simulink model "solar_pv_protected_c07_circuit"  (R2026b)
(part 7 of 16)

      | 用語2　　　　　　　 ; ADC：Analog-to-Digital Converter（アナログ・デジタル変換器）。測定電圧をデジタル値へ変換する回路。電流や温度も、センサーで電圧へ変換した後に読み取る。
      | 用語3　　　　　　　 ; IC：Integrated Circuit（集積回路）。複数の電子素子と機能を小さな半導体チップに集積した部品。
      | 用語4　　　　　　　 ; CH：Channel（測定チャネル）。CH0〜CH7はADCの入力番号であり、同時測定を意味しない。
      | 用語5　　　　　　　 ; MOSFET：Metal-Oxide-Semiconductor Field-Effect Transistor（金属・酸化膜・半導体構造の電界効果トランジスタ）。ゲートとソースの電圧でドレインとソースの導通を制御する素子。N-MOSはNチャネル型を表す。
      | 用語6　　　　　　　 ; FB：Feedback（帰還）。出力などを検出して内部制御へ戻すための信号・端子。
  ReadLabel_R31_P5 : ConnectionLabel  Description=|  Label=P5
      | この回路での名前　　; P5
      | 種別　　　　　　　　; ConnectionLabel
      | この回路での役割　　; 5V電源モジュールU12の出力を、ゲートドライバ入力LEDの電流制限抵抗とRP2040電源用ダイオードD3へ分配する。
      | この場所の直接接続　; R31（P5からU8のLEDへ流す電流をR32とともに制限する／232 ohm 1% 0.125W）: 1
      | 直接接続の範囲　　　; このラベルから実際の線・分岐・明示的な境界端子だけを追った接続。同名ラベルによる離れた場所への接続はこの欄に含めない。
      | 同一ネットの主接続　; U12（12Vから5Vを作る電源モジュール／TSR 1-2450）: 3(+VOUT)
      |                     ; C48（5V出力局所バルク／22uF 25V X7R）: 1
      |                     ; R31（P5からU8のLEDへ流す電流をR32とともに制限する／232 ohm 1% 0.125W）: 1
      |                     ; R38（P5からU9のLEDへ流す電流をR39とともに制限する／232 ohm 1% 0.125W）: 1
      |                     ; D3（DIODE／40V 1A Schottky VSYS OR）: 2(A)
      | 同一ネット全端子　　; C48: 1
      |                     ; D3: 2(A)
      |                     ; R31: 1
      |                     ; R38: 1
      |                     ; U12: 3(+VOUT)
      | 接続部品数　　　　　; 5部品（部品番号で集計。同一ネット全体）
      | 接続端子数　　　　　; 5端子（423端子の部品対応表で集計。ラベル・境界ポートの重複は含めない）
      | この場所の端子数　　; 1端子／1部品（同名ラベルによる接続を除く）
      | 同階層同名ラベル数　; 3個（このラベル自身を含む）
      | 全階層の接続ラベル　; 3個（実際に同じノードへつながるラベル。名前が違う別名も含む）
      | 接続ルール　　　　　; 同じ階層の同じラベル名を仮想配線として結ぶ。別のSubsystem内とは名前だけでつながらず、明示的なConnection Portと配線をたどる。色は用途の表示であり接続を決めない。
      | 確認の範囲　　　　　; 現在の保存回路の端子・配線から求めた静的接続。抵抗やICの内部を導線として短絡せずに集計した。説明の更新は動作シミュレーション、タイミング、実部品の性能・実機動作を保証するものではない。
      | 記録の基準　　　　　; measurement_label_layout_20261022_r01/after_layout_graph.json。部品対応表は端子名の対応付けにのみ使用。
      | 
      | 【この説明欄の略語・記号】
      | 用語1　　　　　　　 ; X7R：セラミックコンデンサの温度特性記号。英語の頭文字ではなく分類コード。X＝下限−55 ℃、7＝上限+125 ℃、R＝その範囲の容量変化±15%。直流バイアスによる容量変化は別に確認する。
      | 用語2　　　　　　　 ; IC：Integrated Circuit（集積回路）。複数の電子素子と機能を小さな半導体チップに集積した部品。
      | 用語3　　　　　　　 ; LED：Light-Emitting Diode（発光ダイオード）。本回路のゲートドライバ入力では光によって信号を伝え、入力側と出力側を絶縁するために用いる。
      | 用語4　　　　　　　 ; VIN/VOUT：入力電圧・出力電圧を表す端子／ネット名。INは入力、OUTは出力。電源変換器の電力端子なのか、検出用端子なのかは対象部品によって異なるため、端子と接続の説明に従う。
  ReadLabel_R38_P5 : ConnectionLabel  Description=|  Label=P5
      | この回路での名前　　; P5
      | 種別　　　　　　　　; ConnectionLabel
      | この回路での役割　　; 5V電源モジュールU12の出力を、ゲートドライバ入力LEDの電流制限抵抗とRP2040電源用ダイオードD3へ分配する。
      | この場所の直接接続　; R38（P5からU9のLEDへ流す電流をR39とともに制限する／232 ohm 1% 0.125W）: 1
      | 直接接続の範囲　　　; このラベルから実際の線・分岐・明示的な境界端子だけを追った接続。同名ラベルによる離れた場所への接続はこの欄に含めない。
      | 同一ネットの主接続　; U12（12Vから5Vを作る電源モジュール／TSR 1-2450）: 3(+VOUT)
      |                     ; C48（5V出力局所バルク／22uF 25V X7R）: 1
      |                     ; R31（P5からU8のLEDへ流す電流をR32とともに制限する／232 ohm 1% 0.125W）: 1
      |                     ; R38（P5からU9のLEDへ流す電流をR39とともに制限する／232 ohm 1% 0.125W）: 1
      |                     ; D3（DIODE／40V 1A Schottky VSYS OR）: 2(A)
      | 同一ネット全端子　　; C48: 1
      |                     ; D3: 2(A)
      |                     ; R31: 1
      |                     ; R38: 1
      |                     ; U12: 3(+VOUT)
      | 接続部品数　　　　　; 5部品（部品番号で集計。同一ネット全体）
      | 接続端子数　　　　　; 5端子（423端子の部品対応表で集計。ラベル・境界ポートの重複は含めない）
      | この場所の端子数　　; 1端子／1部品（同名ラベルによる接続を除く）
      | 同階層同名ラベル数　; 3個（このラベル自身を含む）
      | 全階層の接続ラベル　; 3個（実際に同じノードへつながるラベル。名前が違う別名も含む）
      | 接続ルール　　　　　; 同じ階層の同じラベル名を仮想配線として結ぶ。別のSubsystem内とは名前だけでつながらず、明示的なConnection Portと配線をたどる。色は用途の表示であり接続を決めない。
      | 確認の範囲　　　　　; 現在の保存回路の端子・配線から求めた静的接続。抵抗やICの内部を導線として短絡せずに集計した。説明の更新は動作シミュレーション、タイミング、実部品の性能・実機動作を保証するものではない。
      | 記録の基準　　　　　; measurement_label_layout_20261022_r01/after_layout_graph.json。部品対応表は端子名の対応付けにのみ使用。
      | 
      | 【この説明欄の略語・記号】
      | 用語1　　　　　　　 ; X7R：セラミックコンデンサの温度特性記号。英語の頭文字ではなく分類コード。X＝下限−55 ℃、7＝上限+125 ℃、R＝その範囲の容量変化±15%。直流バイアスによる容量変化は別に確認する。
      | 用語2　　　　　　　 ; IC：Integrated Circuit（集積回路）。複数の電子素子と機能を小さな半導体チップに集積した部品。
      | 用語3　　　　　　　 ; LED：Light-Emitting Diode（発光ダイオード）。本回路のゲートドライバ入力では光によって信号を伝え、入力側と出力側を絶縁するために用いる。
      | 用語4　　　　　　　 ; VIN/VOUT：入力電圧・出力電圧を表す端子／ネット名。INは入力、OUTは出力。電源変換器の電力端子なのか、検出用端子なのかは対象部品によって異なるため、端子と接続の説明に従う。
  ReadLabel_R45_H12 : ConnectionLabel  Description=|  Label=H12
      | この回路での名前　　; H12
      | 種別　　　　　　　　; ConnectionLabel
      | この回路での役割　　; 絶縁電源U10の二次側出力を、高側ゲートドライバU8と二次側コンデンサへ供給する。電圧の基準はSWであり、共通GND基準の12V電源P12とは別。
      | この場所の直接接続　; R45（H12からH_FBへ接続し、R46とともにU10の出力電圧帰還を構成する／38.3k 1%）: 1
      |                     ; R47（H_RLIMとH12を0 Ωで接続し、U10のRLIM端子の既存設定を実装する／0 ohm）: 2
      | 直接接続の範囲　　　; このラベルから実際の線・分岐・明示的な境界端子だけを追った接続。同名ラベルによる離れた場所への接続はこの欄に含めない。
      | 同一ネットの主接続　; U10（高側ゲート用の浮動電源を作る絶縁DC/DC／UCC14131QDWNRQ1）: 28(VDD), 29(VDD)
      |                     ; U8（高側の光ゲートドライバ／ACPL-P346-560E）: 6(VCC)
      |                     ; C32（光ゲートドライバ局所バイパス／1uF 50V X7R）: 1
      |                     ; C37（絶縁DC/DC二次側バルク／22uF 25V X7R）: 1
      |                     ; C38（絶縁DC/DC二次側HFバイパス／100nF 50V X7R）: 1
      |                     ; R45（H12からH_FBへ接続し、R46とともにU10の出力電圧帰還を構成する／38.3k 1%）: 1
      |                     ; R47（H_RLIMとH12を0 Ωで接続し、U10のRLIM端子の既存設定を実装する／0 ohm）: 2
      | 同一ネット全端子　　; C32: 1
      |                     ; C37: 1
      |                     ; C38: 1
      |                     ; R45: 1
      |                     ; R47: 2
      |                     ; U8: 6(VCC)
      |                     ; U10: 28(VDD), 29(VDD)
      | 接続部品数　　　　　; 7部品（部品番号で集計。同一ネット全体）
      | 接続端子数　　　　　; 8端子（423端子の部品対応表で集計。ラベル・境界ポートの重複は含めない）
      | この場所の端子数　　; 2端子／2部品（同名ラベルによる接続を除く）
      | 同階層同名ラベル数　; 3個（このラベル自身を含む）
      | 全階層の接続ラベル　; 3個（実際に同じノードへつながるラベル。名前が違う別名も含む）
      | 接続ルール　　　　　; 同じ階層の同じラベル名を仮想配線として結ぶ。別のSubsystem内とは名前だけでつながらず、明示的なConnection Portと配線をたどる。色は用途の表示であり接続を決めない。
      | 確認の範囲　　　　　; 現在の保存回路の端子・配線から求めた静的接続。抵抗やICの内部を導線として短絡せずに集計した。説明の更新は動作シミュレーション、タイミング、実部品の性能・実機動作を保証するものではない。
      | 記録の基準　　　　　; measurement_label_layout_20261022_r01/after_layout_graph.json。部品対応表は端子名の対応付けにのみ使用。
      | 
      | 【この説明欄の略語・記号】
      | 用語1　　　　　　　 ; DC：Direct Current（直流）。ここでは直流電源または直流成分。DCバイアスはコンデンサに重なる直流電圧を指す。
      | 用語2　　　　　　　 ; DC/DC：DC-to-DC Converter（直流電圧変換器）。直流入力を別の直流電圧へ変換する電源回路。絶縁の有無は個々の部品説明で確認する。
      | 用語3　　　　　　　 ; HF：High Frequency（高周波）。速い電圧・電流変化に対応する成分。具体的な周波数帯は対象回路ごとに説明する。
      | 用語4　　　　　　　 ; X7R：セラミックコンデンサの温度特性記号。英語の頭文字ではなく分類コード。X＝下限−55 ℃、7＝上限+125 ℃、R＝その範囲の容量変化±15%。直流バイアスによる容量変化は別に確認する。
      | 用語5　　　　　　　 ; IC：Integrated Circuit（集積回路）。複数の電子素子と機能を小さな半導体チップに集積した部品。
      | 用語6　　　　　　　 ; MOSFET：Metal-Oxide-Semiconductor Field-Effect Transistor（金属・酸化膜・半導体構造の電界効果トランジスタ）。ゲートとソースの電圧でドレインとソースの導通を制御する素子。N-MOSはNチャネル型を表す。
      | 用語7　　　　　　　 ; GND：Ground（回路の基準電位・電流帰路）。この図の共通基準。保護接地や大地への接続を意味するとは限らない。
      | 用語8　　　　　　　 ; FB：Feedback（帰還）。出力などを検出して内部制御へ戻すための信号・端子。
      | 用語9　　　　　　　 ; VCC/VDD/VEE/VS：ICの電源端子名。文字の歴史的な由来を現在の接続機能へ当てはめない。現回路のVEEはU8/U10では浮動基準SW、U9ではGND。各電圧・基準は端子と接続を参照する。
      | 用語10　　　　　　　; RLIM：U10の外付け抵抗による制限設定端子。外付けR47で二次側の電圧調整に使う電流を制限する端子。主電力段の充電電流制限とは別の機能。
      | 用語11　　　　　　　; SW：Switching Node（スイッチング点）。主電力段の上下MOSFETとL1がつながる、電圧が高速に切り替わる点。GNDとは別電位。
  ReadLabel_R45_H_FB : ConnectionLabel  Description=|  Label=H_FB
      | この回路での名前　　; H_FB
      | 種別　　　　　　　　; ConnectionLabel
      | この回路での役割　　; 絶縁電源U10の二次側出力を監視する分圧抵抗R45/R46と、U10のFBVEE/FBVDD入力、フィルタC39を結ぶアナログ帰還信号。基準はSW。電力を供給する出力線ではない。
      | この場所の直接接続　; R45（H12からH_FBへ接続し、R46とともにU10の出力電圧帰還を構成する／38.3k 1%）: 2
      | 直接接続の範囲　　　; このラベルから実際の線・分岐・明示的な境界端子だけを追った接続。同名ラベルによる離れた場所への接続はこの欄に含めない。
      | 同一ネットの主接続　; U10（高側ゲート用の浮動電源を作る絶縁DC/DC／UCC14131QDWNRQ1）: 33(FBVEE), 34(FBVDD)
      |                     ; R45（H12からH_FBへ接続し、R46とともにU10の出力電圧帰還を構成する／38.3k 1%）: 2
      |                     ; R46（H_FBからSWへ接続し、R45とともにU10の出力電圧帰還を構成する／10k 1%）: 1
      |                     ; C39（浮動出力フィードバックフィルタ／330pF 50V C0G 5%）: 1
      | 同一ネット全端子　　; C39: 1
      |                     ; R45: 2
      |                     ; R46: 1
      |                     ; U10: 33(FBVEE), 34(FBVDD)
      | 接続部品数　　　　　; 4部品（部品番号で集計。同一ネット全体）
      | 接続端子数　　　　　; 5端子（423端子の部品対応表で集計。ラベル・境界ポートの重複は含めない）
      | この場所の端子数　　; 1端子／1部品（同名ラベルによる接続を除く）
      | 同階層同名ラベル数　; 3個（このラベル自身を含む）
      | 全階層の接続ラベル　; 3個（実際に同じノードへつながるラベル。名前が違う別名も含む）
      | 接続ルール　　　　　; 同じ階層の同じラベル名を仮想配線として結ぶ。別のSubsystem内とは名前だけでつながらず、明示的なConnection Portと配線をたどる。色は用途の表示であり接続を決めない。
      | 確認の範囲　　　　　; 現在の保存回路の端子・配線から求めた静的接続。抵抗やICの内部を導線として短絡せずに集計した。説明の更新は動作シミュレーション、タイミング、実部品の性能・実機動作を保証するものではない。
      | 記録の基準　　　　　; measurement_label_layout_20261022_r01/after_layout_graph.json。部品対応表は端子名の対応付けにのみ使用。
      | 
      | 【この説明欄の略語・記号】
      | 用語1　　　　　　　 ; DC：Direct Current（直流）。ここでは直流電源または直流成分。DCバイアスはコンデンサに重なる直流電圧を指す。
      | 用語2　　　　　　　 ; DC/DC：DC-to-DC Converter（直流電圧変換器）。直流入力を別の直流電圧へ変換する電源回路。絶縁の有無は個々の部品説明で確認する。
      | 用語3　　　　　　　 ; C0G：温度補償系セラミックコンデンサの温度特性記号。英語の頭文字ではなく分類コード。−55〜+125 ℃で容量の温度係数が0±30 ppm/℃の特性を表す。ppmはparts per million（100万分の1）で、30 ppm/℃は1 ℃当たり0.003%に相当する。
      | 用語4　　　　　　　 ; IC：Integrated Circuit（集積回路）。複数の電子素子と機能を小さな半導体チップに集積した部品。
      | 用語5　　　　　　　 ; MOSFET：Metal-Oxide-Semiconductor Field-Effect Transistor（金属・酸化膜・半導体構造の電界効果トランジスタ）。ゲートとソースの電圧でドレインとソースの導通を制御する素子。N-MOSはNチャネル型を表す。
      | 用語6　　　　　　　 ; GND：Ground（回路の基準電位・電流帰路）。この図の共通基準。保護接地や大地への接続を意味するとは限らない。
      | 用語7　　　　　　　 ; FB：Feedback（帰還）。出力などを検出して内部制御へ戻すための信号・端子。
      | 用語8　　　　　　　 ; FBVDD/FBVEE：U10の出力電圧帰還端子。二次側の出力電圧設定に用いる。現接続では両端子がH_FBへ接続される。
      | 用語9　　　　　　　 ; SW：Switching Node（スイッチング点）。主電力段の上下MOSFETとL1がつながる、電圧が高速に切り替わる点。GNDとは別電位。
  ReadLabel_R46_H_FB : ConnectionLabel  Description=|  Label=H_FB
      | この回路での名前　　; H_FB
      | 種別　　　　　　　　; ConnectionLabel
      | この回路での役割　　; 絶縁電源U10の二次側出力を監視する分圧抵抗R45/R46と、U10のFBVEE/FBVDD入力、フィルタC39を結ぶアナログ帰還信号。基準はSW。電力を供給する出力線ではない。
      | この場所の直接接続　; R46（H_FBからSWへ接続し、R45とともにU10の出力電圧帰還を構成する／10k 1%）: 1
      | 直接接続の範囲　　　; このラベルから実際の線・分岐・明示的な境界端子だけを追った接続。同名ラベルによる離れた場所への接続はこの欄に含めない。
      | 同一ネットの主接続　; U10（高側ゲート用の浮動電源を作る絶縁DC/DC／UCC14131QDWNRQ1）: 33(FBVEE), 34(FBVDD)
      |                     ; R45（H12からH_FBへ接続し、R46とともにU10の出力電圧帰還を構成する／38.3k 1%）: 2
      |                     ; R46（H_FBからSWへ接続し、R45とともにU10の出力電圧帰還を構成する／10k 1%）: 1
      |                     ; C39（浮動出力フィードバックフィルタ／330pF 50V C0G 5%）: 1
      | 同一ネット全端子　　; C39: 1
      |                     ; R45: 2
      |                     ; R46: 1
      |                     ; U10: 33(FBVEE), 34(FBVDD)
      | 接続部品数　　　　　; 4部品（部品番号で集計。同一ネット全体）
      | 接続端子数　　　　　; 5端子（423端子の部品対応表で集計。ラベル・境界ポートの重複は含めない）
      | この場所の端子数　　; 1端子／1部品（同名ラベルによる接続を除く）
      | 同階層同名ラベル数　; 3個（このラベル自身を含む）
      | 全階層の接続ラベル　; 3個（実際に同じノードへつながるラベル。名前が違う別名も含む）
      | 接続ルール　　　　　; 同じ階層の同じラベル名を仮想配線として結ぶ。別のSubsystem内とは名前だけでつながらず、明示的なConnection Portと配線をたどる。色は用途の表示であり接続を決めない。
      | 確認の範囲　　　　　; 現在の保存回路の端子・配線から求めた静的接続。抵抗やICの内部を導線として短絡せずに集計した。説明の更新は動作シミュレーション、タイミング、実部品の性能・実機動作を保証するものではない。
      | 記録の基準　　　　　; measurement_label_layout_20261022_r01/after_layout_graph.json。部品対応表は端子名の対応付けにのみ使用。
      | 
      | 【この説明欄の略語・記号】
      | 用語1　　　　　　　 ; DC：Direct Current（直流）。ここでは直流電源または直流成分。DCバイアスはコンデンサに重なる直流電圧を指す。
      | 用語2　　　　　　　 ; DC/DC：DC-to-DC Converter（直流電圧変換器）。直流入力を別の直流電圧へ変換する電源回路。絶縁の有無は個々の部品説明で確認する。
      | 用語3　　　　　　　 ; C0G：温度補償系セラミックコンデンサの温度特性記号。英語の頭文字ではなく分類コード。−55〜+125 ℃で容量の温度係数が0±30 ppm/℃の特性を表す。ppmはparts per million（100万分の1）で、30 ppm/℃は1 ℃当たり0.003%に相当する。
      | 用語4　　　　　　　 ; IC：Integrated Circuit（集積回路）。複数の電子素子と機能を小さな半導体チップに集積した部品。
      | 用語5　　　　　　　 ; MOSFET：Metal-Oxide-Semiconductor Field-Effect Transistor（金属・酸化膜・半導体構造の電界効果トランジスタ）。ゲートとソースの電圧でドレインとソースの導通を制御する素子。N-MOSはNチャネル型を表す。
      | 用語6　　　　　　　 ; GND：Ground（回路の基準電位・電流帰路）。この図の共通基準。保護接地や大地への接続を意味するとは限らない。
      | 用語7　　　　　　　 ; FB：Feedback（帰還）。出力などを検出して内部制御へ戻すための信号・端子。
      | 用語8　　　　　　　 ; FBVDD/FBVEE：U10の出力電圧帰還端子。二次側の出力電圧設定に用いる。現接続では両端子がH_FBへ接続される。
      | 用語9　　　　　　　 ; SW：Switching Node（スイッチング点）。主電力段の上下MOSFETとL1がつながる、電圧が高速に切り替わる点。GNDとは別電位。
  ReadLabel_R49_V3V3 : ConnectionLabel  Description=|  Label=V3V3
      | この回路での名前　　; V3V3
      | 種別　　　　　　　　; ConnectionLabel
      | この回路での役割　　; RP2040基板U7の3.3V出力から、ADC・電流検出IC・温度センサー・基準電圧ICなどへ電源を分配する。信号のプルアップ抵抗にも供給する。
      | この場所の直接接続　; R49（U10のオープンドレインPG信号BIAS_PGをPicoの3V3へ引き上げ、GP9で読める電圧にする／10k 1%）: 2
      | 直接接続の範囲　　　; このラベルから実際の線・分岐・明示的な境界端子だけを追った接続。同名ラベルによる離れた場所への接続はこの欄に含めない。
      | 同一ネットの主接続　; U7（RP2040搭載Pico W／SC0918）: 36(3V3_OUT)
      |                     ; U1（外付けADC／MCP3208-CI/SL）: 16(VDD)
      |                     ; U2（PV入力電流の検出アンプ／INA241A3IDDFR）: 6(VS)
      |                     ; U3（L1直後の出力電流の検出アンプ／INA241A3IDDFR）: 6(VS)
      |                     ; U4（電池温度センサー／TMP235A2DBZR）: 1(VDD)
      |                     ; U5（放熱器温度センサー／TMP235A2DBZR）: 1(VDD)
      |                     ; U6（2.5Vの測定基準電圧源／REF3025EAIDBZR）: 1(IN)
      |                     ; R49（U10のオープンドレインPG信号BIAS_PGをPicoの3V3へ引き上げ、GP9で読める電圧にする／10k 1%）: 2
      |                     ; P_RFLT_PU（LTC4364のオープンドレインFLTをMCUの3.3 V系へ引き上げる／22 kΩ）: 1
      | 同一ネット全端子　　; C17: 1
      |                     ; C18: 1
      |                     ; C22: 1
      |                     ; C24: 1
      |                     ; C26: 1
      |                     ; C28: 1
      |                     ; C30: 1
      |                     ; P_RFLT_PU: 1
      |                     ; R15: 1
      |                     ; R49: 2
      |                     ; U1: 16(VDD)
      |                     ; U2: 6(VS)
      |                     ; U3: 6(VS)
      |                     ; U4: 1(VDD)
      |                     ; U5: 1(VDD)
      |                     ; U6: 1(IN)
      |                     ; U7: 36(3V3_OUT)
      | 接続部品数　　　　　; 17部品（部品番号で集計。同一ネット全体）
      | 接続端子数　　　　　; 17端子（423端子の部品対応表で集計。ラベル・境界ポートの重複は含めない）
      | この場所の端子数　　; 1端子／1部品（同名ラベルによる接続を除く）
      | 同階層同名ラベル数　; 10個（このラベル自身を含む）
      | 全階層の接続ラベル　; 10個（実際に同じノードへつながるラベル。名前が違う別名も含む）
      | 接続ルール　　　　　; 同じ階層の同じラベル名を仮想配線として結ぶ。別のSubsystem内とは名前だけでつながらず、明示的なConnection Portと配線をたどる。色は用途の表示であり接続を決めない。
      | 確認の範囲　　　　　; 現在の保存回路の端子・配線から求めた静的接続。抵抗やICの内部を導線として短絡せずに集計した。説明の更新は動作シミュレーション、タイミング、実部品の性能・実機動作を保証するものではない。
      | 記録の基準　　　　　; measurement_label_layout_20261022_r01/after_layout_graph.json。部品対応表は端子名の対応付けにのみ使用。
      | 
      | 【この説明欄の略語・記号】
      | 用語1　　　　　　　 ; ADC：Analog-to-Digital Converter（アナログ・デジタル変換器）。測定電圧をデジタル値へ変換する回路。電流や温度も、センサーで電圧へ変換した後に読み取る。
      | 用語2　　　　　　　 ; IC：Integrated Circuit（集積回路）。複数の電子素子と機能を小さな半導体チップに集積した部品。
      | 用語3　　　　　　　 ; MCU：Microcontroller Unit（マイクロコントローラ）。プログラムを実行し、測定値の処理や出力制御を担当する小型計算機。
      | 用語4　　　　　　　 ; GPIO：General-Purpose Input/Output（汎用入出力端子）。入力・出力や周辺機能に割り当てられる端子。GPの後の数字はRP2040の端子信号番号で、基板上の物理ピン番号とは別。
      | 用語5　　　　　　　 ; MOSFET：Metal-Oxide-Semiconductor Field-Effect Transistor（金属・酸化膜・半導体構造の電界効果トランジスタ）。ゲートとソースの電圧でドレインとソースの導通を制御する素子。N-MOSはNチャネル型を表す。
      | 用語6　　　　　　　 ; PV：Photovoltaic（太陽光発電）。光を電気へ変える発電方式。PVを含むネット名は太陽電池側の測定・電力経路を表す。
      | 用語7　　　　　　　 ; GND：Ground（回路の基準電位・電流帰路）。この図の共通基準。保護接地や大地への接続を意味するとは限らない。
      | 用語8　　　　　　　 ; PG：Power Good（電源状態通知）。電源出力が規定状態にあるかを知らせる信号。プルアップ条件と実際の通知条件は対象ICの説明で確認する。
      | 用語9　　　　　　　 ; FLT：Fault（故障状態通知）。LTC4364の故障警告出力。全種類の異常や逆流を一律に通知する信号という意味ではない。
      | 用語10　　　　　　　; VCC/VDD/VEE/VS：ICの電源端子名。文字の歴史的な由来を現在の接続機能へ当てはめない。現回路のVEEはU8/U10では浮動基準SW、U9ではGND。各電圧・基準は端子と接続を参照する。
      | 用語11　　　　　　　; SW：Switching Node（スイッチング点）。主電力段の上下MOSFETとL1がつながる、電圧が高速に切り替わる点。GNDとは別電位。
  ReadLabel_U10_BIAS_EN : ConnectionLabel  Description=|  Label=BIAS_EN
      | この回路での名前　　; BIAS_EN
      | 種別　　　　　　　　; ConnectionLabel
      | この回路での役割　　; RP2040基板U7のGP8と、絶縁電源U10のENA入力を結ぶ有効化指令線。R48はこの指令線のプルダウン。電源出力そのものではない。
      | この場所の直接接続　; U10（絶縁ゲート用補助電源）: 4(ENA)
      | 直接接続の範囲　　　; このラベルから実際の線・分岐・明示的な境界端子だけを追った接続。同名ラベルによる離れた場所への接続はこの欄に含めない。
      | 同一ネットの主接続　; U7（RP2040搭載Pico W／SC0918）: 11(GP8)
      |                     ; U10（高側ゲート用の浮動電源を作る絶縁DC/DC／UCC14131QDWNRQ1）: 4(ENA)
      |                     ; R48（BIAS_ENをGNDへ引き下げ、RP2040未駆動時のU10停止側の状態を作る／10k 1%）: 1
      | 同一ネット全端子　　; R48: 1
      |                     ; U7: 11(GP8)
      |                     ; U10: 4(ENA)
      | 接続部品数　　　　　; 3部品（部品番号で集計。同一ネット全体）
      | 接続端子数　　　　　; 3端子（423端子の部品対応表で集計。ラベル・境界ポートの重複は含めない）
      | この場所の端子数　　; 1端子／1部品（同名ラベルによる接続を除く）
      | 同階層同名ラベル数　; 2個（このラベル自身を含む）
      | 全階層の接続ラベル　; 2個（実際に同じノードへつながるラベル）
      | 接続ルール　　　　　; 同じ階層の同じラベル名を仮想配線として結ぶ。別のSubsystem内とは名前だけでつながらず、明示的なConnection Portと配線をたどる。色は用途の表示であり接続を決めない。
      | 確認の範囲　　　　　; 現在の保存回路の端子・配線から求めた静的接続。抵抗やICの内部を導線として短絡せずに集計した。説明の更新は動作シミュレーション、タイミング、実部品の性能・実機動作を保証するものではない。
      | 記録の基準　　　　　; bias_resistor_layout_20261022_r01/final_layout_graph.json。実際の配線・端子・同階層ラベルから確認。
      | 
      | 【この説明欄の略語・記号】
      | 用語1　　　　　　　 ; DC：Direct Current（直流）。ここでは直流電源または直流成分。DCバイアスはコンデンサに重なる直流電圧を指す。
      | 用語2　　　　　　　 ; DC/DC：DC-to-DC Converter（直流電圧変換器）。直流入力を別の直流電圧へ変換する電源回路。絶縁の有無は個々の部品説明で確認する。
      | 用語3　　　　　　　 ; IC：Integrated Circuit（集積回路）。複数の電子素子と機能を小さな半導体チップに集積した部品。
      | 用語4　　　　　　　 ; GPIO：General-Purpose Input/Output（汎用入出力端子）。入力・出力や周辺機能に割り当てられる端子。GPの後の数字はRP2040の端子信号番号で、基板上の物理ピン番号とは別。
      | 用語5　　　　　　　 ; GND：Ground（回路の基準電位・電流帰路）。この図の共通基準。保護接地や大地への接続を意味するとは限らない。
      | 用語6　　　　　　　 ; EN：Enable（動作許可）。対象機能の動作を許可する信号。端子ごとの有効レベルや接続状態に従う。
      | 
      | 【信号と抵抗の役割】
      | 名前の意味　　　　　; BIASは英単語Bias（バイアス）で、この図ではゲート駆動用の補助電源を指す。EN = Enable（動作許可）、PG = Power Good（電源状態通知）。ラベルは部品ではなく、同じ階層の同名ノードとの接続を示す。
      | 動作と論理状態　　　; U7のGP8とU10のENA（4番）は同じノード。Highで絶縁電源の動作を許可し、Lowで停止を指示する。R48はそのノードからGNDへの10 kΩプルダウンで、マイコン端子が駆動されない間のLow側の状態を作る。
      | メーカー根拠　　　　; https://www.ti.com/lit/gpn/ucc14131-q1（UCC14131-Q1データシート、端子表と11.3.3）
  ReadLabel_U10_BIAS_PG : ConnectionLabel  Description=|  Label=BIAS_PG
      | この回路での名前　　; BIAS_PG
      | 種別　　　　　　　　; ConnectionLabel
      | この回路での役割　　; 絶縁電源U10のPG出力から、RP2040基板U7のGP9へ電源の状態を返す。R49を介して3.3Vへプルアップされる。停止指令とは別の状態信号。
      | この場所の直接接続　; U10（絶縁ゲート用補助電源）: 3(PG)
      | 直接接続の範囲　　　; このラベルから実際の線・分岐・明示的な境界端子だけを追った接続。同名ラベルによる離れた場所への接続はこの欄に含めない。
      | 同一ネットの主接続　; U10（高側ゲート用の浮動電源を作る絶縁DC/DC／UCC14131QDWNRQ1）: 3(PG)
      |                     ; U7（RP2040搭載Pico W／SC0918）: 12(GP9)
      |                     ; R49（U10のオープンドレインPG信号BIAS_PGをPicoの3V3へ引き上げ、GP9で読める電圧にする／10k 1%）: 1
      | 同一ネット全端子　　; R49: 1
      |                     ; U7: 12(GP9)
      |                     ; U10: 3(PG)
      | 接続部品数　　　　　; 3部品（部品番号で集計。同一ネット全体）
      | 接続端子数　　　　　; 3端子（423端子の部品対応表で集計。ラベル・境界ポートの重複は含めない）
      | この場所の端子数　　; 1端子／1部品（同名ラベルによる接続を除く）
      | 同階層同名ラベル数　; 2個（このラベル自身を含む）
      | 全階層の接続ラベル　; 2個（実際に同じノードへつながるラベル）
      | 接続ルール　　　　　; 同じ階層の同じラベル名を仮想配線として結ぶ。別のSubsystem内とは名前だけでつながらず、明示的なConnection Portと配線をたどる。色は用途の表示であり接続を決めない。
      | 確認の範囲　　　　　; 現在の保存回路の端子・配線から求めた静的接続。抵抗やICの内部を導線として短絡せずに集計した。説明の更新は動作シミュレーション、タイミング、実部品の性能・実機動作を保証するものではない。
      | 記録の基準　　　　　; bias_resistor_layout_20261022_r01/final_layout_graph.json。実際の配線・端子・同階層ラベルから確認。
      | 
      | 【この説明欄の略語・記号】
      | 用語1　　　　　　　 ; DC：Direct Current（直流）。ここでは直流電源または直流成分。DCバイアスはコンデンサに重なる直流電圧を指す。
      | 用語2　　　　　　　 ; DC/DC：DC-to-DC Converter（直流電圧変換器）。直流入力を別の直流電圧へ変換する電源回路。絶縁の有無は個々の部品説明で確認する。
      | 用語3　　　　　　　 ; IC：Integrated Circuit（集積回路）。複数の電子素子と機能を小さな半導体チップに集積した部品。
      | 用語4　　　　　　　 ; GPIO：General-Purpose Input/Output（汎用入出力端子）。入力・出力や周辺機能に割り当てられる端子。GPの後の数字はRP2040の端子信号番号で、基板上の物理ピン番号とは別。
      | 用語5　　　　　　　 ; PG：Power Good（電源状態通知）。電源出力が規定状態にあるかを知らせる信号。プルアップ条件と実際の通知条件は対象ICの説明で確認する。
      | 
      | 【信号と抵抗の役割】
      | 名前の意味　　　　　; BIASは英単語Bias（バイアス）で、この図ではゲート駆動用の補助電源を指す。EN = Enable（動作許可）、PG = Power Good（電源状態通知）。ラベルは部品ではなく、同じ階層の同名ノードとの接続を示す。
      | 動作と論理状態　　　; U10のPG（3番）からU7のGP9へ状態を返す。U10の正常成立時は内部出力がLowへ引き込み、正常不成立・停止時は出力を解放する。R49は解放時のノードを3.3 Vへ引き上げる10 kΩプルアップ。GP9は入力として読む。Highが正常という意味ではない。
      | メーカー根拠　　　　; https://www.ti.com/lit/gpn/ucc14131-q1（UCC14131-Q1データシート、端子表と11.3.3）
  ReadLabel_U10_H12 : ConnectionLabel  Description=|  Label=H12
      | この回路での名前　　; H12
      | 種別　　　　　　　　; ConnectionLabel
      | この回路での役割　　; 絶縁電源U10の二次側出力を、高側ゲートドライバU8と二次側コンデンサへ供給する。電圧の基準はSWであり、共通GND基準の12V電源P12とは別。
      | この場所の直接接続　; C37（絶縁DC/DC二次側バルク／22uF 25V X7R）: 1
      |                     ; C38（絶縁DC/DC二次側HFバイパス／100nF 50V X7R）: 1
      |                     ; U10（高側ゲート用の浮動電源を作る絶縁DC/DC／UCC14131QDWNRQ1）: 28(VDD), 29(VDD)
      | 直接接続の範囲　　　; このラベルから実際の線・分岐・明示的な境界端子だけを追った接続。同名ラベルによる離れた場所への接続はこの欄に含めない。
      | 同一ネットの主接続　; U10（高側ゲート用の浮動電源を作る絶縁DC/DC／UCC14131QDWNRQ1）: 28(VDD), 29(VDD)
      |                     ; U8（高側の光ゲートドライバ／ACPL-P346-560E）: 6(VCC)
      |                     ; C32（光ゲートドライバ局所バイパス／1uF 50V X7R）: 1
      |                     ; C37（絶縁DC/DC二次側バルク／22uF 25V X7R）: 1
      |                     ; C38（絶縁DC/DC二次側HFバイパス／100nF 50V X7R）: 1
      |                     ; R45（H12からH_FBへ接続し、R46とともにU10の出力電圧帰還を構成する／38.3k 1%）: 1
      |                     ; R47（H_RLIMとH12を0 Ωで接続し、U10のRLIM端子の既存設定を実装する／0 ohm）: 2
      | 同一ネット全端子　　; C32: 1
      |                     ; C37: 1
      |                     ; C38: 1
      |                     ; R45: 1
      |                     ; R47: 2
      |                     ; U8: 6(VCC)
      |                     ; U10: 28(VDD), 29(VDD)
      | 接続部品数　　　　　; 7部品（部品番号で集計。同一ネット全体）
      | 接続端子数　　　　　; 8端子（423端子の部品対応表で集計。ラベル・境界ポートの重複は含めない）
      | この場所の端子数　　; 4端子／3部品（同名ラベルによる接続を除く）
      | 同階層同名ラベル数　; 3個（このラベル自身を含む）
      | 全階層の接続ラベル　; 3個（実際に同じノードへつながるラベル。名前が違う別名も含む）
      | 接続ルール　　　　　; 同じ階層の同じラベル名を仮想配線として結ぶ。別のSubsystem内とは名前だけでつながらず、明示的なConnection Portと配線をたどる。色は用途の表示であり接続を決めない。
      | 確認の範囲　　　　　; 現在の保存回路の端子・配線から求めた静的接続。抵抗やICの内部を導線として短絡せずに集計した。説明の更新は動作シミュレーション、タイミング、実部品の性能・実機動作を保証するものではない。
      | 記録の基準　　　　　; measurement_label_layout_20261022_r01/after_layout_graph.json。部品対応表は端子名の対応付けにのみ使用。
      | 
      | 【この説明欄の略語・記号】
      | 用語1　　　　　　　 ; DC：Direct Current（直流）。ここでは直流電源または直流成分。DCバイアスはコンデンサに重なる直流電圧を指す。
      | 用語2　　　　　　　 ; DC/DC：DC-to-DC Converter（直流電圧変換器）。直流入力を別の直流電圧へ変換する電源回路。絶縁の有無は個々の部品説明で確認する。
      | 用語3　　　　　　　 ; HF：High Frequency（高周波）。速い電圧・電流変化に対応する成分。具体的な周波数帯は対象回路ごとに説明する。
      | 用語4　　　　　　　 ; X7R：セラミックコンデンサの温度特性記号。英語の頭文字ではなく分類コード。X＝下限−55 ℃、7＝上限+125 ℃、R＝その範囲の容量変化±15%。直流バイアスによる容量変化は別に確認する。
      | 用語5　　　　　　　 ; IC：Integrated Circuit（集積回路）。複数の電子素子と機能を小さな半導体チップに集積した部品。
      | 用語6　　　　　　　 ; MOSFET：Metal-Oxide-Semiconductor Field-Effect Transistor（金属・酸化膜・半導体構造の電界効果トランジスタ）。ゲートとソースの電圧でドレインとソースの導通を制御する素子。N-MOSはNチャネル型を表す。
      | 用語7　　　　　　　 ; GND：Ground（回路の基準電位・電流帰路）。この図の共通基準。保護接地や大地への接続を意味するとは限らない。
      | 用語8　　　　　　　 ; FB：Feedback（帰還）。出力などを検出して内部制御へ戻すための信号・端子。
      | 用語9　　　　　　　 ; VCC/VDD/VEE/VS：ICの電源端子名。文字の歴史的な由来を現在の接続機能へ当てはめない。現回路のVEEはU8/U10では浮動基準SW、U9ではGND。各電圧・基準は端子と接続を参照する。
      | 用語10　　　　　　　; RLIM：U10の外付け抵抗による制限設定端子。外付けR47で二次側の電圧調整に使う電流を制限する端子。主電力段の充電電流制限とは別の機能。
      | 用語11　　　　　　　; SW：Switching Node（スイッチング点）。主電力段の上下MOSFETとL1がつながる、電圧が高速に切り替わる点。GNDとは別電位。
  ReadLabel_U10_H_FB1 : ConnectionLabel  Description=|  Label=H_FB
      | この回路での名前　　; H_FB
      | 種別　　　　　　　　; ConnectionLabel
      | この回路での役割　　; 絶縁電源U10の二次側出力を監視する分圧抵抗R45/R46と、U10のFBVEE/FBVDD入力、フィルタC39を結ぶアナログ帰還信号。基準はSW。電力を供給する出力線ではない。
      | この場所の直接接続　; C39（浮動出力フィードバックフィルタ／330pF 50V C0G 5%）: 1
      |                     ; U10（高側ゲート用の浮動電源を作る絶縁DC/DC／UCC14131QDWNRQ1）: 33(FBVEE), 34(FBVDD)
      | 直接接続の範囲　　　; このラベルから実際の線・分岐・明示的な境界端子だけを追った接続。同名ラベルによる離れた場所への接続はこの欄に含めない。
      | 同一ネットの主接続　; U10（高側ゲート用の浮動電源を作る絶縁DC/DC／UCC14131QDWNRQ1）: 33(FBVEE), 34(FBVDD)
      |                     ; R45（H12からH_FBへ接続し、R46とともにU10の出力電圧帰還を構成する／38.3k 1%）: 2
      |                     ; R46（H_FBからSWへ接続し、R45とともにU10の出力電圧帰還を構成する／10k 1%）: 1
      |                     ; C39（浮動出力フィードバックフィルタ／330pF 50V C0G 5%）: 1
      | 同一ネット全端子　　; C39: 1
      |                     ; R45: 2
      |                     ; R46: 1
      |                     ; U10: 33(FBVEE), 34(FBVDD)
      | 接続部品数　　　　　; 4部品（部品番号で集計。同一ネット全体）
      | 接続端子数　　　　　; 5端子（423端子の部品対応表で集計。ラベル・境界ポートの重複は含めない）
      | この場所の端子数　　; 3端子／2部品（同名ラベルによる接続を除く）
      | 同階層同名ラベル数　; 3個（このラベル自身を含む）
      | 全階層の接続ラベル　; 3個（実際に同じノードへつながるラベル。名前が違う別名も含む）
      | 接続ルール　　　　　; 同じ階層の同じラベル名を仮想配線として結ぶ。別のSubsystem内とは名前だけでつながらず、明示的なConnection Portと配線をたどる。色は用途の表示であり接続を決めない。
      | 確認の範囲　　　　　; 現在の保存回路の端子・配線から求めた静的接続。抵抗やICの内部を導線として短絡せずに集計した。説明の更新は動作シミュレーション、タイミング、実部品の性能・実機動作を保証するものではない。
      | 記録の基準　　　　　; measurement_label_layout_20261022_r01/after_layout_graph.json。部品対応表は端子名の対応付けにのみ使用。
      | 
      | 【この説明欄の略語・記号】
      | 用語1　　　　　　　 ; DC：Direct Current（直流）。ここでは直流電源または直流成分。DCバイアスはコンデンサに重なる直流電圧を指す。
      | 用語2　　　　　　　 ; DC/DC：DC-to-DC Converter（直流電圧変換器）。直流入力を別の直流電圧へ変換する電源回路。絶縁の有無は個々の部品説明で確認する。
      | 用語3　　　　　　　 ; C0G：温度補償系セラミックコンデンサの温度特性記号。英語の頭文字ではなく分類コード。−55〜+125 ℃で容量の温度係数が0±30 ppm/℃の特性を表す。ppmはparts per million（100万分の1）で、30 ppm/℃は1 ℃当たり0.003%に相当する。
      | 用語4　　　　　　　 ; IC：Integrated Circuit（集積回路）。複数の電子素子と機能を小さな半導体チップに集積した部品。
      | 用語5　　　　　　　 ; MOSFET：Metal-Oxide-Semiconductor Field-Effect Transistor（金属・酸化膜・半導体構造の電界効果トランジスタ）。ゲートとソースの電圧でドレインとソースの導通を制御する素子。N-MOSはNチャネル型を表す。
      | 用語6　　　　　　　 ; GND：Ground（回路の基準電位・電流帰路）。この図の共通基準。保護接地や大地への接続を意味するとは限らない。
      | 用語7　　　　　　　 ; FB：Feedback（帰還）。出力などを検出して内部制御へ戻すための信号・端子。
      | 用語8　　　　　　　 ; FBVDD/FBVEE：U10の出力電圧帰還端子。二次側の出力電圧設定に用いる。現接続では両端子がH_FBへ接続される。
      | 用語9　　　　　　　 ; SW：Switching Node（スイッチング点）。主電力段の上下MOSFETとL1がつながる、電圧が高速に切り替わる点。GNDとは別電位。
  ReadLabel_U10_P12 : ConnectionLabel  Description=|  Label=P12
      | この回路での名前　　; P12
      | 種別　　　　　　　　; ConnectionLabel
      | この回路での役割　　; 12V電源モジュールU11の出力を、低側ゲートドライバU9、絶縁電源U10の一次側、5V電源モジュールU12へ分配する。
      | この場所の直接接続　; C34（絶縁DC/DC入力バルク／22uF 25V X7R）: 1
      |                     ; C35（絶縁DC/DC入力バルク／22uF 25V X7R）: 1
      |                     ; C36（絶縁DC/DC一次側HFバイパス／100nF 50V X7R）: 1
      |                     ; U10（高側ゲート用の浮動電源を作る絶縁DC/DC／UCC14131QDWNRQ1）: 6(VIN), 7(VIN)
      | 直接接続の範囲　　　; このラベルから実際の線・分岐・明示的な境界端子だけを追った接続。同名ラベルによる離れた場所への接続はこの欄に含めない。
      | 同一ネットの主接続　; U11（バッテリー補助分岐から12Vを作る電源モジュール／TSR 1-48120WI）: 3(+VOUT)
      |                     ; U9（低側の光ゲートドライバ／ACPL-P346-560E）: 6(VCC)
      |                     ; U10（高側ゲート用の浮動電源を作る絶縁DC/DC／UCC14131QDWNRQ1）: 6(VIN), 7(VIN)
      |                     ; U12（12Vから5Vを作る電源モジュール／TSR 1-2450）: 1(+VIN)
      |                     ; C45（12Vレギュレータ出力局所バイパス／22uF 25V X7R）: 1
      |                     ; C46（共通12Vバルク/過渡蓄積／470uF 25V hybrid）: 1
      |                     ; C47（5Vレギュレータ入力局所バイパス／1uF 50V X7R）: 1
      | 同一ネット全端子　　; C33: 1
      |                     ; C34: 1
      |                     ; C35: 1
      |                     ; C36: 1
      |                     ; C45: 1
      |                     ; C46: 1
      |                     ; C47: 1
      |                     ; U9: 6(VCC)
      |                     ; U10: 6(VIN), 7(VIN)
      |                     ; U11: 3(+VOUT)
      |                     ; U12: 1(+VIN)
      | 接続部品数　　　　　; 11部品（部品番号で集計。同一ネット全体）
      | 接続端子数　　　　　; 12端子（423端子の部品対応表で集計。ラベル・境界ポートの重複は含めない）
      | この場所の端子数　　; 5端子／4部品（同名ラベルによる接続を除く）
      | 同階層同名ラベル数　; 4個（このラベル自身を含む）
      | 全階層の接続ラベル　; 4個（実際に同じノードへつながるラベル。名前が違う別名も含む）
      | 接続ルール　　　　　; 同じ階層の同じラベル名を仮想配線として結ぶ。別のSubsystem内とは名前だけでつながらず、明示的なConnection Portと配線をたどる。色は用途の表示であり接続を決めない。
      | 確認の範囲　　　　　; 現在の保存回路の端子・配線から求めた静的接続。抵抗やICの内部を導線として短絡せずに集計した。説明の更新は動作シミュレーション、タイミング、実部品の性能・実機動作を保証するものではない。
      | 記録の基準　　　　　; measurement_label_layout_20261022_r01/after_layout_graph.json。部品対応表は端子名の対応付けにのみ使用。
      | 
      | 【この説明欄の略語・記号】
      | 用語1　　　　　　　 ; DC：Direct Current（直流）。ここでは直流電源または直流成分。DCバイアスはコンデンサに重なる直流電圧を指す。
      | 用語2　　　　　　　 ; DC/DC：DC-to-DC Converter（直流電圧変換器）。直流入力を別の直流電圧へ変換する電源回路。絶縁の有無は個々の部品説明で確認する。
      | 用語3　　　　　　　 ; HF：High Frequency（高周波）。速い電圧・電流変化に対応する成分。具体的な周波数帯は対象回路ごとに説明する。
      | 用語4　　　　　　　 ; X7R：セラミックコンデンサの温度特性記号。英語の頭文字ではなく分類コード。X＝下限−55 ℃、7＝上限+125 ℃、R＝その範囲の容量変化±15%。直流バイアスによる容量変化は別に確認する。
      | 用語5　　　　　　　 ; IC：Integrated Circuit（集積回路）。複数の電子素子と機能を小さな半導体チップに集積した部品。
      | 用語6　　　　　　　 ; MOSFET：Metal-Oxide-Semiconductor Field-Effect Transistor（金属・酸化膜・半導体構造の電界効果トランジスタ）。ゲートとソースの電圧でドレインとソースの導通を制御する素子。N-MOSはNチャネル型を表す。
      | 用語7　　　　　　　 ; GND：Ground（回路の基準電位・電流帰路）。この図の共通基準。保護接地や大地への接続を意味するとは限らない。
      | 用語8　　　　　　　 ; VIN/VOUT：入力電圧・出力電圧を表す端子／ネット名。INは入力、OUTは出力。電源変換器の電力端子なのか、検出用端子なのかは対象部品によって異なるため、端子と接続の説明に従う。
      | 用語9　　　　　　　 ; VCC/VDD/VEE/VS：ICの電源端子名。文字の歴史的な由来を現在の接続機能へ当てはめない。現回路のVEEはU8/U10では浮動基準SW、U9ではGND。各電圧・基準は端子と接続を参照する。
      | 用語10　　　　　　　; SW：Switching Node（スイッチング点）。主電力段の上下MOSFETとL1がつながる、電圧が高速に切り替わる点。GNDとは別電位。
  ReadLabel_U11_BAT_AUX : ConnectionLabel  Description=|  Label=BAT_AUX
      | この回路での名前　　; BAT_AUX
      | 種別　　　　　　　　; ConnectionLabel
      | この回路での役割　　; 補助電源入力ヒューズF1の出力と、12V電源モジュールU11の入力・入力コンデンサC40〜C44を結ぶ。
      | この場所の直接接続　; C40（12V補助電源入力バイパス群／2.2uF 100V X7R）: 1
      |                     ; C41（12V補助電源入力バイパス群／2.2uF 100V X7R）: 1
      |                     ; C42（12V補助電源入力バイパス群／2.2uF 100V X7R）: 1
      |                     ; C43（12V補助電源入力バイパス群／2.2uF 100V X7R）: 1
      |                     ; C44（12V補助電源入力バイパス群／2.2uF 100V X7R）: 1
      |                     ; U11（バッテリー補助分岐から12Vを作る電源モジュール／TSR 1-48120WI）: 1(+VIN)
      | 直接接続の範囲　　　; このラベルから実際の線・分岐・明示的な境界端子だけを追った接続。同名ラベルによる離れた場所への接続はこの欄に含めない。
      | 同一ネットの主接続　; F1（U11を含む補助電源入力の過電流に対処するために入れる／1.6A 300VDC time-lag T SMD）: 2
      |                     ; U11（バッテリー補助分岐から12Vを作る電源モジュール／TSR 1-48120WI）: 1(+VIN)
      |                     ; C40（12V補助電源入力バイパス群／2.2uF 100V X7R）: 1
      |                     ; C41（12V補助電源入力バイパス群／2.2uF 100V X7R）: 1
      |                     ; C42（12V補助電源入力バイパス群／2.2uF 100V X7R）: 1
      |                     ; C43（12V補助電源入力バイパス群／2.2uF 100V X7R）: 1
      |                     ; C44（12V補助電源入力バイパス群／2.2uF 100V X7R）: 1
      | 同一ネット全端子　　; C40: 1
      |                     ; C41: 1
      |                     ; C42: 1
      |                     ; C43: 1
      |                     ; C44: 1
      |                     ; F1: 2
      |                     ; U11: 1(+VIN)
      | 接続部品数　　　　　; 7部品（部品番号で集計。同一ネット全体）
      | 接続端子数　　　　　; 7端子（423端子の部品対応表で集計。ラベル・境界ポートの重複は含めない）
      | この場所の端子数　　; 6端子／6部品（同名ラベルによる接続を除く）
      | 同階層同名ラベル数　; 2個（このラベル自身を含む）
      | 全階層の接続ラベル　; 2個（実際に同じノードへつながるラベル。名前が違う別名も含む）
      | 接続ルール　　　　　; 同じ階層の同じラベル名を仮想配線として結ぶ。別のSubsystem内とは名前だけでつながらず、明示的なConnection Portと配線をたどる。色は用途の表示であり接続を決めない。
      | 確認の範囲　　　　　; 現在の保存回路の端子・配線から求めた静的接続。抵抗やICの内部を導線として短絡せずに集計した。説明の更新は動作シミュレーション、タイミング、実部品の性能・実機動作を保証するものではない。
      | 記録の基準　　　　　; measurement_label_layout_20261022_r01/after_layout_graph.json。部品対応表は端子名の対応付けにのみ使用。
      | 
      | 【この説明欄の略語・記号】
      | 用語1　　　　　　　 ; X7R：セラミックコンデンサの温度特性記号。英語の頭文字ではなく分類コード。X＝下限−55 ℃、7＝上限+125 ℃、R＝その範囲の容量変化±15%。直流バイアスによる容量変化は別に確認する。
      | 用語2　　　　　　　 ; IC：Integrated Circuit（集積回路）。複数の電子素子と機能を小さな半導体チップに集積した部品。
      | 用語3　　　　　　　 ; SMD：Surface-Mount Device（表面実装部品）。基板表面のパッドへはんだ付けする形式の部品。
      | 用語4　　　　　　　 ; VIN/VOUT：入力電圧・出力電圧を表す端子／ネット名。INは入力、OUTは出力。電源変換器の電力端子なのか、検出用端子なのかは対象部品によって異なるため、端子と接続の説明に従う。
  ReadLabel_U11_P12 : ConnectionLabel  Description=|  Label=P12
      | この回路での名前　　; P12
      | 種別　　　　　　　　; ConnectionLabel
      | この回路での役割　　; 12V電源モジュールU11の出力を、低側ゲートドライバU9、絶縁電源U10の一次側、5V電源モジュールU12へ分配する。
      | この場所の直接接続　; C45（12Vレギュレータ出力局所バイパス／22uF 25V X7R）: 1
      |                     ; C46（共通12Vバルク/過渡蓄積／470uF 25V hybrid）: 1
      |                     ; U11（バッテリー補助分岐から12Vを作る電源モジュール／TSR 1-48120WI）: 3(+VOUT)
      | 直接接続の範囲　　　; このラベルから実際の線・分岐・明示的な境界端子だけを追った接続。同名ラベルによる離れた場所への接続はこの欄に含めない。
      | 同一ネットの主接続　; U11（バッテリー補助分岐から12Vを作る電源モジュール／TSR 1-48120WI）: 3(+VOUT)
      |                     ; U9（低側の光ゲートドライバ／ACPL-P346-560E）: 6(VCC)
      |                     ; U10（高側ゲート用の浮動電源を作る絶縁DC/DC／UCC14131QDWNRQ1）: 6(VIN), 7(VIN)
      |                     ; U12（12Vから5Vを作る電源モジュール／TSR 1-2450）: 1(+VIN)
      |                     ; C45（12Vレギュレータ出力局所バイパス／22uF 25V X7R）: 1
      |                     ; C46（共通12Vバルク/過渡蓄積／470uF 25V hybrid）: 1
      |                     ; C47（5Vレギュレータ入力局所バイパス／1uF 50V X7R）: 1
      | 同一ネット全端子　　; C33: 1
      |                     ; C34: 1
      |                     ; C35: 1
      |                     ; C36: 1
      |                     ; C45: 1
      |                     ; C46: 1
      |                     ; C47: 1
      |                     ; U9: 6(VCC)
      |                     ; U10: 6(VIN), 7(VIN)
      |                     ; U11: 3(+VOUT)
      |                     ; U12: 1(+VIN)
      | 接続部品数　　　　　; 11部品（部品番号で集計。同一ネット全体）
      | 接続端子数　　　　　; 12端子（423端子の部品対応表で集計。ラベル・境界ポートの重複は含めない）
      | この場所の端子数　　; 3端子／3部品（同名ラベルによる接続を除く）
      | 同階層同名ラベル数　; 4個（このラベル自身を含む）
      | 全階層の接続ラベル　; 4個（実際に同じノードへつながるラベル。名前が違う別名も含む）
      | 接続ルール　　　　　; 同じ階層の同じラベル名を仮想配線として結ぶ。別のSubsystem内とは名前だけでつながらず、明示的なConnection Portと配線をたどる。色は用途の表示であり接続を決めない。
      | 確認の範囲　　　　　; 現在の保存回路の端子・配線から求めた静的接続。抵抗やICの内部を導線として短絡せずに集計した。説明の更新は動作シミュレーション、タイミング、実部品の性能・実機動作を保証するものではない。
      | 記録の基準　　　　　; measurement_label_layout_20261022_r01/after_layout_graph.json。部品対応表は端子名の対応付けにのみ使用。
      | 
      | 【この説明欄の略語・記号】
      | 用語1　　　　　　　 ; DC：Direct Current（直流）。ここでは直流電源または直流成分。DCバイアスはコンデンサに重なる直流電圧を指す。
      | 用語2　　　　　　　 ; DC/DC：DC-to-DC Converter（直流電圧変換器）。直流入力を別の直流電圧へ変換する電源回路。絶縁の有無は個々の部品説明で確認する。
      | 用語3　　　　　　　 ; X7R：セラミックコンデンサの温度特性記号。英語の頭文字ではなく分類コード。X＝下限−55 ℃、7＝上限+125 ℃、R＝その範囲の容量変化±15%。直流バイアスによる容量変化は別に確認する。
      | 用語4　　　　　　　 ; IC：Integrated Circuit（集積回路）。複数の電子素子と機能を小さな半導体チップに集積した部品。
      | 用語5　　　　　　　 ; MOSFET：Metal-Oxide-Semiconductor Field-Effect Transistor（金属・酸化膜・半導体構造の電界効果トランジスタ）。ゲートとソースの電圧でドレインとソースの導通を制御する素子。N-MOSはNチャネル型を表す。
      | 用語6　　　　　　　 ; GND：Ground（回路の基準電位・電流帰路）。この図の共通基準。保護接地や大地への接続を意味するとは限らない。
      | 用語7　　　　　　　 ; VIN/VOUT：入力電圧・出力電圧を表す端子／ネット名。INは入力、OUTは出力。電源変換器の電力端子なのか、検出用端子なのかは対象部品によって異なるため、端子と接続の説明に従う。
      | 用語8　　　　　　　 ; VCC/VDD/VEE/VS：ICの電源端子名。文字の歴史的な由来を現在の接続機能へ当てはめない。現回路のVEEはU8/U10では浮動基準SW、U9ではGND。各電圧・基準は端子と接続を参照する。
      | 用語9　　　　　　　 ; SW：Switching Node（スイッチング点）。主電力段の上下MOSFETとL1がつながる、電圧が高速に切り替わる点。GNDとは別電位。
  ReadLabel_U12_P12 : ConnectionLabel  Description=|  Label=P12
      | この回路での名前　　; P12
      | 種別　　　　　　　　; ConnectionLabel
      | この回路での役割　　; 12V電源モジュールU11の出力を、低側ゲートドライバU9、絶縁電源U10の一次側、5V電源モジュールU12へ分配する。
      | この場所の直接接続　; C47（5Vレギュレータ入力局所バイパス／1uF 50V X7R）: 1
      |                     ; U12（12Vから5Vを作る電源モジュール／TSR 1-2450）: 1(+VIN)
      | 直接接続の範囲　　　; このラベルから実際の線・分岐・明示的な境界端子だけを追った接続。同名ラベルによる離れた場所への接続はこの欄に含めない。
      | 同一ネットの主接続　; U11（バッテリー補助分岐から12Vを作る電源モジュール／TSR 1-48120WI）: 3(+VOUT)
      |                     ; U9（低側の光ゲートドライバ／ACPL-P346-560E）: 6(VCC)
      |                     ; U10（高側ゲート用の浮動電源を作る絶縁DC/DC／UCC14131QDWNRQ1）: 6(VIN), 7(VIN)
      |                     ; U12（12Vから5Vを作る電源モジュール／TSR 1-2450）: 1(+VIN)
      |                     ; C45（12Vレギュレータ出力局所バイパス／22uF 25V X7R）: 1
      |                     ; C46（共通12Vバルク/過渡蓄積／470uF 25V hybrid）: 1
      |                     ; C47（5Vレギュレータ入力局所バイパス／1uF 50V X7R）: 1
      | 同一ネット全端子　　; C33: 1
      |                     ; C34: 1
      |                     ; C35: 1
      |                     ; C36: 1
      |                     ; C45: 1
      |                     ; C46: 1
      |                     ; C47: 1
      |                     ; U9: 6(VCC)
      |                     ; U10: 6(VIN), 7(VIN)
      |                     ; U11: 3(+VOUT)
      |                     ; U12: 1(+VIN)
      | 接続部品数　　　　　; 11部品（部品番号で集計。同一ネット全体）
      | 接続端子数　　　　　; 12端子（423端子の部品対応表で集計。ラベル・境界ポートの重複は含めない）
      | この場所の端子数　　; 2端子／2部品（同名ラベルによる接続を除く）
      | 同階層同名ラベル数　; 4個（このラベル自身を含む）
      | 全階層の接続ラベル　; 4個（実際に同じノードへつながるラベル。名前が違う別名も含む）
      | 接続ルール　　　　　; 同じ階層の同じラベル名を仮想配線として結ぶ。別のSubsystem内とは名前だけでつながらず、明示的なConnection Portと配線をたどる。色は用途の表示であり接続を決めない。
      | 確認の範囲　　　　　; 現在の保存回路の端子・配線から求めた静的接続。抵抗やICの内部を導線として短絡せずに集計した。説明の更新は動作シミュレーション、タイミング、実部品の性能・実機動作を保証するものではない。
      | 記録の基準　　　　　; measurement_label_layout_20261022_r01/after_layout_graph.json。部品対応表は端子名の対応付けにのみ使用。
      | 
      | 【この説明欄の略語・記号】
      | 用語1　　　　　　　 ; DC：Direct Current（直流）。ここでは直流電源または直流成分。DCバイアスはコンデンサに重なる直流電圧を指す。
      | 用語2　　　　　　　 ; DC/DC：DC-to-DC Converter（直流電圧変換器）。直流入力を別の直流電圧へ変換する電源回路。絶縁の有無は個々の部品説明で確認する。
      | 用語3　　　　　　　 ; X7R：セラミックコンデンサの温度特性記号。英語の頭文字ではなく分類コード。X＝下限−55 ℃、7＝上限+125 ℃、R＝その範囲の容量変化±15%。直流バイアスによる容量変化は別に確認する。
      | 用語4　　　　　　　 ; IC：Integrated Circuit（集積回路）。複数の電子素子と機能を小さな半導体チップに集積した部品。
      | 用語5　　　　　　　 ; MOSFET：Metal-Oxide-Semiconductor Field-Effect Transistor（金属・酸化膜・半導体構造の電界効果トランジスタ）。ゲートとソースの電圧でドレインとソースの導通を制御する素子。N-MOSはNチャネル型を表す。
      | 用語6　　　　　　　 ; GND：Ground（回路の基準電位・電流帰路）。この図の共通基準。保護接地や大地への接続を意味するとは限らない。
      | 用語7　　　　　　　 ; VIN/VOUT：入力電圧・出力電圧を表す端子／ネット名。INは入力、OUTは出力。電源変換器の電力端子なのか、検出用端子なのかは対象部品によって異なるため、端子と接続の説明に従う。
      | 用語8　　　　　　　 ; VCC/VDD/VEE/VS：ICの電源端子名。文字の歴史的な由来を現在の接続機能へ当てはめない。現回路のVEEはU8/U10では浮動基準SW、U9ではGND。各電圧・基準は端子と接続を参照する。
      | 用語9　　　　　　　 ; SW：Switching Node（スイッチング点）。主電力段の上下MOSFETとL1がつながる、電圧が高速に切り替わる点。GNDとは別電位。
  ReadLabel_U12_P5 : ConnectionLabel  Description=|  Label=P5
      | この回路での名前　　; P5
      | 種別　　　　　　　　; ConnectionLabel
      | この回路での役割　　; 5V電源モジュールU12の出力を、ゲートドライバ入力LEDの電流制限抵抗とRP2040電源用ダイオードD3へ分配する。
      | この場所の直接接続　; C48（5V出力局所バルク／22uF 25V X7R）: 1
      |                     ; D3（DIODE／40V 1A Schottky VSYS OR）: 2(A)
      |                     ; U12（12Vから5Vを作る電源モジュール／TSR 1-2450）: 3(+VOUT)
      | 直接接続の範囲　　　; このラベルから実際の線・分岐・明示的な境界端子だけを追った接続。同名ラベルによる離れた場所への接続はこの欄に含めない。
      | 同一ネットの主接続　; U12（12Vから5Vを作る電源モジュール／TSR 1-2450）: 3(+VOUT)
      |                     ; C48（5V出力局所バルク／22uF 25V X7R）: 1
      |                     ; R31（P5からU8のLEDへ流す電流をR32とともに制限する／232 ohm 1% 0.125W）: 1
      |                     ; R38（P5からU9のLEDへ流す電流をR39とともに制限する／232 ohm 1% 0.125W）: 1
      |                     ; D3（DIODE／40V 1A Schottky VSYS OR）: 2(A)
      | 同一ネット全端子　　; C48: 1
      |                     ; D3: 2(A)
      |                     ; R31: 1
      |                     ; R38: 1
      |                     ; U12: 3(+VOUT)
      | 接続部品数　　　　　; 5部品（部品番号で集計。同一ネット全体）
      | 接続端子数　　　　　; 5端子（423端子の部品対応表で集計。ラベル・境界ポートの重複は含めない）
      | この場所の端子数　　; 3端子／3部品（同名ラベルによる接続を除く）
      | 同階層同名ラベル数　; 3個（このラベル自身を含む）
      | 全階層の接続ラベル　; 3個（実際に同じノードへつながるラベル。名前が違う別名も含む）
      | 接続ルール　　　　　; 同じ階層の同じラベル名を仮想配線として結ぶ。別のSubsystem内とは名前だけでつながらず、明示的なConnection Portと配線をたどる。色は用途の表示であり接続を決めない。
      | 確認の範囲　　　　　; 現在の保存回路の端子・配線から求めた静的接続。抵抗やICの内部を導線として短絡せずに集計した。説明の更新は動作シミュレーション、タイミング、実部品の性能・実機動作を保証するものではない。
      | 記録の基準　　　　　; measurement_label_layout_20261022_r01/after_layout_graph.json。部品対応表は端子名の対応付けにのみ使用。
      | 
      | 【この説明欄の略語・記号】
      | 用語1　　　　　　　 ; X7R：セラミックコンデンサの温度特性記号。英語の頭文字ではなく分類コード。X＝下限−55 ℃、7＝上限+125 ℃、R＝その範囲の容量変化±15%。直流バイアスによる容量変化は別に確認する。
      | 用語2　　　　　　　 ; IC：Integrated Circuit（集積回路）。複数の電子素子と機能を小さな半導体チップに集積した部品。
      | 用語3　　　　　　　 ; LED：Light-Emitting Diode（発光ダイオード）。本回路のゲートドライバ入力では光によって信号を伝え、入力側と出力側を絶縁するために用いる。
      | 用語4　　　　　　　 ; VIN/VOUT：入力電圧・出力電圧を表す端子／ネット名。INは入力、OUTは出力。電源変換器の電力端子なのか、検出用端子なのかは対象部品によって異なるため、端子と接続の説明に従う。
  ReadLabel_U1_SPI_MISO : ConnectionLabel  Description=|  Label=SPI_MISO
      | この回路での名前　　; SPI_MISO
      | 種別　　　　　　　　; ConnectionLabel
      | この回路での役割　　; 外付けADC U1のDOUTから、RP2040基板U7のGP16へ測定データを送るSPI信号。測定値を運ぶが、この線はアナログ電圧測定線ではなくデジタル通信線。
      | この場所の直接接続　; U1（外付けADC／MCP3208-CI/SL）: 12(DOUT)
      | 直接接続の範囲　　　; このラベルから実際の線・分岐・明示的な境界端子だけを追った接続。同名ラベルによる離れた場所への接続はこの欄に含めない。
      | 同一ネットの主接続　; U1（外付けADC／MCP3208-CI/SL）: 12(DOUT)
      |                     ; U7（RP2040搭載Pico W／SC0918）: 21(GP16)
      | 同一ネット全端子　　; U1: 12(DOUT)
      |                     ; U7: 21(GP16)
      | 接続部品数　　　　　; 2部品（部品番号で集計。同一ネット全体）
      | 接続端子数　　　　　; 2端子（423端子の部品対応表で集計。ラベル・境界ポートの重複は含めない）
      | この場所の端子数　　; 1端子／1部品（同名ラベルによる接続を除く）
      | 同階層同名ラベル数　; 2個（このラベル自身を含む）
      | 全階層の接続ラベル　; 2個（実際に同じノードへつながるラベル。名前が違う別名も含む）
      | 接続ルール　　　　　; 同じ階層の同じラベル名を仮想配線として結ぶ。別のSubsystem内とは名前だけでつながらず、明示的なConnection Portと配線をたどる。色は用途の表示であり接続を決めない。
      | 確認の範囲　　　　　; 現在の保存回路の端子・配線から求めた静的接続。抵抗やICの内部を導線として短絡せずに集計した。説明の更新は動作シミュレーション、タイミング、実部品の性能・実機動作を保証するものではない。
      | 記録の基準　　　　　; measurement_label_layout_20261022_r01/after_layout_graph.json。部品対応表は端子名の対応付けにのみ使用。
      | 
      | 【この説明欄の略語・記号】
      | 用語1　　　　　　　 ; ADC：Analog-to-Digital Converter（アナログ・デジタル変換器）。測定電圧をデジタル値へ変換する回路。電流や温度も、センサーで電圧へ変換した後に読み取る。
      | 用語2　　　　　　　 ; IC：Integrated Circuit（集積回路）。複数の電子素子と機能を小さな半導体チップに集積した部品。
      | 用語3　　　　　　　 ; GPIO：General-Purpose Input/Output（汎用入出力端子）。入力・出力や周辺機能に割り当てられる端子。GPの後の数字はRP2040の端子信号番号で、基板上の物理ピン番号とは別。
      | 用語4　　　　　　　 ; SPI：Serial Peripheral Interface（同期式シリアル通信）。クロックとデータ線を使う通信方式。本回路ではRP2040と外付け測定用ADCの通信に使う。
      | 用語5　　　　　　　 ; MISO：Master In, Slave Out（制御側へ入るSPIデータ線）。この回路ではADCのDOUTからRP2040へ測定値が流れる。名称の主従は通信上の役割を表す。
      | 用語6　　　　　　　 ; DOUT：Data Out（データ出力端子）。ADC側から見た変換結果のデジタルデータ出力。
  ReadLabel_U1_SPI_MOSI : ConnectionLabel  Description=|  Label=SPI_MOSI
      | この回路での名前　　; SPI_MOSI
      | 種別　　　　　　　　; ConnectionLabel
      | この回路での役割　　; RP2040基板U7のGP19から、外付けADC U1のDINへ入力チャンネルなどの選択情報を送るSPI信号。
      | この場所の直接接続　; U1（外付けADC／MCP3208-CI/SL）: 11(DIN)
      | 直接接続の範囲　　　; このラベルから実際の線・分岐・明示的な境界端子だけを追った接続。同名ラベルによる離れた場所への接続はこの欄に含めない。
      | 同一ネットの主接続　; U7（RP2040搭載Pico W／SC0918）: 25(GP19)
      |                     ; U1（外付けADC／MCP3208-CI/SL）: 11(DIN)
      | 同一ネット全端子　　; U1: 11(DIN)
      |                     ; U7: 25(GP19)
      | 接続部品数　　　　　; 2部品（部品番号で集計。同一ネット全体）
      | 接続端子数　　　　　; 2端子（423端子の部品対応表で集計。ラベル・境界ポートの重複は含めない）
      | この場所の端子数　　; 1端子／1部品（同名ラベルによる接続を除く）
      | 同階層同名ラベル数　; 2個（このラベル自身を含む）
      | 全階層の接続ラベル　; 2個（実際に同じノードへつながるラベル。名前が違う別名も含む）
      | 接続ルール　　　　　; 同じ階層の同じラベル名を仮想配線として結ぶ。別のSubsystem内とは名前だけでつながらず、明示的なConnection Portと配線をたどる。色は用途の表示であり接続を決めない。
      | 確認の範囲　　　　　; 現在の保存回路の端子・配線から求めた静的接続。抵抗やICの内部を導線として短絡せずに集計した。説明の更新は動作シミュレーション、タイミング、実部品の性能・実機動作を保証するものではない。
      | 記録の基準　　　　　; measurement_label_layout_20261022_r01/after_layout_graph.json。部品対応表は端子名の対応付けにのみ使用。
      | 
      | 【この説明欄の略語・記号】
      | 用語1　　　　　　　 ; ADC：Analog-to-Digital Converter（アナログ・デジタル変換器）。測定電圧をデジタル値へ変換する回路。電流や温度も、センサーで電圧へ変換した後に読み取る。
      | 用語2　　　　　　　 ; IC：Integrated Circuit（集積回路）。複数の電子素子と機能を小さな半導体チップに集積した部品。
      | 用語3　　　　　　　 ; GPIO：General-Purpose Input/Output（汎用入出力端子）。入力・出力や周辺機能に割り当てられる端子。GPの後の数字はRP2040の端子信号番号で、基板上の物理ピン番号とは別。
      | 用語4　　　　　　　 ; SPI：Serial Peripheral Interface（同期式シリアル通信）。クロックとデータ線を使う通信方式。本回路ではRP2040と外付け測定用ADCの通信に使う。
      | 用語5　　　　　　　 ; MOSI：Master Out, Slave In（制御側から出るSPIデータ線）。この回路ではRP2040からADCのDINへ測定チャネル選択などの情報が流れる。
      | 用語6　　　　　　　 ; DIN：Data In（データ入力端子）。ADC側から見たデジタルデータ入力。測定対象のアナログ電圧入力とは別。
  ReadLabel_U1_SPI_SCK : ConnectionLabel  Description=|  Label=SPI_SCK
      | この回路での名前　　; SPI_SCK
      | 種別　　　　　　　　; ConnectionLabel
      | この回路での役割　　; RP2040基板U7のGP18から、外付けADC U1のCLKへ通信のタイミングを渡すSPIクロック線。
      | この場所の直接接続　; U1（外付けADC／MCP3208-CI/SL）: 13(CLK)
      | 直接接続の範囲　　　; このラベルから実際の線・分岐・明示的な境界端子だけを追った接続。同名ラベルによる離れた場所への接続はこの欄に含めない。
      | 同一ネットの主接続　; U7（RP2040搭載Pico W／SC0918）: 24(GP18)
      |                     ; U1（外付けADC／MCP3208-CI/SL）: 13(CLK)
      | 同一ネット全端子　　; U1: 13(CLK)
      |                     ; U7: 24(GP18)
      | 接続部品数　　　　　; 2部品（部品番号で集計。同一ネット全体）
      | 接続端子数　　　　　; 2端子（423端子の部品対応表で集計。ラベル・境界ポートの重複は含めない）
      | この場所の端子数　　; 1端子／1部品（同名ラベルによる接続を除く）
      | 同階層同名ラベル数　; 2個（このラベル自身を含む）
      | 全階層の接続ラベル　; 2個（実際に同じノードへつながるラベル。名前が違う別名も含む）
      | 接続ルール　　　　　; 同じ階層の同じラベル名を仮想配線として結ぶ。別のSubsystem内とは名前だけでつながらず、明示的なConnection Portと配線をたどる。色は用途の表示であり接続を決めない。
      | 確認の範囲　　　　　; 現在の保存回路の端子・配線から求めた静的接続。抵抗やICの内部を導線として短絡せずに集計した。説明の更新は動作シミュレーション、タイミング、実部品の性能・実機動作を保証するものではない。
      | 記録の基準　　　　　; measurement_label_layout_20261022_r01/after_layout_graph.json。部品対応表は端子名の対応付けにのみ使用。
      | 
      | 【この説明欄の略語・記号】
      | 用語1　　　　　　　 ; ADC：Analog-to-Digital Converter（アナログ・デジタル変換器）。測定電圧をデジタル値へ変換する回路。電流や温度も、センサーで電圧へ変換した後に読み取る。
      | 用語2　　　　　　　 ; IC：Integrated Circuit（集積回路）。複数の電子素子と機能を小さな半導体チップに集積した部品。
      | 用語3　　　　　　　 ; GPIO：General-Purpose Input/Output（汎用入出力端子）。入力・出力や周辺機能に割り当てられる端子。GPの後の数字はRP2040の端子信号番号で、基板上の物理ピン番号とは別。
      | 用語4　　　　　　　 ; SPI：Serial Peripheral Interface（同期式シリアル通信）。クロックとデータ線を使う通信方式。本回路ではRP2040と外付け測定用ADCの通信に使う。
      | 用語5　　　　　　　 ; SCK：Serial Clock（シリアル通信クロック）。SPIのデータを送り受けするタイミングを定める信号。
      | 用語6　　　　　　　 ; CLK：Clock（クロック端子）。データ転送などの動作タイミングを定める端子。
  ReadLabel_U1_V3V3 : ConnectionLabel  Description=|  Label=V3V3
      | この回路での名前　　; V3V3
      | 種別　　　　　　　　; ConnectionLabel
      | この回路での役割　　; RP2040基板U7の3.3V出力から、ADC・電流検出IC・温度センサー・基準電圧ICなどへ電源を分配する。信号のプルアップ抵抗にも供給する。
      | この場所の直接接続　; C17（ADC電源バイパス／100 nF）: 1
      |                     ; C18（3V3測定群の局所バルク／2.2 uF）: 1
      |                     ; U1（外付けADC／MCP3208-CI/SL）: 16(VDD)
      | 直接接続の範囲　　　; このラベルから実際の線・分岐・明示的な境界端子だけを追った接続。同名ラベルによる離れた場所への接続はこの欄に含めない。
      | 同一ネットの主接続　; U7（RP2040搭載Pico W／SC0918）: 36(3V3_OUT)
      |                     ; U1（外付けADC／MCP3208-CI/SL）: 16(VDD)
      |                     ; U2（PV入力電流の検出アンプ／INA241A3IDDFR）: 6(VS)
      |                     ; U3（L1直後の出力電流の検出アンプ／INA241A3IDDFR）: 6(VS)
      |                     ; U4（電池温度センサー／TMP235A2DBZR）: 1(VDD)
      |                     ; U5（放熱器温度センサー／TMP235A2DBZR）: 1(VDD)
      |                     ; U6（2.5Vの測定基準電圧源／REF3025EAIDBZR）: 1(IN)
      |                     ; R49（U10のオープンドレインPG信号BIAS_PGをPicoの3V3へ引き上げ、GP9で読める電圧にする／10k 1%）: 2
      |                     ; P_RFLT_PU（LTC4364のオープンドレインFLTをMCUの3.3 V系へ引き上げる／22 kΩ）: 1
      | 同一ネット全端子　　; C17: 1
      |                     ; C18: 1
      |                     ; C22: 1
      |                     ; C24: 1
      |                     ; C26: 1
      |                     ; C28: 1
      |                     ; C30: 1
      |                     ; P_RFLT_PU: 1
      |                     ; R15: 1
      |                     ; R49: 2
      |                     ; U1: 16(VDD)
      |                     ; U2: 6(VS)
      |                     ; U3: 6(VS)
      |                     ; U4: 1(VDD)
      |                     ; U5: 1(VDD)
      |                     ; U6: 1(IN)
      |                     ; U7: 36(3V3_OUT)
      | 接続部品数　　　　　; 17部品（部品番号で集計。同一ネット全体）
      | 接続端子数　　　　　; 17端子（423端子の部品対応表で集計。ラベル・境界ポートの重複は含めない）
      | この場所の端子数　　; 3端子／3部品（同名ラベルによる接続を除く）
      | 同階層同名ラベル数　; 10個（このラベル自身を含む）
      | 全階層の接続ラベル　; 10個（実際に同じノードへつながるラベル。名前が違う別名も含む）
      | 接続ルール　　　　　; 同じ階層の同じラベル名を仮想配線として結ぶ。別のSubsystem内とは名前だけでつながらず、明示的なConnection Portと配線をたどる。色は用途の表示であり接続を決めない。
      | 確認の範囲　　　　　; 現在の保存回路の端子・配線から求めた静的接続。抵抗やICの内部を導線として短絡せずに集計した。説明の更新は動作シミュレーション、タイミング、実部品の性能・実機動作を保証するものではない。
      | 記録の基準　　　　　; measurement_label_layout_20261022_r01/after_layout_graph.json。部品対応表は端子名の対応付けにのみ使用。
      | 
      | 【この説明欄の略語・記号】
      | 用語1　　　　　　　 ; ADC：Analog-to-Digital Converter（アナログ・デジタル変換器）。測定電圧をデジタル値へ変換する回路。電流や温度も、センサーで電圧へ変換した後に読み取る。
      | 用語2　　　　　　　 ; IC：Integrated Circuit（集積回路）。複数の電子素子と機能を小さな半導体チップに集積した部品。
      | 用語3　　　　　　　 ; MCU：Microcontroller Unit（マイクロコントローラ）。プログラムを実行し、測定値の処理や出力制御を担当する小型計算機。
      | 用語4　　　　　　　 ; GPIO：General-Purpose Input/Output（汎用入出力端子）。入力・出力や周辺機能に割り当てられる端子。GPの後の数字はRP2040の端子信号番号で、基板上の物理ピン番号とは別。
      | 用語5　　　　　　　 ; MOSFET：Metal-Oxide-Semiconductor Field-Effect Transistor（金属・酸化膜・半導体構造の電界効果トランジスタ）。ゲートとソースの電圧でドレインとソースの導通を制御する素子。N-MOSはNチャネル型を表す。
      | 用語6　　　　　　　 ; PV：Photovoltaic（太陽光発電）。光を電気へ変える発電方式。PVを含むネット名は太陽電池側の測定・電力経路を表す。
      | 用語7　　　　　　　 ; GND：Ground（回路の基準電位・電流帰路）。この図の共通基準。保護接地や大地への接続を意味するとは限らない。
      | 用語8　　　　　　　 ; PG：Power Good（電源状態通知）。電源出力が規定状態にあるかを知らせる信号。プルアップ条件と実際の通知条件は対象ICの説明で確認する。
      | 用語9　　　　　　　 ; FLT：Fault（故障状態通知）。LTC4364の故障警告出力。全種類の異常や逆流を一律に通知する信号という意味ではない。
      | 用語10　　　　　　　; VCC/VDD/VEE/VS：ICの電源端子名。文字の歴史的な由来を現在の接続機能へ当てはめない。現回路のVEEはU8/U10では浮動基準SW、U9ではGND。各電圧・基準は端子と接続を参照する。
      | 用語11　　　　　　　; SW：Switching Node（スイッチング点）。主電力段の上下MOSFETとL1がつながる、電圧が高速に切り替わる点。GNDとは別電位。
  ReadLabel_U3_V3V3 : ConnectionLabel  Description=|  Label=V3V3
      | この回路での名前　　; V3V3
      | 種別　　　　　　　　; ConnectionLabel
      | この回路での役割　　; RP2040基板U7の3.3V出力から、ADC・電流検出IC・温度センサー・基準電圧ICなどへ電源を分配する。信号のプルアップ抵抗にも供給する。
      | この場所の直接接続　; C24（電流検出IC電源バイパス／100nF 50V）: 1
      |                     ; U3（L1直後の出力電流の検出アンプ／INA241A3IDDFR）: 6(VS)
      | 直接接続の範囲　　　; このラベルから実際の線・分岐・明示的な境界端子だけを追った接続。同名ラベルによる離れた場所への接続はこの欄に含めない。
      | 同一ネットの主接続　; U7（RP2040搭載Pico W／SC0918）: 36(3V3_OUT)
      |                     ; U1（外付けADC／MCP3208-CI/SL）: 16(VDD)
      |                     ; U2（PV入力電流の検出アンプ／INA241A3IDDFR）: 6(VS)
      |                     ; U3（L1直後の出力電流の検出アンプ／INA241A3IDDFR）: 6(VS)
      |                     ; U4（電池温度センサー／TMP235A2DBZR）: 1(VDD)
      |                     ; U5（放熱器温度センサー／TMP235A2DBZR）: 1(VDD)
      |                     ; U6（2.5Vの測定基準電圧源／REF3025EAIDBZR）: 1(IN)
      |                     ; R49（U10のオープンドレインPG信号BIAS_PGをPicoの3V3へ引き上げ、GP9で読める電圧にする／10k 1%）: 2
      |                     ; P_RFLT_PU（LTC4364のオープンドレインFLTをMCUの3.3 V系へ引き上げる／22 kΩ）: 1
      | 同一ネット全端子　　; C17: 1
      |                     ; C18: 1
      |                     ; C22: 1
      |                     ; C24: 1
      |                     ; C26: 1
      |                     ; C28: 1
      |                     ; C30: 1
      |                     ; P_RFLT_PU: 1
      |                     ; R15: 1
      |                     ; R49: 2
      |                     ; U1: 16(VDD)
      |                     ; U2: 6(VS)
      |                     ; U3: 6(VS)
      |                     ; U4: 1(VDD)
      |                     ; U5: 1(VDD)
      |                     ; U6: 1(IN)
      |                     ; U7: 36(3V3_OUT)
      | 接続部品数　　　　　; 17部品（部品番号で集計。同一ネット全体）
      | 接続端子数　　　　　; 17端子（423端子の部品対応表で集計。ラベル・境界ポートの重複は含めない）
      | この場所の端子数　　; 2端子／2部品（同名ラベルによる接続を除く）
      | 同階層同名ラベル数　; 10個（このラベル自身を含む）
      | 全階層の接続ラベル　; 10個（実際に同じノードへつながるラベル。名前が違う別名も含む）
      | 接続ルール　　　　　; 同じ階層の同じラベル名を仮想配線として結ぶ。別のSubsystem内とは名前だけでつながらず、明示的なConnection Portと配線をたどる。色は用途の表示であり接続を決めない。
      | 確認の範囲　　　　　; 現在の保存回路の端子・配線から求めた静的接続。抵抗やICの内部を導線として短絡せずに集計した。説明の更新は動作シミュレーション、タイミング、実部品の性能・実機動作を保証するものではない。
      | 記録の基準　　　　　; measurement_label_layout_20261022_r01/after_layout_graph.json。部品対応表は端子名の対応付けにのみ使用。
      | 
      | 【この説明欄の略語・記号】
      | 用語1　　　　　　　 ; ADC：Analog-to-Digital Converter（アナログ・デジタル変換器）。測定電圧をデジタル値へ変換する回路。電流や温度も、センサーで電圧へ変換した後に読み取る。
      | 用語2　　　　　　　 ; IC：Integrated Circuit（集積回路）。複数の電子素子と機能を小さな半導体チップに集積した部品。
      | 用語3　　　　　　　 ; MCU：Microcontroller Unit（マイクロコントローラ）。プログラムを実行し、測定値の処理や出力制御を担当する小型計算機。
      | 用語4　　　　　　　 ; GPIO：General-Purpose Input/Output（汎用入出力端子）。入力・出力や周辺機能に割り当てられる端子。GPの後の数字はRP2040の端子信号番号で、基板上の物理ピン番号とは別。
      | 用語5　　　　　　　 ; MOSFET：Metal-Oxide-Semiconductor Field-Effect Transistor（金属・酸化膜・半導体構造の電界効果トランジスタ）。ゲートとソースの電圧でドレインとソースの導通を制御する素子。N-MOSはNチャネル型を表す。
      | 用語6　　　　　　　 ; PV：Photovoltaic（太陽光発電）。光を電気へ変える発電方式。PVを含むネット名は太陽電池側の測定・電力経路を表す。
      | 用語7　　　　　　　 ; GND：Ground（回路の基準電位・電流帰路）。この図の共通基準。保護接地や大地への接続を意味するとは限らない。
      | 用語8　　　　　　　 ; PG：Power Good（電源状態通知）。電源出力が規定状態にあるかを知らせる信号。プルアップ条件と実際の通知条件は対象ICの説明で確認する。
      | 用語9　　　　　　　 ; FLT：Fault（故障状態通知）。LTC4364の故障警告出力。全種類の異常や逆流を一律に通知する信号という意味ではない。
      | 用語10　　　　　　　; VCC/VDD/VEE/VS：ICの電源端子名。文字の歴史的な由来を現在の接続機能へ当てはめない。現回路のVEEはU8/U10では浮動基準SW、U9ではGND。各電圧・基準は端子と接続を参照する。
      | 用語11　　　　　　　; SW：Switching Node（スイッチング点）。主電力段の上下MOSFETとL1がつながる、電圧が高速に切り替わる点。GNDとは別電位。
  ReadLabel_U4_V3V3 : ConnectionLabel  Description=|  Label=V3V3
      | この回路での名前　　; V3V3
      | 種別　　　　　　　　; ConnectionLabel
      | この回路での役割　　; RP2040基板U7の3.3V出力から、ADC・電流検出IC・温度センサー・基準電圧ICなどへ電源を分配する。信号のプルアップ抵抗にも供給する。
      | この場所の直接接続　; C26（温度センサー電源バイパス／100 nF）: 1
      |                     ; U4（電池温度センサー／TMP235A2DBZR）: 1(VDD)
      | 直接接続の範囲　　　; このラベルから実際の線・分岐・明示的な境界端子だけを追った接続。同名ラベルによる離れた場所への接続はこの欄に含めない。
      | 同一ネットの主接続　; U7（RP2040搭載Pico W／SC0918）: 36(3V3_OUT)
      |                     ; U1（外付けADC／MCP3208-CI/SL）: 16(VDD)
      |                     ; U2（PV入力電流の検出アンプ／INA241A3IDDFR）: 6(VS)
      |                     ; U3（L1直後の出力電流の検出アンプ／INA241A3IDDFR）: 6(VS)
      |                     ; U4（電池温度センサー／TMP235A2DBZR）: 1(VDD)
      |                     ; U5（放熱器温度センサー／TMP235A2DBZR）: 1(VDD)
      |                     ; U6（2.5Vの測定基準電圧源／REF3025EAIDBZR）: 1(IN)
      |                     ; R49（U10のオープンドレインPG信号BIAS_PGをPicoの3V3へ引き上げ、GP9で読める電圧にする／10k 1%）: 2
      |                     ; P_RFLT_PU（LTC4364のオープンドレインFLTをMCUの3.3 V系へ引き上げる／22 kΩ）: 1
      | 同一ネット全端子　　; C17: 1
      |                     ; C18: 1
      |                     ; C22: 1
      |                     ; C24: 1
      |                     ; C26: 1
      |                     ; C28: 1
      |                     ; C30: 1
      |                     ; P_RFLT_PU: 1
      |                     ; R15: 1
      |                     ; R49: 2
      |                     ; U1: 16(VDD)
      |                     ; U2: 6(VS)
      |                     ; U3: 6(VS)
      |                     ; U4: 1(VDD)
      |                     ; U5: 1(VDD)
      |                     ; U6: 1(IN)
      |                     ; U7: 36(3V3_OUT)
      | 接続部品数　　　　　; 17部品（部品番号で集計。同一ネット全体）
      | 接続端子数　　　　　; 17端子（423端子の部品対応表で集計。ラベル・境界ポートの重複は含めない）
      | この場所の端子数　　; 2端子／2部品（同名ラベルによる接続を除く）
      | 同階層同名ラベル数　; 10個（このラベル自身を含む）
      | 全階層の接続ラベル　; 10個（実際に同じノードへつながるラベル。名前が違う別名も含む）
      | 接続ルール　　　　　; 同じ階層の同じラベル名を仮想配線として結ぶ。別のSubsystem内とは名前だけでつながらず、明示的なConnection Portと配線をたどる。色は用途の表示であり接続を決めない。
      | 確認の範囲　　　　　; 現在の保存回路の端子・配線から求めた静的接続。抵抗やICの内部を導線として短絡せずに集計した。説明の更新は動作シミュレーション、タイミング、実部品の性能・実機動作を保証するものではない。
      | 記録の基準　　　　　; measurement_label_layout_20261022_r01/after_layout_graph.json。部品対応表は端子名の対応付けにのみ使用。
      | 
      | 【この説明欄の略語・記号】
      | 用語1　　　　　　　 ; ADC：Analog-to-Digital Converter（アナログ・デジタル変換器）。測定電圧をデジタル値へ変換する回路。電流や温度も、センサーで電圧へ変換した後に読み取る。
      | 用語2　　　　　　　 ; IC：Integrated Circuit（集積回路）。複数の電子素子と機能を小さな半導体チップに集積した部品。
      | 用語3　　　　　　　 ; MCU：Microcontroller Unit（マイクロコントローラ）。プログラムを実行し、測定値の処理や出力制御を担当する小型計算機。
      | 用語4　　　　　　　 ; GPIO：General-Purpose Input/Output（汎用入出力端子）。入力・出力や周辺機能に割り当てられる端子。GPの後の数字はRP2040の端子信号番号で、基板上の物理ピン番号とは別。
      | 用語5　　　　　　　 ; MOSFET：Metal-Oxide-Semiconductor Field-Effect Transistor（金属・酸化膜・半導体構造の電界効果トランジスタ）。ゲートとソースの電圧でドレインとソースの導通を制御する素子。N-MOSはNチャネル型を表す。
      | 用語6　　　　　　　 ; PV：Photovoltaic（太陽光発電）。光を電気へ変える発電方式。PVを含むネット名は太陽電池側の測定・電力経路を表す。
      | 用語7　　　　　　　 ; GND：Ground（回路の基準電位・電流帰路）。この図の共通基準。保護接地や大地への接続を意味するとは限らない。
      | 用語8　　　　　　　 ; PG：Power Good（電源状態通知）。電源出力が規定状態にあるかを知らせる信号。プルアップ条件と実際の通知条件は対象ICの説明で確認する。
      | 用語9　　　　　　　 ; FLT：Fault（故障状態通知）。LTC4364の故障警告出力。全種類の異常や逆流を一律に通知する信号という意味ではない。
      | 用語10　　　　　　　; VCC/VDD/VEE/VS：ICの電源端子名。文字の歴史的な由来を現在の接続機能へ当てはめない。現回路のVEEはU8/U10では浮動基準SW、U9ではGND。各電圧・基準は端子と接続を参照する。
      | 用語11　　　　　　　; SW：Switching Node（スイッチング点）。主電力段の上下MOSFETとL1がつながる、電圧が高速に切り替わる点。GNDとは別電位。
  ReadLabel_U5_V3V3 : ConnectionLabel  Description=|  Label=V3V3
      | この回路での名前　　; V3V3
      | 種別　　　　　　　　; ConnectionLabel
      | この回路での役割　　; RP2040基板U7の3.3V出力から、ADC・電流検出IC・温度センサー・基準電圧ICなどへ電源を分配する。信号のプルアップ抵抗にも供給する。
      | この場所の直接接続　; C28（温度センサー電源バイパス／100 nF）: 1
      |                     ; U5（放熱器温度センサー／TMP235A2DBZR）: 1(VDD)
      | 直接接続の範囲　　　; このラベルから実際の線・分岐・明示的な境界端子だけを追った接続。同名ラベルによる離れた場所への接続はこの欄に含めない。
      | 同一ネットの主接続　; U7（RP2040搭載Pico W／SC0918）: 36(3V3_OUT)
      |                     ; U1（外付けADC／MCP3208-CI/SL）: 16(VDD)
      |                     ; U2（PV入力電流の検出アンプ／INA241A3IDDFR）: 6(VS)
      |                     ; U3（L1直後の出力電流の検出アンプ／INA241A3IDDFR）: 6(VS)
      |                     ; U4（電池温度センサー／TMP235A2DBZR）: 1(VDD)
      |                     ; U5（放熱器温度センサー／TMP235A2DBZR）: 1(VDD)
      |                     ; U6（2.5Vの測定基準電圧源／REF3025EAIDBZR）: 1(IN)
      |                     ; R49（U10のオープンドレインPG信号BIAS_PGをPicoの3V3へ引き上げ、GP9で読める電圧にする／10k 1%）: 2
      |                     ; P_RFLT_PU（LTC4364のオープンドレインFLTをMCUの3.3 V系へ引き上げる／22 kΩ）: 1
      | 同一ネット全端子　　; C17: 1
      |                     ; C18: 1
      |                     ; C22: 1
      |                     ; C24: 1
      |                     ; C26: 1
      |                     ; C28: 1
      |                     ; C30: 1
      |                     ; P_RFLT_PU: 1
      |                     ; R15: 1
      |                     ; R49: 2
      |                     ; U1: 16(VDD)
      |                     ; U2: 6(VS)
      |                     ; U3: 6(VS)
      |                     ; U4: 1(VDD)
      |                     ; U5: 1(VDD)
      |                     ; U6: 1(IN)
      |                     ; U7: 36(3V3_OUT)
      | 接続部品数　　　　　; 17部品（部品番号で集計。同一ネット全体）
      | 接続端子数　　　　　; 17端子（423端子の部品対応表で集計。ラベル・境界ポートの重複は含めない）
      | この場所の端子数　　; 2端子／2部品（同名ラベルによる接続を除く）
      | 同階層同名ラベル数　; 10個（このラベル自身を含む）
      | 全階層の接続ラベル　; 10個（実際に同じノードへつながるラベル。名前が違う別名も含む）
      | 接続ルール　　　　　; 同じ階層の同じラベル名を仮想配線として結ぶ。別のSubsystem内とは名前だけでつながらず、明示的なConnection Portと配線をたどる。色は用途の表示であり接続を決めない。
      | 確認の範囲　　　　　; 現在の保存回路の端子・配線から求めた静的接続。抵抗やICの内部を導線として短絡せずに集計した。説明の更新は動作シミュレーション、タイミング、実部品の性能・実機動作を保証するものではない。
      | 記録の基準　　　　　; measurement_label_layout_20261022_r01/after_layout_graph.json。部品対応表は端子名の対応付けにのみ使用。
      | 
      | 【この説明欄の略語・記号】
      | 用語1　　　　　　　 ; ADC：Analog-to-Digital Converter（アナログ・デジタル変換器）。測定電圧をデジタル値へ変換する回路。電流や温度も、センサーで電圧へ変換した後に読み取る。
      | 用語2　　　　　　　 ; IC：Integrated Circuit（集積回路）。複数の電子素子と機能を小さな半導体チップに集積した部品。
      | 用語3　　　　　　　 ; MCU：Microcontroller Unit（マイクロコントローラ）。プログラムを実行し、測定値の処理や出力制御を担当する小型計算機。
      | 用語4　　　　　　　 ; GPIO：General-Purpose Input/Output（汎用入出力端子）。入力・出力や周辺機能に割り当てられる端子。GPの後の数字はRP2040の端子信号番号で、基板上の物理ピン番号とは別。
      | 用語5　　　　　　　 ; MOSFET：Metal-Oxide-Semiconductor Field-Effect Transistor（金属・酸化膜・半導体構造の電界効果トランジスタ）。ゲートとソースの電圧でドレインとソースの導通を制御する素子。N-MOSはNチャネル型を表す。
      | 用語6　　　　　　　 ; PV：Photovoltaic（太陽光発電）。光を電気へ変える発電方式。PVを含むネット名は太陽電池側の測定・電力経路を表す。
      | 用語7　　　　　　　 ; GND：Ground（回路の基準電位・電流帰路）。この図の共通基準。保護接地や大地への接続を意味するとは限らない。
      | 用語8　　　　　　　 ; PG：Power Good（電源状態通知）。電源出力が規定状態にあるかを知らせる信号。プルアップ条件と実際の通知条件は対象ICの説明で確認する。
      | 用語9　　　　　　　 ; FLT：Fault（故障状態通知）。LTC4364の故障警告出力。全種類の異常や逆流を一律に通知する信号という意味ではない。
      | 用語10　　　　　　　; VCC/VDD/VEE/VS：ICの電源端子名。文字の歴史的な由来を現在の接続機能へ当てはめない。現回路のVEEはU8/U10では浮動基準SW、U9ではGND。各電圧・基準は端子と接続を参照する。
      | 用語11　　　　　　　; SW：Switching Node（スイッチング点）。主電力段の上下MOSFETとL1がつながる、電圧が高速に切り替わる点。GNDとは別電位。
  ReadLabel_U6_V3V3 : ConnectionLabel  Description=|  Label=V3V3
      | この回路での名前　　; V3V3
      | 種別　　　　　　　　; ConnectionLabel
      | この回路での役割　　; RP2040基板U7の3.3V出力から、ADC・電流検出IC・温度センサー・基準電圧ICなどへ電源を分配する。信号のプルアップ抵抗にも供給する。
      | この場所の直接接続　; C30（基準源入力バイパス／1 uF）: 1
      |                     ; U6（2.5Vの測定基準電圧源／REF3025EAIDBZR）: 1(IN)
      | 直接接続の範囲　　　; このラベルから実際の線・分岐・明示的な境界端子だけを追った接続。同名ラベルによる離れた場所への接続はこの欄に含めない。
      | 同一ネットの主接続　; U7（RP2040搭載Pico W／SC0918）: 36(3V3_OUT)
      |                     ; U1（外付けADC／MCP3208-CI/SL）: 16(VDD)
      |                     ; U2（PV入力電流の検出アンプ／INA241A3IDDFR）: 6(VS)
      |                     ; U3（L1直後の出力電流の検出アンプ／INA241A3IDDFR）: 6(VS)
      |                     ; U4（電池温度センサー／TMP235A2DBZR）: 1(VDD)
      |                     ; U5（放熱器温度センサー／TMP235A2DBZR）: 1(VDD)
      |                     ; U6（2.5Vの測定基準電圧源／REF3025EAIDBZR）: 1(IN)
      |                     ; R49（U10のオープンドレインPG信号BIAS_PGをPicoの3V3へ引き上げ、GP9で読める電圧にする／10k 1%）: 2
      |                     ; P_RFLT_PU（LTC4364のオープンドレインFLTをMCUの3.3 V系へ引き上げる／22 kΩ）: 1
      | 同一ネット全端子　　; C17: 1
      |                     ; C18: 1
      |                     ; C22: 1
      |                     ; C24: 1
      |                     ; C26: 1
      |                     ; C28: 1
      |                     ; C30: 1
      |                     ; P_RFLT_PU: 1
      |                     ; R15: 1
      |                     ; R49: 2
      |                     ; U1: 16(VDD)
      |                     ; U2: 6(VS)
      |                     ; U3: 6(VS)
      |                     ; U4: 1(VDD)
      |                     ; U5: 1(VDD)
      |                     ; U6: 1(IN)
      |                     ; U7: 36(3V3_OUT)
      | 接続部品数　　　　　; 17部品（部品番号で集計。同一ネット全体）
      | 接続端子数　　　　　; 17端子（423端子の部品対応表で集計。ラベル・境界ポートの重複は含めない）
      | この場所の端子数　　; 2端子／2部品（同名ラベルによる接続を除く）
      | 同階層同名ラベル数　; 10個（このラベル自身を含む）
      | 全階層の接続ラベル　; 10個（実際に同じノードへつながるラベル。名前が違う別名も含む）
      | 接続ルール　　　　　; 同じ階層の同じラベル名を仮想配線として結ぶ。別のSubsystem内とは名前だけでつながらず、明示的なConnection Portと配線をたどる。色は用途の表示であり接続を決めない。
      | 確認の範囲　　　　　; 現在の保存回路の端子・配線から求めた静的接続。抵抗やICの内部を導線として短絡せずに集計した。説明の更新は動作シミュレーション、タイミング、実部品の性能・実機動作を保証するものではない。
      | 記録の基準　　　　　; measurement_label_layout_20261022_r01/after_layout_graph.json。部品対応表は端子名の対応付けにのみ使用。
      | 
      | 【この説明欄の略語・記号】
      | 用語1　　　　　　　 ; ADC：Analog-to-Digital Converter（アナログ・デジタル変換器）。測定電圧をデジタル値へ変換する回路。電流や温度も、センサーで電圧へ変換した後に読み取る。
      | 用語2　　　　　　　 ; IC：Integrated Circuit（集積回路）。複数の電子素子と機能を小さな半導体チップに集積した部品。
      | 用語3　　　　　　　 ; MCU：Microcontroller Unit（マイクロコントローラ）。プログラムを実行し、測定値の処理や出力制御を担当する小型計算機。
      | 用語4　　　　　　　 ; GPIO：General-Purpose Input/Output（汎用入出力端子）。入力・出力や周辺機能に割り当てられる端子。GPの後の数字はRP2040の端子信号番号で、基板上の物理ピン番号とは別。
      | 用語5　　　　　　　 ; MOSFET：Metal-Oxide-Semiconductor Field-Effect Transistor（金属・酸化膜・半導体構造の電界効果トランジスタ）。ゲートとソースの電圧でドレインとソースの導通を制御する素子。N-MOSはNチャネル型を表す。
      | 用語6　　　　　　　 ; PV：Photovoltaic（太陽光発電）。光を電気へ変える発電方式。PVを含むネット名は太陽電池側の測定・電力経路を表す。
      | 用語7　　　　　　　 ; GND：Ground（回路の基準電位・電流帰路）。この図の共通基準。保護接地や大地への接続を意味するとは限らない。
      | 用語8　　　　　　　 ; PG：Power Good（電源状態通知）。電源出力が規定状態にあるかを知らせる信号。プルアップ条件と実際の通知条件は対象ICの説明で確認する。
      | 用語9　　　　　　　 ; FLT：Fault（故障状態通知）。LTC4364の故障警告出力。全種類の異常や逆流を一律に通知する信号という意味ではない。
      | 用語10　　　　　　　; VCC/VDD/VEE/VS：ICの電源端子名。文字の歴史的な由来を現在の接続機能へ当てはめない。現回路のVEEはU8/U10では浮動基準SW、U9ではGND。各電圧・基準は端子と接続を参照する。
      | 用語11　　　　　　　; SW：Switching Node（スイッチング点）。主電力段の上下MOSFETとL1がつながる、電圧が高速に切り替わる点。GNDとは別電位。
  ReadLabel_U7_BIAS_EN : ConnectionLabel  Description=|  Label=BIAS_EN
      | この回路での名前　　; BIAS_EN
      | 種別　　　　　　　　; ConnectionLabel
      | この回路での役割　　; RP2040基板U7のGP8と、絶縁電源U10のENA入力を結ぶ有効化指令線。R48はこの指令線のプルダウン。電源出力そのものではない。
      | この場所の直接接続　; U7（RP2040搭載Pico W）: 11(GP8)
      | 　　　　　　　　　　; R48（10 kΩ、プルダウン）: 1
      | 直接接続の範囲　　　; このラベルから実際の線・分岐・明示的な境界端子だけを追った接続。同名ラベルによる離れた場所への接続はこの欄に含めない。
      | 同一ネットの主接続　; U7（RP2040搭載Pico W／SC0918）: 11(GP8)
      |                     ; U10（高側ゲート用の浮動電源を作る絶縁DC/DC／UCC14131QDWNRQ1）: 4(ENA)
      |                     ; R48（BIAS_ENをGNDへ引き下げ、RP2040未駆動時のU10停止側の状態を作る／10k 1%）: 1
      | 同一ネット全端子　　; R48: 1
      |                     ; U7: 11(GP8)
      |                     ; U10: 4(ENA)
      | 接続部品数　　　　　; 3部品（部品番号で集計。同一ネット全体）
      | 接続端子数　　　　　; 3端子（423端子の部品対応表で集計。ラベル・境界ポートの重複は含めない）
      | この場所の端子数　　; 2端子／2部品（同名ラベルによる接続を除く）
      | 同階層同名ラベル数　; 2個（このラベル自身を含む）
      | 全階層の接続ラベル　; 2個（実際に同じノードへつながるラベル）
      | 接続ルール　　　　　; 同じ階層の同じラベル名を仮想配線として結ぶ。別のSubsystem内とは名前だけでつながらず、明示的なConnection Portと配線をたどる。色は用途の表示であり接続を決めない。
      | 確認の範囲　　　　　; 現在の保存回路の端子・配線から求めた静的接続。抵抗やICの内部を導線として短絡せずに集計した。説明の更新は動作シミュレーション、タイミング、実部品の性能・実機動作を保証するものではない。
      | 記録の基準　　　　　; bias_resistor_layout_20261022_r01/final_layout_graph.json。実際の配線・端子・同階層ラベルから確認。
      | 
      | 【この説明欄の略語・記号】
      | 用語1　　　　　　　 ; DC：Direct Current（直流）。ここでは直流電源または直流成分。DCバイアスはコンデンサに重なる直流電圧を指す。
      | 用語2　　　　　　　 ; DC/DC：DC-to-DC Converter（直流電圧変換器）。直流入力を別の直流電圧へ変換する電源回路。絶縁の有無は個々の部品説明で確認する。
      | 用語3　　　　　　　 ; IC：Integrated Circuit（集積回路）。複数の電子素子と機能を小さな半導体チップに集積した部品。
      | 用語4　　　　　　　 ; GPIO：General-Purpose Input/Output（汎用入出力端子）。入力・出力や周辺機能に割り当てられる端子。GPの後の数字はRP2040の端子信号番号で、基板上の物理ピン番号とは別。
      | 用語5　　　　　　　 ; GND：Ground（回路の基準電位・電流帰路）。この図の共通基準。保護接地や大地への接続を意味するとは限らない。
      | 用語6　　　　　　　 ; EN：Enable（動作許可）。対象機能の動作を許可する信号。端子ごとの有効レベルや接続状態に従う。
      | 
      | 【信号と抵抗の役割】
      | 名前の意味　　　　　; BIASは英単語Bias（バイアス）で、この図ではゲート駆動用の補助電源を指す。EN = Enable（動作許可）、PG = Power Good（電源状態通知）。ラベルは部品ではなく、同じ階層の同名ノードとの接続を示す。
      | 動作と論理状態　　　; U7のGP8とU10のENA（4番）は同じノード。Highで絶縁電源の動作を許可し、Lowで停止を指示する。R48はそのノードからGNDへの10 kΩプルダウンで、マイコン端子が駆動されない間のLow側の状態を作る。
      | メーカー根拠　　　　; https://www.ti.com/lit/gpn/ucc14131-q1（UCC14131-Q1データシート、端子表と11.3.3）
  ReadLabel_U7_BIAS_PG : ConnectionLabel  Description=|  Label=BIAS_PG
      | この回路での名前　　; BIAS_PG
      | 種別　　　　　　　　; ConnectionLabel
      | この回路での役割　　; 絶縁電源U10のPG出力から、RP2040基板U7のGP9へ電源の状態を返す。R49を介して3.3Vへプルアップされる。停止指令とは別の状態信号。
      | この場所の直接接続　; U7（RP2040搭載Pico W）: 12(GP9)
      | 　　　　　　　　　　; R49（10 kΩ、プルアップ）: 1
      | 直接接続の範囲　　　; このラベルから実際の線・分岐・明示的な境界端子だけを追った接続。同名ラベルによる離れた場所への接続はこの欄に含めない。
      | 同一ネットの主接続　; U10（高側ゲート用の浮動電源を作る絶縁DC/DC／UCC14131QDWNRQ1）: 3(PG)
      |                     ; U7（RP2040搭載Pico W／SC0918）: 12(GP9)
      |                     ; R49（U10のオープンドレインPG信号BIAS_PGをPicoの3V3へ引き上げ、GP9で読める電圧にする／10k 1%）: 1
      | 同一ネット全端子　　; R49: 1
      |                     ; U7: 12(GP9)
      |                     ; U10: 3(PG)
      | 接続部品数　　　　　; 3部品（部品番号で集計。同一ネット全体）
      | 接続端子数　　　　　; 3端子（423端子の部品対応表で集計。ラベル・境界ポートの重複は含めない）
      | この場所の端子数　　; 2端子／2部品（同名ラベルによる接続を除く）
      | 同階層同名ラベル数　; 2個（このラベル自身を含む）
      | 全階層の接続ラベル　; 2個（実際に同じノードへつながるラベル）
      | 接続ルール　　　　　; 同じ階層の同じラベル名を仮想配線として結ぶ。別のSubsystem内とは名前だけでつながらず、明示的なConnection Portと配線をたどる。色は用途の表示であり接続を決めない。
      | 確認の範囲　　　　　; 現在の保存回路の端子・配線から求めた静的接続。抵抗やICの内部を導線として短絡せずに集計した。説明の更新は動作シミュレーション、タイミング、実部品の性能・実機動作を保証するものではない。
      | 記録の基準　　　　　; bias_resistor_layout_20261022_r01/final_layout_graph.json。実際の配線・端子・同階層ラベルから確認。
      | 
      | 【この説明欄の略語・記号】
      | 用語1　　　　　　　 ; DC：Direct Current（直流）。ここでは直流電源または直流成分。DCバイアスはコンデンサに重なる直流電圧を指す。
      | 用語2　　　　　　　 ; DC/DC：DC-to-DC Converter（直流電圧変換器）。直流入力を別の直流電圧へ変換する電源回路。絶縁の有無は個々の部品説明で確認する。
      | 用語3　　　　　　　 ; IC：Integrated Circuit（集積回路）。複数の電子素子と機能を小さな半導体チップに集積した部品。
      | 用語4　　　　　　　 ; GPIO：General-Purpose Input/Output（汎用入出力端子）。入力・出力や周辺機能に割り当てられる端子。GPの後の数字はRP2040の端子信号番号で、基板上の物理ピン番号とは別。
      | 用語5　　　　　　　 ; PG：Power Good（電源状態通知）。電源出力が規定状態にあるかを知らせる信号。プルアップ条件と実際の通知条件は対象ICの説明で確認する。
      | 
      | 【信号と抵抗の役割】
      | 名前の意味　　　　　; BIASは英単語Bias（バイアス）で、この図ではゲート駆動用の補助電源を指す。EN = Enable（動作許可）、PG = Power Good（電源状態通知）。ラベルは部品ではなく、同じ階層の同名ノードとの接続を示す。
      | 動作と論理状態　　　; U10のPG（3番）からU7のGP9へ状態を返す。U10の正常成立時は内部出力がLowへ引き込み、正常不成立・停止時は出力を解放する。R49は解放時のノードを3.3 Vへ引き上げる10 kΩプルアップ。GP9は入力として読む。Highが正常という意味ではない。
      | メーカー根拠　　　　; https://www.ti.com/lit/gpn/ucc14131-q1（UCC14131-Q1データシート、端子表と11.3.3）
  ReadLabel_U7_SPI_CS_N : ConnectionLabel  Description=|  Label=SPI_CS_N
      | この回路での名前　　; SPI_CS_N
      | 種別　　　　　　　　; ConnectionLabel
      | この回路での役割　　; RP2040基板U7のGP17と、外付けADC U1のCS_Nを結ぶSPIチップ選択信号。R15によって3.3Vへプルアップする。
      | この場所の直接接続　; U7（RP2040搭載Pico W／SC0918）: 22(GP17)
      | 直接接続の範囲　　　; このラベルから実際の線・分岐・明示的な境界端子だけを追った接続。同名ラベルによる離れた場所への接続はこの欄に含めない。
      | 同一ネットの主接続　; U7（RP2040搭載Pico W／SC0918）: 22(GP17)
      |                     ; U1（外付けADC／MCP3208-CI/SL）: 10(CS_N)
      |                     ; R15（SPI_CS_Nを3V3へ引き上げ、RP2040の出力が未確定なときにU1を非選択側へ保つ／10 kohm）: 2
      | 同一ネット全端子　　; R15: 2
      |                     ; U1: 10(CS_N)
      |                     ; U7: 22(GP17)
      | 接続部品数　　　　　; 3部品（部品番号で集計。同一ネット全体）
      | 接続端子数　　　　　; 3端子（423端子の部品対応表で集計。ラベル・境界ポートの重複は含めない）
      | この場所の端子数　　; 1端子／1部品（同名ラベルによる接続を除く）
      | 同階層同名ラベル数　; 3個（このラベル自身を含む）
      | 全階層の接続ラベル　; 3個（実際に同じノードへつながるラベル。名前が違う別名も含む）
      | 接続ルール　　　　　; 同じ階層の同じラベル名を仮想配線として結ぶ。別のSubsystem内とは名前だけでつながらず、明示的なConnection Portと配線をたどる。色は用途の表示であり接続を決めない。
      | 確認の範囲　　　　　; 現在の保存回路の端子・配線から求めた静的接続。抵抗やICの内部を導線として短絡せずに集計した。説明の更新は動作シミュレーション、タイミング、実部品の性能・実機動作を保証するものではない。
      | 記録の基準　　　　　; measurement_label_layout_20261022_r01/after_layout_graph.json。部品対応表は端子名の対応付けにのみ使用。
      | 
      | 【この説明欄の略語・記号】
      | 用語1　　　　　　　 ; ADC：Analog-to-Digital Converter（アナログ・デジタル変換器）。測定電圧をデジタル値へ変換する回路。電流や温度も、センサーで電圧へ変換した後に読み取る。
      | 用語2　　　　　　　 ; IC：Integrated Circuit（集積回路）。複数の電子素子と機能を小さな半導体チップに集積した部品。
      | 用語3　　　　　　　 ; GPIO：General-Purpose Input/Output（汎用入出力端子）。入力・出力や周辺機能に割り当てられる端子。GPの後の数字はRP2040の端子信号番号で、基板上の物理ピン番号とは別。
      | 用語4　　　　　　　 ; SPI：Serial Peripheral Interface（同期式シリアル通信）。クロックとデータ線を使う通信方式。本回路ではRP2040と外付け測定用ADCの通信に使う。
      | 用語5　　　　　　　 ; CS_N：Chip Select（チップ選択信号）。末尾Nはこの設計でLow有効を表す。Lowにして通信対象のADCを選択する。
  ReadLabel_U7_SPI_MISO : ConnectionLabel  Description=|  Label=SPI_MISO
      | この回路での名前　　; SPI_MISO
      | 種別　　　　　　　　; ConnectionLabel
      | この回路での役割　　; 外付けADC U1のDOUTから、RP2040基板U7のGP16へ測定データを送るSPI信号。測定値を運ぶが、この線はアナログ電圧測定線ではなくデジタル通信線。
      | この場所の直接接続　; U7（RP2040搭載Pico W／SC0918）: 21(GP16)
      | 直接接続の範囲　　　; このラベルから実際の線・分岐・明示的な境界端子だけを追った接続。同名ラベルによる離れた場所への接続はこの欄に含めない。
      | 同一ネットの主接続　; U1（外付けADC／MCP3208-CI/SL）: 12(DOUT)
      |                     ; U7（RP2040搭載Pico W／SC0918）: 21(GP16)
      | 同一ネット全端子　　; U1: 12(DOUT)
      |                     ; U7: 21(GP16)
      | 接続部品数　　　　　; 2部品（部品番号で集計。同一ネット全体）
      | 接続端子数　　　　　; 2端子（423端子の部品対応表で集計。ラベル・境界ポートの重複は含めない）
      | この場所の端子数　　; 1端子／1部品（同名ラベルによる接続を除く）
      | 同階層同名ラベル数　; 2個（このラベル自身を含む）
      | 全階層の接続ラベル　; 2個（実際に同じノードへつながるラベル。名前が違う別名も含む）
      | 接続ルール　　　　　; 同じ階層の同じラベル名を仮想配線として結ぶ。別のSubsystem内とは名前だけでつながらず、明示的なConnection Portと配線をたどる。色は用途の表示であり接続を決めない。
      | 確認の範囲　　　　　; 現在の保存回路の端子・配線から求めた静的接続。抵抗やICの内部を導線として短絡せずに集計した。説明の更新は動作シミュレーション、タイミング、実部品の性能・実機動作を保証するものではない。
      | 記録の基準　　　　　; measurement_label_layout_20261022_r01/after_layout_graph.json。部品対応表は端子名の対応付けにのみ使用。
      | 
      | 【この説明欄の略語・記号】
      | 用語1　　　　　　　 ; ADC：Analog-to-Digital Converter（アナログ・デジタル変換器）。測定電圧をデジタル値へ変換する回路。電流や温度も、センサーで電圧へ変換した後に読み取る。
      | 用語2　　　　　　　 ; IC：Integrated Circuit（集積回路）。複数の電子素子と機能を小さな半導体チップに集積した部品。
      | 用語3　　　　　　　 ; GPIO：General-Purpose Input/Output（汎用入出力端子）。入力・出力や周辺機能に割り当てられる端子。GPの後の数字はRP2040の端子信号番号で、基板上の物理ピン番号とは別。
      | 用語4　　　　　　　 ; SPI：Serial Peripheral Interface（同期式シリアル通信）。クロックとデータ線を使う通信方式。本回路ではRP2040と外付け測定用ADCの通信に使う。
      | 用語5　　　　　　　 ; MISO：Master In, Slave Out（制御側へ入るSPIデータ線）。この回路ではADCのDOUTからRP2040へ測定値が流れる。名称の主従は通信上の役割を表す。
      | 用語6　　　　　　　 ; DOUT：Data Out（データ出力端子）。ADC側から見た変換結果のデジタルデータ出力。
  ReadLabel_U7_SPI_MOSI : ConnectionLabel  Description=|  Label=SPI_MOSI
      | この回路での名前　　; SPI_MOSI
      | 種別　　　　　　　　; ConnectionLabel
      | この回路での役割　　; RP2040基板U7のGP19から、外付けADC U1のDINへ入力チャンネルなどの選択情報を送るSPI信号。
      | この場所の直接接続　; U7（RP2040搭載Pico W／SC0918）: 25(GP19)
      | 直接接続の範囲　　　; このラベルから実際の線・分岐・明示的な境界端子だけを追った接続。同名ラベルによる離れた場所への接続はこの欄に含めない。
      | 同一ネットの主接続　; U7（RP2040搭載Pico W／SC0918）: 25(GP19)
      |                     ; U1（外付けADC／MCP3208-CI/SL）: 11(DIN)
      | 同一ネット全端子　　; U1: 11(DIN)
      |                     ; U7: 25(GP19)
      | 接続部品数　　　　　; 2部品（部品番号で集計。同一ネット全体）
      | 接続端子数　　　　　; 2端子（423端子の部品対応表で集計。ラベル・境界ポートの重複は含めない）
      | この場所の端子数　　; 1端子／1部品（同名ラベルによる接続を除く）
      | 同階層同名ラベル数　; 2個（このラベル自身を含む）
      | 全階層の接続ラベル　; 2個（実際に同じノードへつながるラベル。名前が違う別名も含む）
      | 接続ルール　　　　　; 同じ階層の同じラベル名を仮想配線として結ぶ。別のSubsystem内とは名前だけでつながらず、明示的なConnection Portと配線をたどる。色は用途の表示であり接続を決めない。
      | 確認の範囲　　　　　; 現在の保存回路の端子・配線から求めた静的接続。抵抗やICの内部を導線として短絡せずに集計した。説明の更新は動作シミュレーション、タイミング、実部品の性能・実機動作を保証するものではない。
      | 記録の基準　　　　　; measurement_label_layout_20261022_r01/after_layout_graph.json。部品対応表は端子名の対応付けにのみ使用。
      | 
      | 【この説明欄の略語・記号】
      | 用語1　　　　　　　 ; ADC：Analog-to-Digital Converter（アナログ・デジタル変換器）。測定電圧をデジタル値へ変換する回路。電流や温度も、センサーで電圧へ変換した後に読み取る。
      | 用語2　　　　　　　 ; IC：Integrated Circuit（集積回路）。複数の電子素子と機能を小さな半導体チップに集積した部品。
      | 用語3　　　　　　　 ; GPIO：General-Purpose Input/Output（汎用入出力端子）。入力・出力や周辺機能に割り当てられる端子。GPの後の数字はRP2040の端子信号番号で、基板上の物理ピン番号とは別。
      | 用語4　　　　　　　 ; SPI：Serial Peripheral Interface（同期式シリアル通信）。クロックとデータ線を使う通信方式。本回路ではRP2040と外付け測定用ADCの通信に使う。
      | 用語5　　　　　　　 ; MOSI：Master Out, Slave In（制御側から出るSPIデータ線）。この回路ではRP2040からADCのDINへ測定チャネル選択などの情報が流れる。
      | 用語6　　　　　　　 ; DIN：Data In（データ入力端子）。ADC側から見たデジタルデータ入力。測定対象のアナログ電圧入力とは別。
  ReadLabel_U7_SPI_SCK : ConnectionLabel  Description=|  Label=SPI_SCK
      | この回路での名前　　; SPI_SCK
      | 種別　　　　　　　　; ConnectionLabel
      | この回路での役割　　; RP2040基板U7のGP18から、外付けADC U1のCLKへ通信のタイミングを渡すSPIクロック線。
      | この場所の直接接続　; U7（RP2040搭載Pico W／SC0918）: 24(GP18)
      | 直接接続の範囲　　　; このラベルから実際の線・分岐・明示的な境界端子だけを追った接続。同名ラベルによる離れた場所への接続はこの欄に含めない。
      | 同一ネットの主接続　; U7（RP2040搭載Pico W／SC0918）: 24(GP18)
      |                     ; U1（外付けADC／MCP3208-CI/SL）: 13(CLK)
      | 同一ネット全端子　　; U1: 13(CLK)
      |                     ; U7: 24(GP18)
      | 接続部品数　　　　　; 2部品（部品番号で集計。同一ネット全体）
      | 接続端子数　　　　　; 2端子（423端子の部品対応表で集計。ラベル・境界ポートの重複は含めない）
      | この場所の端子数　　; 1端子／1部品（同名ラベルによる接続を除く）
      | 同階層同名ラベル数　; 2個（このラベル自身を含む）
      | 全階層の接続ラベル　; 2個（実際に同じノードへつながるラベル。名前が違う別名も含む）
      | 接続ルール　　　　　; 同じ階層の同じラベル名を仮想配線として結ぶ。別のSubsystem内とは名前だけでつながらず、明示的なConnection Portと配線をたどる。色は用途の表示であり接続を決めない。
      | 確認の範囲　　　　　; 現在の保存回路の端子・配線から求めた静的接続。抵抗やICの内部を導線として短絡せずに集計した。説明の更新は動作シミュレーション、タイミング、実部品の性能・実機動作を保証するものではない。
      | 記録の基準　　　　　; measurement_label_layout_20261022_r01/after_layout_graph.json。部品対応表は端子名の対応付けにのみ使用。
      | 
      | 【この説明欄の略語・記号】
      | 用語1　　　　　　　 ; ADC：Analog-to-Digital Converter（アナログ・デジタル変換器）。測定電圧をデジタル値へ変換する回路。電流や温度も、センサーで電圧へ変換した後に読み取る。
      | 用語2　　　　　　　 ; IC：Integrated Circuit（集積回路）。複数の電子素子と機能を小さな半導体チップに集積した部品。
      | 用語3　　　　　　　 ; GPIO：General-Purpose Input/Output（汎用入出力端子）。入力・出力や周辺機能に割り当てられる端子。GPの後の数字はRP2040の端子信号番号で、基板上の物理ピン番号とは別。
      | 用語4　　　　　　　 ; SPI：Serial Peripheral Interface（同期式シリアル通信）。クロックとデータ線を使う通信方式。本回路ではRP2040と外付け測定用ADCの通信に使う。
      | 用語5　　　　　　　 ; SCK：Serial Clock（シリアル通信クロック）。SPIのデータを送り受けするタイミングを定める信号。
      | 用語6　　　　　　　 ; CLK：Clock（クロック端子）。データ転送などの動作タイミングを定める端子。
  ReadLabel_U7_V3V3 : ConnectionLabel  Description=|  Label=V3V3
      | この回路での名前　　; V3V3
      | 種別　　　　　　　　; ConnectionLabel
      | この回路での役割　　; RP2040基板U7の3.3V出力から、ADC・電流検出IC・温度センサー・基準電圧ICなどへ電源を分配する。信号のプルアップ抵抗にも供給する。
      | この場所の直接接続　; U7（RP2040搭載Pico W／SC0918）: 36(3V3_OUT)
      | 直接接続の範囲　　　; このラベルから実際の線・分岐・明示的な境界端子だけを追った接続。同名ラベルによる離れた場所への接続はこの欄に含めない。
      | 同一ネットの主接続　; U7（RP2040搭載Pico W／SC0918）: 36(3V3_OUT)
      |                     ; U1（外付けADC／MCP3208-CI/SL）: 16(VDD)
      |                     ; U2（PV入力電流の検出アンプ／INA241A3IDDFR）: 6(VS)
      |                     ; U3（L1直後の出力電流の検出アンプ／INA241A3IDDFR）: 6(VS)
      |                     ; U4（電池温度センサー／TMP235A2DBZR）: 1(VDD)
      |                     ; U5（放熱器温度センサー／TMP235A2DBZR）: 1(VDD)
      |                     ; U6（2.5Vの測定基準電圧源／REF3025EAIDBZR）: 1(IN)
      |                     ; R49（U10のオープンドレインPG信号BIAS_PGをPicoの3V3へ引き上げ、GP9で読める電圧にする／10k 1%）: 2
      |                     ; P_RFLT_PU（LTC4364のオープンドレインFLTをMCUの3.3 V系へ引き上げる／22 kΩ）: 1
      | 同一ネット全端子　　; C17: 1
      |                     ; C18: 1
      |                     ; C22: 1
      |                     ; C24: 1
      |                     ; C26: 1
      |                     ; C28: 1
      |                     ; C30: 1
      |                     ; P_RFLT_PU: 1
      |                     ; R15: 1
      |                     ; R49: 2
      |                     ; U1: 16(VDD)
      |                     ; U2: 6(VS)
      |                     ; U3: 6(VS)
      |                     ; U4: 1(VDD)
      |                     ; U5: 1(VDD)
      |                     ; U6: 1(IN)
      |                     ; U7: 36(3V3_OUT)
      | 接続部品数　　　　　; 17部品（部品番号で集計。同一ネット全体）
      | 接続端子数　　　　　; 17端子（423端子の部品対応表で集計。ラベル・境界ポートの重複は含めない）
      | この場所の端子数　　; 1端子／1部品（同名ラベルによる接続を除く）
      | 同階層同名ラベル数　; 10個（このラベル自身を含む）
      | 全階層の接続ラベル　; 10個（実際に同じノードへつながるラベル。名前が違う別名も含む）
      | 接続ルール　　　　　; 同じ階層の同じラベル名を仮想配線として結ぶ。別のSubsystem内とは名前だけでつながらず、明示的なConnection Portと配線をたどる。色は用途の表示であり接続を決めない。
      | 確認の範囲　　　　　; 現在の保存回路の端子・配線から求めた静的接続。抵抗やICの内部を導線として短絡せずに集計した。説明の更新は動作シミュレーション、タイミング、実部品の性能・実機動作を保証するものではない。
      | 記録の基準　　　　　; measurement_label_layout_20261022_r01/after_layout_graph.json。部品対応表は端子名の対応付けにのみ使用。
      | 
      | 【この説明欄の略語・記号】
      | 用語1　　　　　　　 ; ADC：Analog-to-Digital Converter（アナログ・デジタル変換器）。測定電圧をデジタル値へ変換する回路。電流や温度も、センサーで電圧へ変換した後に読み取る。
      | 用語2　　　　　　　 ; IC：Integrated Circuit（集積回路）。複数の電子素子と機能を小さな半導体チップに集積した部品。
      | 用語3　　　　　　　 ; MCU：Microcontroller Unit（マイクロコントローラ）。プログラムを実行し、測定値の処理や出力制御を担当する小型計算機。
      | 用語4　　　　　　　 ; GPIO：General-Purpose Input/Output（汎用入出力端子）。入力・出力や周辺機能に割り当てられる端子。GPの後の数字はRP2040の端子信号番号で、基板上の物理ピン番号とは別。
      | 用語5　　　　　　　 ; MOSFET：Metal-Oxide-Semiconductor Field-Effect Transistor（金属・酸化膜・半導体構造の電界効果トランジスタ）。ゲートとソースの電圧でドレインとソースの導通を制御する素子。N-MOSはNチャネル型を表す。
      | 用語6　　　　　　　 ; PV：Photovoltaic（太陽光発電）。光を電気へ変える発電方式。PVを含むネット名は太陽電池側の測定・電力経路を表す。
      | 用語7　　　　　　　 ; GND：Ground（回路の基準電位・電流帰路）。この図の共通基準。保護接地や大地への接続を意味するとは限らない。
      | 用語8　　　　　　　 ; PG：Power Good（電源状態通知）。電源出力が規定状態にあるかを知らせる信号。プルアップ条件と実際の通知条件は対象ICの説明で確認する。
      | 用語9　　　　　　　 ; FLT：Fault（故障状態通知）。LTC4364の故障警告出力。全種類の異常や逆流を一律に通知する信号という意味ではない。
      | 用語10　　　　　　　; VCC/VDD/VEE/VS：ICの電源端子名。文字の歴史的な由来を現在の接続機能へ当てはめない。現回路のVEEはU8/U10では浮動基準SW、U9ではGND。各電圧・基準は端子と接続を参照する。
      | 用語11　　　　　　　; SW：Switching Node（スイッチング点）。主電力段の上下MOSFETとL1がつながる、電圧が高速に切り替わる点。GNDとは別電位。
  ReadLabel_U7_VSYS_5V : ConnectionLabel  Description=|  Label=VSYS_5V
      | この回路での名前　　; VSYS_5V
      | 種別　　　　　　　　; ConnectionLabel
      | この回路での役割　　; ダイオードD3の出力を、RP2040基板U7のVSYS電源入力へ渡す。P5からはD3を介して供給されるため、P5とは別ノード。
      | この場所の直接接続　; U7（RP2040搭載Pico W／SC0918）: 39(VSYS)
      | 直接接続の範囲　　　; このラベルから実際の線・分岐・明示的な境界端子だけを追った接続。同名ラベルによる離れた場所への接続はこの欄に含めない。
      | 同一ネットの主接続　; D3（DIODE／40V 1A Schottky VSYS OR）: 1(K)
      |                     ; U7（RP2040搭載Pico W／SC0918）: 39(VSYS)
      | 同一ネット全端子　　; D3: 1(K)
      |                     ; U7: 39(VSYS)
      | 接続部品数　　　　　; 2部品（部品番号で集計。同一ネット全体）
      | 接続端子数　　　　　; 2端子（423端子の部品対応表で集計。ラベル・境界ポートの重複は含めない）
      | この場所の端子数　　; 1端子／1部品（同名ラベルによる接続を除く）
      | 同階層同名ラベル数　; 2個（このラベル自身を含む）
      | 全階層の接続ラベル　; 2個（実際に同じノードへつながるラベル。名前が違う別名も含む）
      | 接続ルール　　　　　; 同じ階層の同じラベル名を仮想配線として結ぶ。別のSubsystem内とは名前だけでつながらず、明示的なConnection Portと配線をたどる。色は用途の表示であり接続を決めない。
      | 確認の範囲　　　　　; 現在の保存回路の端子・配線から求めた静的接続。抵抗やICの内部を導線として短絡せずに集計した。説明の更新は動作シミュレーション、タイミング、実部品の性能・実機動作を保証するものではない。
      | 記録の基準　　　　　; measurement_label_layout_20261022_r01/after_layout_graph.json。部品対応表は端子名の対応付けにのみ使用。
      | 
      | 【この説明欄の略語・記号】
      | 用語1　　　　　　　 ; IC：Integrated Circuit（集積回路）。複数の電子素子と機能を小さな半導体チップに集積した部品。
  ReadLabel_U8_H12 : ConnectionLabel  Description=|  Label=H12
      | この回路での名前　　; H12
      | 種別　　　　　　　　; ConnectionLabel
      | この回路での役割　　; 絶縁電源U10の二次側出力を、高側ゲートドライバU8と二次側コンデンサへ供給する。電圧の基準はSWであり、共通GND基準の12V電源P12とは別。
      | この場所の直接接続　; C32（光ゲートドライバ局所バイパス／1uF 50V X7R）: 1
      |                     ; U8（高側の光ゲートドライバ／ACPL-P346-560E）: 6(VCC)
      | 直接接続の範囲　　　; このラベルから実際の線・分岐・明示的な境界端子だけを追った接続。同名ラベルによる離れた場所への接続はこの欄に含めない。
      | 同一ネットの主接続　; U10（高側ゲート用の浮動電源を作る絶縁DC/DC／UCC14131QDWNRQ1）: 28(VDD), 29(VDD)
      |                     ; U8（高側の光ゲートドライバ／ACPL-P346-560E）: 6(VCC)
      |                     ; C32（光ゲートドライバ局所バイパス／1uF 50V X7R）: 1
      |                     ; C37（絶縁DC/DC二次側バルク／22uF 25V X7R）: 1
      |                     ; C38（絶縁DC/DC二次側HFバイパス／100nF 50V X7R）: 1
      |                     ; R45（H12からH_FBへ接続し、R46とともにU10の出力電圧帰還を構成する／38.3k 1%）: 1
      |                     ; R47（H_RLIMとH12を0 Ωで接続し、U10のRLIM端子の既存設定を実装する／0 ohm）: 2
      | 同一ネット全端子　　; C32: 1
      |                     ; C37: 1
      |                     ; C38: 1
      |                     ; R45: 1
      |                     ; R47: 2
      |                     ; U8: 6(VCC)
      |                     ; U10: 28(VDD), 29(VDD)
      | 接続部品数　　　　　; 7部品（部品番号で集計。同一ネット全体）
      | 接続端子数　　　　　; 8端子（423端子の部品対応表で集計。ラベル・境界ポートの重複は含めない）
      | この場所の端子数　　; 2端子／2部品（同名ラベルによる接続を除く）
      | 同階層同名ラベル数　; 3個（このラベル自身を含む）
      | 全階層の接続ラベル　; 3個（実際に同じノードへつながるラベル。名前が違う別名も含む）
      | 接続ルール　　　　　; 同じ階層の同じラベル名を仮想配線として結ぶ。別のSubsystem内とは名前だけでつながらず、明示的なConnection Portと配線をたどる。色は用途の表示であり接続を決めない。
      | 確認の範囲　　　　　; 現在の保存回路の端子・配線から求めた静的接続。抵抗やICの内部を導線として短絡せずに集計した。説明の更新は動作シミュレーション、タイミング、実部品の性能・実機動作を保証するものではない。
      | 記録の基準　　　　　; measurement_label_layout_20261022_r01/after_layout_graph.json。部品対応表は端子名の対応付けにのみ使用。
      | 
      | 【この説明欄の略語・記号】
      | 用語1　　　　　　　 ; DC：Direct Current（直流）。ここでは直流電源または直流成分。DCバイアスはコンデンサに重なる直流電圧を指す。
      | 用語2　　　　　　　 ; DC/DC：DC-to-DC Converter（直流電圧変換器）。直流入力を別の直流電圧へ変換する電源回路。絶縁の有無は個々の部品説明で確認する。
      | 用語3　　　　　　　 ; HF：High Frequency（高周波）。速い電圧・電流変化に対応する成分。具体的な周波数帯は対象回路ごとに説明する。
      | 用語4　　　　　　　 ; X7R：セラミックコンデンサの温度特性記号。英語の頭文字ではなく分類コード。X＝下限−55 ℃、7＝上限+125 ℃、R＝その範囲の容量変化±15%。直流バイアスによる容量変化は別に確認する。
      | 用語5　　　　　　　 ; IC：Integrated Circuit（集積回路）。複数の電子素子と機能を小さな半導体チップに集積した部品。
      | 用語6　　　　　　　 ; MOSFET：Metal-Oxide-Semiconductor Field-Effect Transistor（金属・酸化膜・半導体構造の電界効果トランジスタ）。ゲートとソースの電圧でドレインとソースの導通を制御する素子。N-MOSはNチャネル型を表す。
      | 用語7　　　　　　　 ; GND：Ground（回路の基準電位・電流帰路）。この図の共通基準。保護接地や大地への接続を意味するとは限らない。
      | 用語8　　　　　　　 ; FB：Feedback（帰還）。出力などを検出して内部制御へ戻すための信号・端子。
      | 用語9　　　　　　　 ; VCC/VDD/VEE/VS：ICの電源端子名。文字の歴史的な由来を現在の接続機能へ当てはめない。現回路のVEEはU8/U10では浮動基準SW、U9ではGND。各電圧・基準は端子と接続を参照する。
      | 用語10　　　　　　　; RLIM：U10の外付け抵抗による制限設定端子。外付けR47で二次側の電圧調整に使う電流を制限する端子。主電力段の充電電流制限とは別の機能。
      | 用語11　　　　　　　; SW：Switching Node（スイッチング点）。主電力段の上下MOSFETとL1がつながる、電圧が高速に切り替わる点。GNDとは別電位。
  ReadLabel_U9_P12 : ConnectionLabel  Description=|  Label=P12
      | この回路での名前　　; P12
      | 種別　　　　　　　　; ConnectionLabel
      | この回路での役割　　; 12V電源モジュールU11の出力を、低側ゲートドライバU9、絶縁電源U10の一次側、5V電源モジュールU12へ分配する。
      | この場所の直接接続　; C33（光ゲートドライバ局所バイパス／1uF 50V X7R）: 1
      |                     ; U9（低側の光ゲートドライバ／ACPL-P346-560E）: 6(VCC)
      | 直接接続の範囲　　　; このラベルから実際の線・分岐・明示的な境界端子だけを追った接続。同名ラベルによる離れた場所への接続はこの欄に含めない。
      | 同一ネットの主接続　; U11（バッテリー補助分岐から12Vを作る電源モジュール／TSR 1-48120WI）: 3(+VOUT)
      |                     ; U9（低側の光ゲートドライバ／ACPL-P346-560E）: 6(VCC)
      |                     ; U10（高側ゲート用の浮動電源を作る絶縁DC/DC／UCC14131QDWNRQ1）: 6(VIN), 7(VIN)
      |                     ; U12（12Vから5Vを作る電源モジュール／TSR 1-2450）: 1(+VIN)
      |                     ; C45（12Vレギュレータ出力局所バイパス／22uF 25V X7R）: 1
      |                     ; C46（共通12Vバルク/過渡蓄積／470uF 25V hybrid）: 1
      |                     ; C47（5Vレギュレータ入力局所バイパス／1uF 50V X7R）: 1
      | 同一ネット全端子　　; C33: 1
      |                     ; C34: 1
      |                     ; C35: 1
      |                     ; C36: 1
      |                     ; C45: 1
      |                     ; C46: 1
      |                     ; C47: 1
      |                     ; U9: 6(VCC)
      |                     ; U10: 6(VIN), 7(VIN)
      |                     ; U11: 3(+VOUT)
      |                     ; U12: 1(+VIN)
      | 接続部品数　　　　　; 11部品（部品番号で集計。同一ネット全体）
      | 接続端子数　　　　　; 12端子（423端子の部品対応表で集計。ラベル・境界ポートの重複は含めない）
      | この場所の端子数　　; 2端子／2部品（同名ラベルによる接続を除く）
      | 同階層同名ラベル数　; 4個（このラベル自身を含む）
      | 全階層の接続ラベル　; 4個（実際に同じノードへつながるラベル。名前が違う別名も含む）
      | 接続ルール　　　　　; 同じ階層の同じラベル名を仮想配線として結ぶ。別のSubsystem内とは名前だけでつながらず、明示的なConnection Portと配線をたどる。色は用途の表示であり接続を決めない。
      | 確認の範囲　　　　　; 現在の保存回路の端子・配線から求めた静的接続。抵抗やICの内部を導線として短絡せずに集計した。説明の更新は動作シミュレーション、タイミング、実部品の性能・実機動作を保証するものではない。
      | 記録の基準　　　　　; measurement_label_layout_20261022_r01/after_layout_graph.json。部品対応表は端子名の対応付けにのみ使用。
      | 
      | 【この説明欄の略語・記号】
      | 用語1　　　　　　　 ; DC：Direct Current（直流）。ここでは直流電源または直流成分。DCバイアスはコンデンサに重なる直流電圧を指す。
      | 用語2　　　　　　　 ; DC/DC：DC-to-DC Converter（直流電圧変換器）。直流入力を別の直流電圧へ変換する電源回路。絶縁の有無は個々の部品説明で確認する。
      | 用語3　　　　　　　 ; X7R：セラミックコンデンサの温度特性記号。英語の頭文字ではなく分類コード。X＝下限−55 ℃、7＝上限+125 ℃、R＝その範囲の容量変化±15%。直流バイアスによる容量変化は別に確認する。
      | 用語4　　　　　　　 ; IC：Integrated Circuit（集積回路）。複数の電子素子と機能を小さな半導体チップに集積した部品。
      | 用語5　　　　　　　 ; MOSFET：Metal-Oxide-Semiconductor Field-Effect Transistor（金属・酸化膜・半導体構造の電界効果トランジスタ）。ゲートとソースの電圧でドレインとソースの導通を制御する素子。N-MOSはNチャネル型を表す。
      | 用語6　　　　　　　 ; GND：Ground（回路の基準電位・電流帰路）。この図の共通基準。保護接地や大地への接続を意味するとは限らない。
      | 用語7　　　　　　　 ; VIN/VOUT：入力電圧・出力電圧を表す端子／ネット名。INは入力、OUTは出力。電源変換器の電力端子なのか、検出用端子なのかは対象部品によって異なるため、端子と接続の説明に従う。
      | 用語8　　　　　　　 ; VCC/VDD/VEE/VS：ICの電源端子名。文字の歴史的な由来を現在の接続機能へ当てはめない。現回路のVEEはU8/U10では浮動基準SW、U9ではGND。各電圧・基準は端子と接続を参照する。
      | 用語9　　　　　　　 ; SW：Switching Node（スイッチング点）。主電力段の上下MOSFETとL1がつながる、電圧が高速に切り替わる点。GNDとは別電位。
  U1 : Subsystem  Description=|  mask(太陽光充電回路 編集用部品){PartRef=U1, PartMPN=MCP3208-CI/SL, PartValue=MCP3208-CI/SL, DesignValue=MCP3208-CI/SL, SourceRef=FI_MEAS_ADC/U_ADC}
      | この回路での名前　　; U1
      | 部品名　　　　　　　; MCP3208-CI/SL
      | この回路での役割　　; 電圧・電流・温度の測定信号を、マイコンU7が計算に使える数値へ変える測定用IC。
      | ここでの動き　　　　; 太陽電池の電圧と電流、充電器出力電圧、充電電流、電池温度、放熱器温度、電池側電圧の8信号（追加CH7は保護前のパネル電圧）を接続する。マイコンU7の指示で対象の信号を選び、数値へ変換して返す。各入力は前段で読み取れる電圧に整えられている。
      | 
      | 【詳しい働き・仕様・接続・確認の範囲】
      | 部品種別　　　　　　; 8チャネルADC
      | 公称値　　　　　　　; MCP3208-CI/SL
      | 配置目的　　　　　　; PV電圧・PV電流・出力電圧・充電電流・電池温度・放熱器温度・電池電圧を読み、SPIでU7へ渡す。
      | 意図する動作　　　　; CH0〜CH7を測定に使用し、CH7はパネル側保護より上流の電圧。各入力のRC、基準電圧、取得時間、SPI設定は変換精度と応答を左右する。
      | 端子と接続　　　　　; 1 CH0 → ADC_VPV、2 CH1 → ADC_IPV、3 CH2 → ADC_VOUT、4 CH3 → ADC_IL、5 CH4 → ADC_TBAT、6 CH5 → ADC_TSINK、7 CH6 → ADC_VBAT、8 CH7 → ADC_VPV_INPUT、9 DGND → GND、10 CS_N → SPI_CS_N、11 DIN → SPI_MOSI、12 DOUT → SPI_MISO、13 CLK → SPI_SCK、14 AGND → GND、15 VREF → VREF2V5_ADC、16 VDD → 3V3
      | モデルの範囲　　　　; 端子配置・接続確認用の図面ブロック。内部はConnection Portによる端子表現であり、このブロック単体は対象IC/モジュールの電気的機能やソフトウェアを再現しない。
      | 確認の範囲　　　　　; 本説明は保存回路の部品情報・端子割当・既存設計意図を整理したもの。今回の説明更新によって新たな動作試験や実機検証を実施した意味ではない。
      | 設計記録　　　　　　; evaluation\component_annotations_20261022_r01\before_graph.json
      | evaluation\component_annotations_20261022_r01\before_metadata.json
      | evaluation\protection_capacitor_integration_20261021_r01\final_delivery\independent_readback\physical_bom.json
      | 
      | 【この説明欄の略語・記号】
      | 用語1　　　　　　　 ; ADC：Analog-to-Digital Converter（アナログ・デジタル変換器）。測定電圧をデジタル値へ変換する回路。電流や温度も、センサーで電圧へ変換した後に読み取る。
      | 用語2　　　　　　　 ; IC：Integrated Circuit（集積回路）。複数の電子素子と機能を小さな半導体チップに集積した部品。
      | 用語3　　　　　　　 ; SPI：Serial Peripheral Interface（同期式シリアル通信）。クロックとデータ線を使う通信方式。本回路ではRP2040と外付け測定用ADCの通信に使う。
      | 用語4　　　　　　　 ; MISO：Master In, Slave Out（制御側へ入るSPIデータ線）。この回路ではADCのDOUTからRP2040へ測定値が流れる。名称の主従は通信上の役割を表す。
      | 用語5　　　　　　　 ; MOSI：Master Out, Slave In（制御側から出るSPIデータ線）。この回路ではRP2040からADCのDINへ測定チャネル選択などの情報が流れる。
      | 用語6　　　　　　　 ; SCK：Serial Clock（シリアル通信クロック）。SPIのデータを送り受けするタイミングを定める信号。
      | 用語7　　　　　　　 ; CS_N：Chip Select（チップ選択信号）。末尾Nはこの設計でLow有効を表す。Lowにして通信対象のADCを選択する。
      | 用語8　　　　　　　 ; DIN：Data In（データ入力端子）。ADC側から見たデジタルデータ入力。測定対象のアナログ電圧入力とは別。
      | 用語9　　　　　　　 ; DOUT：Data Out（データ出力端子）。ADC側から見た変換結果のデジタルデータ出力。
      | 用語10　　　　　　　; CLK：Clock（クロック端子）。データ転送などの動作タイミングを定める端子。
      | 用語11　　　　　　　; CH：Channel（測定チャネル）。CH0〜CH7はADCの入力番号であり、同時測定を意味しない。
      | 用語12　　　　　　　; MOSFET：Metal-Oxide-Semiconductor Field-Effect Transistor（金属・酸化膜・半導体構造の電界効果トランジスタ）。ゲートとソースの電圧でドレインとソースの導通を制御する素子。N-MOSはNチャネル型を表す。
      | 用語13　　　　　　　; PV：Photovoltaic（太陽光発電）。光を電気へ変える発電方式。PVを含むネット名は太陽電池側の測定・電力経路を表す。
      | 用語14　　　　　　　; RC：Resistor-Capacitor（抵抗とコンデンサの組合せ）。主に測定信号のフィルタや時定数を作る。カットオフ周波数は実際の接続と抵抗・容量から求める。
      | 用語15　　　　　　　; GND：Ground（回路の基準電位・電流帰路）。この図の共通基準。保護接地や大地への接続を意味するとは限らない。
      | 用語16　　　　　　　; AGND：Analog Ground（アナログ回路の基準端子）。アナログ部分の電流帰路。現図では共通GNDへ接続されるが、実装時の電流経路への配慮は別途必要。
      | 用語17　　　　　　　; DGND：Digital Ground（デジタル回路の基準端子）。デジタル部分の電流帰路。現図では共通GNDへ接続される。
      | 用語18　　　　　　　; VIN/VOUT：入力電圧・出力電圧を表す端子／ネット名。INは入力、OUTは出力。電源変換器の電力端子なのか、検出用端子なのかは対象部品によって異なるため、端子と接続の説明に従う。
      | 用語19　　　　　　　; VREF/REF：基準電圧を表す端子名。REFはReference（基準）の意味。ADCの変換尺度や電流アンプの出力基準に使う。REF1/REF2の接続電位は個別に確認する。
      | 用語20　　　　　　　; VCC/VDD/VEE/VS：ICの電源端子名。文字の歴史的な由来を現在の接続機能へ当てはめない。現回路のVEEはU8/U10では浮動基準SW、U9ではGND。各電圧・基準は端子と接続を参照する。
      | 用語21　　　　　　　; SW：Switching Node（スイッチング点）。主電力段の上下MOSFETとL1がつながる、電圧が高速に切り替わる点。GNDとは別電位。
      | 
      | 
      | 【実物に対応する端子配置】
      | 表示の向き　　　　　; TOP VIEW / 1番端子が左上
      | 対象パッケージ　　　; SOIC-16
      | 番号の意味　　　　　; 図内の番号は実部品の端子番号。GPIO名やSimulink内部のポート番号とは区別する。未使用の端子にもメーカーの機能名を表示する。
      | 表示の範囲　　　　　; 端子の相対的な並びを示す。部品の寸法・縮尺や基板フットプリントを保証する図ではない。
      | メーカー根拠　　　　; https://ww1.microchip.com/downloads/en/DeviceDoc/21298e.pdf
      | 
      | 【c06のCH7追加】
      | CH7（物理8番）は保護前PV_FUSEDを75kΩ+75kΩと3.3kΩで分圧したADC_VPV_INPUTを読む。以前のGND接続は除去。CH0は従来どおり保護後VINを読む。100nFをADC近傍へ置き、再許可判定は十分に整定した値と誤差余裕を使う。ADC取得時間・チャネル切替誤差・無電源時流入は別検証範囲。
      mask prompts: PartRef "物理部品番号"; PartMPN "部品型番"; PartValue "部品値・表示値"; DesignValue "元設計値（記録）"; SourceRef "旧参照名（記録）"
      mask help: 回路図編集用です。端子・配線は実際のSimscape接続ですが、部品内部の動作式は未実装です。値・型番を変更し、配線をドラッグして編集できます。
      settings: AttributesFormatString=MCP3208 ADC
      mask Display:
      | color('black');
      | plot([0.005 0.995 0.995 0.005 0.005],[0.005 0.005 0.995 0.995 0.005]);
      | text(0.5,0.94,'U1','horizontalAlignment','center','texmode','off');
      | text(0.5,0.86,'TOP VIEW','horizontalAlignment','center','texmode','off');
      | plot([0.10 0.12 0.14 0.12 0.10],[0.97 0.99 0.97 0.95 0.97]);
      | port_label('lconn',1,'1 CH0');
      | port_label('lconn',2,'2 CH1');
      | port_label('lconn',3,'3 CH2');
      | port_label('lconn',4,'4 CH3');
      | port_label('lconn',5,'5 CH4');
      | port_label('lconn',6,'6 CH5');
      | port_label('lconn',7,'7 CH6');
      | port_label('lconn',8,'8 CH7');
      | port_label('rconn',1,'16 VDD');
      | port_label('rconn',2,'15 VREF');
      | port_label('rconn',3,'14 AGND');
      | port_label('rconn',4,'13 CLK');
      | port_label('rconn',5,'12 DOUT');
      | port_label('rconn',6,'11 DIN');
      | port_label('rconn',7,'10 CS_N');
      | port_label('rconn',8,'9 DGND');
  U10 : Subsystem  Description=|  mask(太陽光充電回路 編集用部品){PartRef=U10, PartMPN=UCC14131QDWNRQ1, PartValue=UCC14131QDWNRQ1, DesignValue=single floating 12.075V bias, SourceRef=ti_ucc}
      | この回路での名前　　; U10
      | 部品名　　　　　　　; UCC14131QDWNRQ1
      | この回路での役割　　; 上側ゲートドライバU8用の約12 V電源を作る部品。入力と出力を電気的に絶縁するトランスを内蔵した電源モジュール。
      | ここでの動き　　　　; 入力側は共通GNDを基準にした12 Vを受け取り、出力側は上側MOSFET Q1のソースSWより約12.075 V高い電源H12を作る設計設定。SWが上下しても、U8に供給するH12とSWの電圧差を約12 Vに保つことを狙う。
      | 
      | 【詳しい働き・仕様・接続・確認の範囲】
      | 詳しい役割　　　　　; 上側ゲートドライバU8用の約12 V電源を作る部品。入力と出力を電気的に絶縁するトランスを内蔵した、絶縁DC/DC電源モジュール。
      | なぜ必要か　　　　　; 上側MOSFET Q1のソースはSWにつながり、スイッチングに伴って電圧が上下する。Q1を駆動するU8にも、このSWを基準とする電源が必要なため、U10を置いている。
      | 入力する電源　　　　; P12と共通GNDの間の約12 Vから電力を受け取る。U10の入力側GNDPは、主電力段と同じ共通GNDへ接続する。
      | 作る電源　　　　　　; 出力のプラス側はH12、マイナス側はSW。H12がSWより約12.075 V高くなる設計設定。共通GNDから測ったH12が、いつも12 Vになるという意味ではない。
      | 電圧のイメージ　　　; たとえばSWが共通GNDに対して50 Vのとき、H12は約62.1 Vになる考え方。SWが上下しても、U8に供給するH12とSWの間は約12 Vを保つことを狙う。この数値例は原理の説明で、測定結果ではない。
      | 基準電位の区別　　　; 入力側GNDPは共通GND。出力側VEE/VEEAはSW。出力側は「静かなGND」ではなく、SWと一緒に高速で電圧が動く基準であり、共通GNDとは直接つながない。
      | 帰還配線への配慮　　; 出力電圧を測るVEEAは、出力側の電力電流の影響を受けにくく配線するための検出用基準。メーカーはVEEへの一点接続を指定している。図面で同じSWネットであることと、基板上で雑音を拾いにくく配線できていることは別であり、後者はこの図だけでは確認できない。
      | 電圧を決める部品　　; R45=38.3 kΩ、R46=10 kΩで、2.5 V × (1 + 38.3/10) = 12.075 Vに設定する。これは抵抗の公称値による目標値で、誤差を含む実際の出力電圧を保証する値ではない。C39は帰還検出の高周波雑音を抑えるための部品。
      | 基準端子が多い理由　; GNDPは14端子、VEEは12端子あり、電流の帰り道と基板への放熱に使う。GNDPの1・2・5番はアナログ基準、8～18番は電力帰路。VEEAの35番は別に設けた帰還検出用基準。余った機能端子をGNDへ落としているわけではない。
      | ほかの使われ方　　　; モータ用インバータ、車載充電器、太陽光用インバータなどでも、ゲートドライバの補助電源として使う。外付け回路の設定により単一出力や正負を含む二出力にもできる。現回路では約12 Vの単一出力を使う。
      | 
      | 【マイコンからの操作と状態確認】
      | 名前の意味　　　　　; BIASは英単語Bias（バイアス）で、この図ではゲート駆動用の補助電源を指す。EN = Enable（動作許可）、PG = Power Good（電源状態通知）。ラベルは部品ではなく、同じ階層の同名ノードとの接続を示す。
      | BIAS_EN　　　　　　 ; U7のGP8とU10のENA（4番）は同じノード。Highで絶縁電源の動作を許可し、Lowで停止を指示する。R48はそのノードからGNDへの10 kΩプルダウンで、マイコン端子が駆動されない間のLow側の状態を作る。
      | BIAS_PG　　　　　　 ; U10のPG（3番）からU7のGP9へ状態を返す。U10の正常成立時は内部出力がLowへ引き込み、正常不成立・停止時は出力を解放する。R49は解放時のノードを3.3 Vへ引き上げる10 kΩプルアップ。GP9は入力として読む。Highが正常という意味ではない。
      | 確認範囲　　　　　　; 接続とメーカー仕様に基づく説明。今回、MicroPythonの制御プログラムや起動動作試験を変更・実行した意味ではない。
      | メーカー根拠　　　　; https://www.ti.com/lit/gpn/ucc14131-q1（UCC14131-Q1データシート、端子表と11.3.3）
      | 
      | 【端子一覧・モデルの範囲・記録】
      | 端子と接続　　　　　; 1 GNDP → GND、2 GNDP → GND、3 PG → BIAS_PG、4 ENA → BIAS_EN、5 GNDP → GND、6 VIN → P12、7 VIN → P12、8 GNDP → GND、9 GNDP → GND、10 GNDP → GND、11 GNDP → GND、12 GNDP → GND、13 GNDP → GND、14 GNDP → GND、15 GNDP → GND、16 GNDP → GND、17 GNDP → GND、18 GNDP → GND、19 VEE → SW、20 VEE → SW、21 VEE → SW、22 VEE → SW、23 VEE → SW、24 VEE → SW、25 VEE → SW、26 VEE → SW、27 VEE → SW、28 VDD → H12、29 VDD → H12、30 VEE → SW、31 VEE → SW、32 RLIM → H_RLIM、33 FBVEE → H_FB、34 FBVDD → H_FB、35 VEEA → SW、36 VEE → SW
      | モデルの範囲　　　　; 端子配置・接続確認用の図面ブロック。内部はConnection Portによる端子表現であり、このブロック単体は対象IC/モジュールの電気的機能やソフトウェアを再現しない。
      | 確認の範囲　　　　　; 本説明は保存回路の部品情報・端子割当・既存設計意図を整理したもの。今回の説明更新によって新たな動作試験や実機検証を実施した意味ではない。
      | 設計記録　　　　　　; evaluation\component_annotations_20261022_r01\before_graph.json
      | evaluation\component_annotations_20261022_r01\before_metadata.json
      | evaluation\protection_capacitor_integration_20261021_r01\final_delivery\independent_readback\physical_bom.json
      | 
      | 【この説明欄の略語・記号】
      | 用語1　　　　　　　 ; DC：Direct Current（直流）。ここでは直流電源または直流成分。DCバイアスはコンデンサに重なる直流電圧を指す。
      | 用語2　　　　　　　 ; DC/DC：DC-to-DC Converter（直流電圧変換器）。直流入力を別の直流電圧へ変換する電源回路。絶縁の有無は個々の部品説明で確認する。
      | 用語3　　　　　　　 ; IC：Integrated Circuit（集積回路）。複数の電子素子と機能を小さな半導体チップに集積した部品。
      | 用語4　　　　　　　 ; GPIO：General-Purpose Input/Output（汎用入出力端子）。入力・出力や周辺機能に割り当てられる端子。GPの後の数字はRP2040の端子信号番号で、基板上の物理ピン番号とは別。
      | 用語5　　　　　　　 ; MOSFET：Metal-Oxide-Semiconductor Field-Effect Transistor（金属・酸化膜・半導体構造の電界効果トランジスタ）。ゲートとソースの電圧でドレインとソースの導通を制御する素子。N-MOSはNチャネル型を表す。
      | 用語6　　　　　　　 ; GND：Ground（回路の基準電位・電流帰路）。この図の共通基準。保護接地や大地への接続を意味するとは限らない。
      | 用語7　　　　　　　 ; PG：Power Good（電源状態通知）。電源出力が規定状態にあるかを知らせる信号。プルアップ条件と実際の通知条件は対象ICの説明で確認する。
      | 用語8　　　　　　　 ; FB：Feedback（帰還）。出力などを検出して内部制御へ戻すための信号・端子。
      | 用語9　　　　　　　 ; EN：Enable（動作許可）。対象機能の動作を許可する信号。端子ごとの有効レベルや接続状態に従う。
      | 用語10　　　　　　　; VIN/VOUT：入力電圧・出力電圧を表す端子／ネット名。INは入力、OUTは出力。電源変換器の電力端子なのか、検出用端子なのかは対象部品によって異なるため、端子と接続の説明に従う。
      | 用語11　　　　　　　; VCC/VDD/VEE/VS：ICの電源端子名。文字の歴史的な由来を現在の接続機能へ当てはめない。現回路のVEEはU8/U10では浮動基準SW、U9ではGND。各電圧・基準は端子と接続を参照する。
      | 用語12　　　　　　　; GNDP：U10の一次側電源の基準端子。絶縁電源の入力側GND。二次側基準VEE=SWと直接同一の導体ではない。
      | 用語13　　　　　　　; VEEA：U10の二次側アナログ基準端子。現回路ではSWへ接続する。共通GNDへ接続する意味ではない。
      | 用語14　　　　　　　; FBVDD/FBVEE：U10の出力電圧帰還端子。二次側の出力電圧設定に用いる。現接続では両端子がH_FBへ接続される。
      | 用語15　　　　　　　; RLIM：U10の外付け抵抗による制限設定端子。外付けR47で二次側の電圧調整に使う電流を制限する端子。主電力段の充電電流制限とは別の機能。
      | 用語16　　　　　　　; SW：Switching Node（スイッチング点）。主電力段の上下MOSFETとL1がつながる、電圧が高速に切り替わる点。GNDとは別電位。
      | 
      | 
      | 【実物に対応する端子配置】
      | 表示の向き　　　　　; TOP VIEW / 1番端子が左上
      | 対象パッケージ　　　; SSOP-36 (DWN)
      | 番号の意味　　　　　; 図内の番号は実部品の端子番号。GPIO名やSimulink内部のポート番号とは区別する。未使用の端子にもメーカーの機能名を表示する。
      | 表示の範囲　　　　　; 端子の相対的な並びを示す。部品の寸法・縮尺や基板フットプリントを保証する図ではない。
      | メーカー根拠　　　　; https://www.ti.com/lit/gpn/ucc14131-q1
      mask prompts: PartRef "物理部品番号"; PartMPN "部品型番"; PartValue "部品値・表示値"; DesignValue "元設計値（記録）"; SourceRef "旧参照名（記録）"
      mask help: 回路図編集用です。端子・配線は実際のSimscape接続ですが、部品内部の動作式は未実装です。値・型番を変更し、配線をドラッグして編集できます。
      settings: AttributesFormatString=UCC14131 絶縁電源
      mask Display:
      | color('black');
      | plot([0.005 0.995 0.995 0.005 0.005],[0.005 0.005 0.995 0.995 0.005]);
      | text(0.5,0.94,'U10','horizontalAlignment','center','texmode','off');
      | text(0.5,0.86,'TOP VIEW','horizontalAlignment','center','texmode','off');
      | plot([0.10 0.12 0.14 0.12 0.10],[0.97 0.99 0.97 0.95 0.97]);
      | port_label('lconn',1,'1 GNDP');
      | port_label('lconn',2,'2 GNDP');
      | port_label('lconn',3,'3 PG');
      | port_label('lconn',4,'4 ENA');
      | port_label('lconn',5,'5 GNDP');
      | port_label('lconn',6,'6 VIN');
      | port_label('lconn',7,'7 VIN');
      | port_label('lconn',8,'8 GNDP');
      | port_label('lconn',9,'9 GNDP');
      | port_label('lconn',10,'10 GNDP');
      | port_label('lconn',11,'11 GNDP');
      | port_label('lconn',12,'12 GNDP');
      | port_label('lconn',13,'13 GNDP');
      | port_label('lconn',14,'14 GNDP');
      | port_label('lconn',15,'15 GNDP');
      | port_label('lconn',16,'16 GNDP');
      | port_label('lconn',17,'17 GNDP');
      | port_label('lconn',18,'18 GNDP');
      | port_label('rconn',1,'36 VEE');
      | port_label('rconn',2,'35 VEEA');
      | port_label('rconn',3,'34 FBVDD');
      | port_label('rconn',4,'33 FBVEE');
      | port_label('rconn',5,'32 RLIM');
      | port_label('rconn',6,'31 VEE');
      | port_label('rconn',7,'30 VEE');
      | port_label('rconn',8,'29 VDD');
      | port_label('rconn',9,'28 VDD');
      | port_label('rconn',10,'27 VEE');
      | port_label('rconn',11,'26 VEE');
      | port_label('rconn',12,'25 VEE');
      | port_label('rconn',13,'24 VEE');
      | port_label('rconn',14,'23 VEE');
      | port_label('rconn',15,'22 VEE');
      | port_label('rconn',16,'21 VEE');
      | port_label('rconn',17,'20 VEE');
      | port_label('rconn',18,'19 VEE');
  U11 : Subsystem  Description=|  mask(太陽光充電回路 編集用部品){PartRef=U11, PartMPN=TSR 1-48120WI, PartValue=TSR 1-48120WI, DesignValue=battery to 12V 1A, SourceRef=traco_tsr1wi}
      | この回路での名前　　; U11
      | 部品名　　　　　　　; TSR 1-48120WI
      | この回路での役割　　; ゲート駆動回路や、ほかの補助電源に使う12 Vを電池から作る電源モジュール。
      | ここでの動き　　　　; 電池の補助電源用分岐から受けた電圧を12 Vへ下げ、下側ゲートドライバU9、上側用絶縁電源U10、5 V電源U12へ供給する。入力と出力は共通GNDを使う。
      | 
      | 【詳しい働き・仕様・接続・確認の範囲】
      | 部品種別　　　　　　; 12 V降圧電源モジュール
      | 公称値　　　　　　　; battery to 12V 1A
      | 配置目的　　　　　　; 電池の補助分岐BAT_AUXからP12を作り、ゲート駆動電源・U10・U12へ供給する。
      | 意図する動作　　　　; 非絶縁の補助電源。入力側C40〜C44、出力側C45と共通バルクC46を使用。個数・容量が最小構成と確定したわけではない。
      | 端子と接続　　　　　; 1 +VIN → BAT_AUX、2 GND → GND、3 +VOUT → P12、4 CASE → 未接続、5 CASE → 未接続
      | モデルの範囲　　　　; 端子配置・接続確認用の図面ブロック。内部はConnection Portによる端子表現であり、このブロック単体は対象IC/モジュールの電気的機能やソフトウェアを再現しない。
      | 確認の範囲　　　　　; 本説明は保存回路の部品情報・端子割当・既存設計意図を整理したもの。今回の説明更新によって新たな動作試験や実機検証を実施した意味ではない。
      | 設計記録　　　　　　; evaluation\component_annotations_20261022_r01\before_graph.json
      | evaluation\component_annotations_20261022_r01\before_metadata.json
      | evaluation\protection_capacitor_integration_20261021_r01\final_delivery\independent_readback\physical_bom.json
      | 
      | 【この説明欄の略語・記号】
      | 用語1　　　　　　　 ; IC：Integrated Circuit（集積回路）。複数の電子素子と機能を小さな半導体チップに集積した部品。
      | 用語2　　　　　　　 ; GND：Ground（回路の基準電位・電流帰路）。この図の共通基準。保護接地や大地への接続を意味するとは限らない。
      | 用語3　　　　　　　 ; VIN/VOUT：入力電圧・出力電圧を表す端子／ネット名。INは入力、OUTは出力。電源変換器の電力端子なのか、検出用端子なのかは対象部品によって異なるため、端子と接続の説明に従う。
      | 
      | 
      | 【実物に対応する端子配置】
      | 表示の向き　　　　　; 正面・印字面 / ピンが下
      | 対象パッケージ　　　; SIP / Straight pin
      | 番号の意味　　　　　; 図内の番号は実部品の端子番号。GPIO名やSimulink内部のポート番号とは区別する。未使用の端子にもメーカーの機能名を表示する。
      | 表示の範囲　　　　　; 端子の相対的な並びを示す。部品の寸法・縮尺や基板フットプリントを保証する図ではない。
      | 特殊な表示　　　　　; SIP（Single In-line Package：端子が一列のパッケージ）として印字面を正面に見る。U11の4/5はケース端子で、現回路では未接続を保つ。
      | メーカー根拠　　　　; https://www.tracopower.com/tsr1wi-datasheet
      mask prompts: PartRef "物理部品番号"; PartMPN "部品型番"; PartValue "部品値・表示値"; DesignValue "元設計値（記録）"; SourceRef "旧参照名（記録）"
      mask help: 回路図編集用です。端子・配線は実際のSimscape接続ですが、部品内部の動作式は未実装です。値・型番を変更し、配線をドラッグして編集できます。
      settings: AttributesFormatString=TSR1 12 V電源
      mask Display:
      | color('black');
      | plot([0.005 0.995 0.995 0.005 0.005],[0.005 0.005 0.995 0.995 0.005]);
      | text(0.5,0.8,'U11','horizontalAlignment','center','texmode','off');
      | text(0.5,0.6,'FRONT / MARKING','horizontalAlignment','center','texmode','off');
      | text(0.5,0.4,'TSR 1-48120WI','horizontalAlignment','center','texmode','off');
      | port_label('lconn',1,'4 CASE');
      | port_label('lconn',2,'1 +VIN');
      | port_label('lconn',3,'2 GND');
      | port_label('lconn',4,'3 +VOUT');
      | port_label('lconn',5,'5 CASE');
  U12 : Subsystem  Description=|  mask(太陽光充電回路 編集用部品){PartRef=U12, PartMPN=TSR 1-2450, PartValue=TSR 1-2450, DesignValue=12V to 5V 1A, SourceRef=traco_tsr1}
      | この回路での名前　　; U12
      | 部品名　　　　　　　; TSR 1-2450
      | この回路での役割　　; マイコン基板とゲートドライバの入力側に使う5 Vを作る電源モジュール。
      | ここでの動き　　　　; U11の12 Vを5 Vへ下げ、U8/U9内部の発光素子を駆動する回路と、ダイオードD3を通したマイコン基板U7の電源へ供給する。
      | 
      | 【詳しい働き・仕様・接続・確認の範囲】
      | 部品種別　　　　　　; 5 V降圧電源モジュール
      | 公称値　　　　　　　; 12V to 5V 1A
      | 配置目的　　　　　　; P12からP5を作り、ゲートドライバ入力LEDとD3を介したPico電源へ供給する。
      | 意図する動作　　　　; C47はU12入力、C48はU12出力用。P12に並ぶだけでC47をU11専用出力コンデンサと解釈しない。
      | 端子と接続　　　　　; 1 +VIN → P12、2 GND → GND、3 +VOUT → P5
      | モデルの範囲　　　　; 端子配置・接続確認用の図面ブロック。内部はConnection Portによる端子表現であり、このブロック単体は対象IC/モジュールの電気的機能やソフトウェアを再現しない。
      | 確認の範囲　　　　　; 本説明は保存回路の部品情報・端子割当・既存設計意図を整理したもの。今回の説明更新によって新たな動作試験や実機検証を実施した意味ではない。
      | 設計記録　　　　　　; evaluation\component_annotations_20261022_r01\before_graph.json
      | evaluation\component_annotations_20261022_r01\before_metadata.json
      | evaluation\protection_capacitor_integration_20261021_r01\final_delivery\independent_readback\physical_bom.json
      | 
      | 【この説明欄の略語・記号】
      | 用語1　　　　　　　 ; IC：Integrated Circuit（集積回路）。複数の電子素子と機能を小さな半導体チップに集積した部品。
      | 用語2　　　　　　　 ; LED：Light-Emitting Diode（発光ダイオード）。本回路のゲートドライバ入力では光によって信号を伝え、入力側と出力側を絶縁するために用いる。
      | 用語3　　　　　　　 ; GND：Ground（回路の基準電位・電流帰路）。この図の共通基準。保護接地や大地への接続を意味するとは限らない。
      | 用語4　　　　　　　 ; VIN/VOUT：入力電圧・出力電圧を表す端子／ネット名。INは入力、OUTは出力。電源変換器の電力端子なのか、検出用端子なのかは対象部品によって異なるため、端子と接続の説明に従う。
      | 
      | 
      | 【実物に対応する端子配置】
      | 表示の向き　　　　　; 正面・印字面 / ピンが下
      | 対象パッケージ　　　; SIP-3
      | 番号の意味　　　　　; 図内の番号は実部品の端子番号。GPIO名やSimulink内部のポート番号とは区別する。未使用の端子にもメーカーの機能名を表示する。
      | 表示の範囲　　　　　; 端子の相対的な並びを示す。部品の寸法・縮尺や基板フットプリントを保証する図ではない。
      | 特殊な表示　　　　　; SIP（Single In-line Package：端子が一列のパッケージ）として印字面を正面に見る。
      | メーカー根拠　　　　; https://www.tracopower.com/tsr1-datasheet
      mask prompts: PartRef "物理部品番号"; PartMPN "部品型番"; PartValue "部品値・表示値"; DesignValue "元設計値（記録）"; SourceRef "旧参照名（記録）"
      mask help: 回路図編集用です。端子・配線は実際のSimscape接続ですが、部品内部の動作式は未実装です。値・型番を変更し、配線をドラッグして編集できます。
      settings: AttributesFormatString=TSR1 5 V電源
      mask Display:
      | color('black');
      | plot([0.005 0.995 0.995 0.005 0.005],[0.005 0.005 0.995 0.995 0.005]);
      | text(0.5,0.8,'U12','horizontalAlignment','center','texmode','off');
      | text(0.5,0.6,'FRONT / MARKING','horizontalAlignment','center','texmode','off');
      | text(0.5,0.4,'TSR 1-2450','horizontalAlignment','center','texmode','off');
      | port_label('lconn',1,'1 +VIN');
      | port_label('lconn',2,'2 GND');
      | port_label('lconn',3,'3 +VOUT');
  U3 : Subsystem  Description=|  mask(太陽光充電回路 編集用部品){PartRef=U3, PartMPN=INA241A3IDDFR, PartValue=INA241A3IDDFR, DesignValue=INA241A3 (50 V/V), SourceRef=FI_PROTECTION/U_ISENSE_CHG}
      | この回路での名前　　; U3
      | 部品名　　　　　　　; INA241A3IDDFR
      | この回路での役割　　; 主インダクタL1を通った充電側の電流を測るための増幅IC。
      | ここでの動き　　　　; 電流検出用抵抗R2の両端の小さな電圧差を増幅し、測定用IC U1へ渡す。太陽電池側を測るU2とは測定場所が異なる。
      | 
      | 【詳しい働き・仕様・接続・確認の範囲】
      | 部品種別　　　　　　; 充電電流検出アンプ
      | 公称値　　　　　　　; INA241A3 (50 V/V)
      | 配置目的　　　　　　; R2のKelvin端子間の微小電圧差を増幅してIL_OUTへ出す。
      | 意図する動作　　　　; PV入力電流とは別位置のL1後の電流を測る。REF1=VREF2V5_ADC、REF2=GND。逆方向電流の数値測定と高速遮断は同一の機能ではない。
      | 端子と接続　　　　　; 1 IN- → IL_SENSE_M、2 GND → GND、3 REF2 → GND、4 RESERVED_GND → GND、5 OUT → IL_OUT、6 VS → 3V3、7 REF1 → VREF2V5_ADC、8 IN+ → IL_SENSE_P
      | モデルの範囲　　　　; 端子配置・接続確認用の図面ブロック。内部はConnection Portによる端子表現であり、このブロック単体は対象IC/モジュールの電気的機能やソフトウェアを再現しない。
      | 確認の範囲　　　　　; 本説明は保存回路の部品情報・端子割当・既存設計意図を整理したもの。今回の説明更新によって新たな動作試験や実機検証を実施した意味ではない。
      | 設計記録　　　　　　; evaluation\component_annotations_20261022_r01\before_graph.json
      | evaluation\component_annotations_20261022_r01\before_metadata.json
      | evaluation\protection_capacitor_integration_20261021_r01\final_delivery\independent_readback\physical_bom.json
      | 
      | 【この説明欄の略語・記号】
      | 用語1　　　　　　　 ; ADC：Analog-to-Digital Converter（アナログ・デジタル変換器）。測定電圧をデジタル値へ変換する回路。電流や温度も、センサーで電圧へ変換した後に読み取る。
      | 用語2　　　　　　　 ; IC：Integrated Circuit（集積回路）。複数の電子素子と機能を小さな半導体チップに集積した部品。
      | 用語3　　　　　　　 ; MOSFET：Metal-Oxide-Semiconductor Field-Effect Transistor（金属・酸化膜・半導体構造の電界効果トランジスタ）。ゲートとソースの電圧でドレインとソースの導通を制御する素子。N-MOSはNチャネル型を表す。
      | 用語4　　　　　　　 ; PV：Photovoltaic（太陽光発電）。光を電気へ変える発電方式。PVを含むネット名は太陽電池側の測定・電力経路を表す。
      | 用語5　　　　　　　 ; GND：Ground（回路の基準電位・電流帰路）。この図の共通基準。保護接地や大地への接続を意味するとは限らない。
      | 用語6　　　　　　　 ; VREF/REF：基準電圧を表す端子名。REFはReference（基準）の意味。ADCの変換尺度や電流アンプの出力基準に使う。REF1/REF2の接続電位は個別に確認する。
      | 用語7　　　　　　　 ; VCC/VDD/VEE/VS：ICの電源端子名。文字の歴史的な由来を現在の接続機能へ当てはめない。現回路のVEEはU8/U10では浮動基準SW、U9ではGND。各電圧・基準は端子と接続を参照する。
      | 用語8　　　　　　　 ; SW：Switching Node（スイッチング点）。主電力段の上下MOSFETとL1がつながる、電圧が高速に切り替わる点。GNDとは別電位。
      | 用語9　　　　　　　 ; IN+/IN−：差動測定の正側・負側入力。電流検出アンプは両端子の電圧差を読む。IN−は必ずGNDという意味ではない。
      | 
      | 
      | 【実物に対応する端子配置】
      | 表示の向き　　　　　; TOP VIEW / 1番端子が左上
      | 対象パッケージ　　　; DDF-8
      | 番号の意味　　　　　; 図内の番号は実部品の端子番号。GPIO名やSimulink内部のポート番号とは区別する。未使用の端子にもメーカーの機能名を表示する。
      | 表示の範囲　　　　　; 端子の相対的な並びを示す。部品の寸法・縮尺や基板フットプリントを保証する図ではない。
      | メーカー根拠　　　　; https://www.ti.com/lit/gpn/ina241a
      mask prompts: PartRef "物理部品番号"; PartMPN "部品型番"; PartValue "部品値・表示値"; DesignValue "元設計値（記録）"; SourceRef "旧参照名（記録）"
      mask help: 回路図編集用です。端子・配線は実際のSimscape接続ですが、部品内部の動作式は未実装です。値・型番を変更し、配線をドラッグして編集できます。
      settings: AttributesFormatString=INA241 充電電流
      mask Display:
      | color('black');
      | plot([0.005 0.995 0.995 0.005 0.005],[0.005 0.005 0.995 0.995 0.005]);
      | text(0.5,0.94,'U3','horizontalAlignment','center','texmode','off');
      | text(0.5,0.86,'TOP VIEW','horizontalAlignment','center','texmode','off');
      | plot([0.10 0.12 0.14 0.12 0.10],[0.97 0.99 0.97 0.95 0.97]);
      | port_label('lconn',1,'1 IN-');
      | port_label('lconn',2,'2 GND');
      | port_label('lconn',3,'3 REF2');
      | port_label('lconn',4,'4 RESERVED_GND');
      | port_label('rconn',1,'8 IN+');
      | port_label('rconn',2,'7 REF1');
      | port_label('rconn',3,'6 VS');
      | port_label('rconn',4,'5 OUT');
  U4 : Subsystem  Description=|  mask(太陽光充電回路 編集用部品){PartRef=U4, PartMPN=TMP235A2DBZR, PartValue=TMP235A2DBZR, DesignValue=TMP235A2DBZR, SourceRef=FI_MEAS_FRONTEND/U_TBAT}
      | この回路での名前　　; U4
      | 部品名　　　　　　　; TMP235A2DBZR
      | この回路での役割　　; 電池付近の温度をマイコンへ知らせるための温度センサー。
      | ここでの動き　　　　; センサー自身の温度に応じた電圧を出し、測定用IC U1で数値へ変換する。電池内部の温度を直接測っているという意味ではない。
      | 
      | 【詳しい働き・仕様・接続・確認の範囲】
      | 部品種別　　　　　　; 電池側アナログ温度センサー
      | 公称値　　　　　　　; TMP235A2DBZR
      | 配置目的　　　　　　; 電池付近の温度をアナログ電圧TBAT_OUTへ変換しU1へ渡す。
      | 意図する動作　　　　; 測定する温度はセンサー実装位置の温度であり、電池内部温度そのものの保証ではない。取り付け・熱遅れを別途確認する。
      | 端子と接続　　　　　; 1 VDD → 3V3、2 OUT → TBAT_OUT、3 GND → GND
      | モデルの範囲　　　　; 端子配置・接続確認用の図面ブロック。内部はConnection Portによる端子表現であり、このブロック単体は対象IC/モジュールの電気的機能やソフトウェアを再現しない。
      | 確認の範囲　　　　　; 本説明は保存回路の部品情報・端子割当・既存設計意図を整理したもの。今回の説明更新によって新たな動作試験や実機検証を実施した意味ではない。
      | 設計記録　　　　　　; evaluation\component_annotations_20261022_r01\before_graph.json
      | evaluation\component_annotations_20261022_r01\before_metadata.json
      | evaluation\protection_capacitor_integration_20261021_r01\final_delivery\independent_readback\physical_bom.json
      | 
      | 【この説明欄の略語・記号】
      | 用語1　　　　　　　 ; IC：Integrated Circuit（集積回路）。複数の電子素子と機能を小さな半導体チップに集積した部品。
      | 用語2　　　　　　　 ; MOSFET：Metal-Oxide-Semiconductor Field-Effect Transistor（金属・酸化膜・半導体構造の電界効果トランジスタ）。ゲートとソースの電圧でドレインとソースの導通を制御する素子。N-MOSはNチャネル型を表す。
      | 用語3　　　　　　　 ; GND：Ground（回路の基準電位・電流帰路）。この図の共通基準。保護接地や大地への接続を意味するとは限らない。
      | 用語4　　　　　　　 ; VCC/VDD/VEE/VS：ICの電源端子名。文字の歴史的な由来を現在の接続機能へ当てはめない。現回路のVEEはU8/U10では浮動基準SW、U9ではGND。各電圧・基準は端子と接続を参照する。
      | 用語5　　　　　　　 ; SW：Switching Node（スイッチング点）。主電力段の上下MOSFETとL1がつながる、電圧が高速に切り替わる点。GNDとは別電位。
      | 
      | 
      | 【実物に対応する端子配置】
      | 表示の向き　　　　　; TOP VIEW / 1番端子が左上
      | 対象パッケージ　　　; SOT-23-3 (DBZ)
      | 番号の意味　　　　　; 図内の番号は実部品の端子番号。GPIO名やSimulink内部のポート番号とは区別する。未使用の端子にもメーカーの機能名を表示する。
      | 表示の範囲　　　　　; 端子の相対的な並びを示す。部品の寸法・縮尺や基板フットプリントを保証する図ではない。
      | メーカー根拠　　　　; https://www.ti.com/lit/gpn/tmp235
      mask prompts: PartRef "物理部品番号"; PartMPN "部品型番"; PartValue "部品値・表示値"; DesignValue "元設計値（記録）"; SourceRef "旧参照名（記録）"
      mask help: 回路図編集用です。端子・配線は実際のSimscape接続ですが、部品内部の動作式は未実装です。値・型番を変更し、配線をドラッグして編集できます。
      settings: AttributesFormatString=TMP235 電池温度
      mask Display:
      | color('black');
      | plot([0.005 0.995 0.995 0.005 0.005],[0.005 0.005 0.995 0.995 0.005]);
      | text(0.5,0.94,'U4','horizontalAlignment','center','texmode','off');
      | text(0.5,0.86,'TOP VIEW','horizontalAlignment','center','texmode','off');
      | plot([0.10 0.12 0.14 0.12 0.10],[0.97 0.99 0.97 0.95 0.97]);
      | port_label('lconn',1,'1 VDD');
      | port_label('lconn',2,'2 OUT');
      | port_label('rconn',1,'3 GND');
  U5 : Subsystem  Description=|  mask(太陽光充電回路 編集用部品){PartRef=U5, PartMPN=TMP235A2DBZR, PartValue=TMP235A2DBZR, DesignValue=TMP235A2DBZR, SourceRef=FI_MEAS_FRONTEND/U_TSW}
      | この回路での名前　　; U5
      | 部品名　　　　　　　; TMP235A2DBZR
      | この回路での役割　　; 主電力段の放熱器付近の温度をマイコンへ知らせるための温度センサー。
      | ここでの動き　　　　; 設置位置の温度に応じた電圧を出し、測定用IC U1で数値へ変換する。MOSFET内部の温度とは、熱の伝わり方や時間差がある。
      | 
      | 【詳しい働き・仕様・接続・確認の範囲】
      | 部品種別　　　　　　; 放熱器側アナログ温度センサー
      | 公称値　　　　　　　; TMP235A2DBZR
      | 配置目的　　　　　　; 放熱器付近の温度をTSINK_OUTへ変換しU1へ渡す。
      | 意図する動作　　　　; 放熱器温度からMOSFET接合温度へは熱抵抗・熱容量・取り付けの影響がある。
      | 端子と接続　　　　　; 1 VDD → 3V3、2 OUT → TSINK_OUT、3 GND → GND
      | モデルの範囲　　　　; 端子配置・接続確認用の図面ブロック。内部はConnection Portによる端子表現であり、このブロック単体は対象IC/モジュールの電気的機能やソフトウェアを再現しない。
      | 確認の範囲　　　　　; 本説明は保存回路の部品情報・端子割当・既存設計意図を整理したもの。今回の説明更新によって新たな動作試験や実機検証を実施した意味ではない。
      | 設計記録　　　　　　; evaluation\component_annotations_20261022_r01\before_graph.json
      | evaluation\component_annotations_20261022_r01\before_metadata.json
      | evaluation\protection_capacitor_integration_20261021_r01\final_delivery\independent_readback\physical_bom.json
      | 
      | 【この説明欄の略語・記号】
      | 用語1　　　　　　　 ; IC：Integrated Circuit（集積回路）。複数の電子素子と機能を小さな半導体チップに集積した部品。
      | 用語2　　　　　　　 ; MOSFET：Metal-Oxide-Semiconductor Field-Effect Transistor（金属・酸化膜・半導体構造の電界効果トランジスタ）。ゲートとソースの電圧でドレインとソースの導通を制御する素子。N-MOSはNチャネル型を表す。
      | 用語3　　　　　　　 ; GND：Ground（回路の基準電位・電流帰路）。この図の共通基準。保護接地や大地への接続を意味するとは限らない。
      | 用語4　　　　　　　 ; VCC/VDD/VEE/VS：ICの電源端子名。文字の歴史的な由来を現在の接続機能へ当てはめない。現回路のVEEはU8/U10では浮動基準SW、U9ではGND。各電圧・基準は端子と接続を参照する。
      | 用語5　　　　　　　 ; SW：Switching Node（スイッチング点）。主電力段の上下MOSFETとL1がつながる、電圧が高速に切り替わる点。GNDとは別電位。
      | 
      | 
      | 【実物に対応する端子配置】
      | 表示の向き　　　　　; TOP VIEW / 1番端子が左上
      | 対象パッケージ　　　; SOT-23-3 (DBZ)
      | 番号の意味　　　　　; 図内の番号は実部品の端子番号。GPIO名やSimulink内部のポート番号とは区別する。未使用の端子にもメーカーの機能名を表示する。
      | 表示の範囲　　　　　; 端子の相対的な並びを示す。部品の寸法・縮尺や基板フットプリントを保証する図ではない。
      | メーカー根拠　　　　; https://www.ti.com/lit/gpn/tmp235
      mask prompts: PartRef "物理部品番号"; PartMPN "部品型番"; PartValue "部品値・表示値"; DesignValue "元設計値（記録）"; SourceRef "旧参照名（記録）"
      mask help: 回路図編集用です。端子・配線は実際のSimscape接続ですが、部品内部の動作式は未実装です。値・型番を変更し、配線をドラッグして編集できます。
      settings: AttributesFormatString=TMP235 放熱器温度
      mask Display:
      | color('black');
      | plot([0.005 0.995 0.995 0.005 0.005],[0.005 0.005 0.995 0.995 0.005]);
      | text(0.5,0.94,'U5','horizontalAlignment','center','texmode','off');
      | text(0.5,0.86,'TOP VIEW','horizontalAlignment','center','texmode','off');
      | plot([0.10 0.12 0.14 0.12 0.10],[0.97 0.99 0.97 0.95 0.97]);
      | port_label('lconn',1,'1 VDD');
      | port_label('lconn',2,'2 OUT');
      | port_label('rconn',1,'3 GND');
  U6 : Subsystem  Description=|  mask(太陽光充電回路 編集用部品){PartRef=U6, PartMPN=REF3025EAIDBZR, PartValue=REF3025EAIDBZR, DesignValue=REF3025EAIDBZR / 2.5V, SourceRef=}
      | この回路での名前　　; U6
      | 部品名　　　　　　　; REF3025EAIDBZR
      | この回路での役割　　; 電圧・電流の測定に使う、基準となる2.5 Vを作るIC。
      | ここでの動き　　　　; 3.3 V電源から2.5 Vの基準電圧を作り、測定用IC U1と電流検出用IC U2/U3へ供給する。測定値を数値へ変える物差しや、出力の基準点として使う。
      | 
      | 【詳しい働き・仕様・接続・確認の範囲】
      | 部品種別　　　　　　; 2.5 V基準電源IC
      | 公称値　　　　　　　; REF3025EAIDBZR / 2.5V
      | 配置目的　　　　　　; U1のADC基準とU2/U3の基準入力へVREF2V5_ADCを供給する。
      | 意図する動作　　　　; 3V3電源から基準電圧を作る。C30は入力バイパス、R30/C31は出力容量枝。初期誤差・温度ドリフト・負荷応答は測定誤差へ影響する。
      | 端子と接続　　　　　; 1 IN → 3V3、2 OUT → VREF2V5_ADC、3 GND → GND
      | モデルの範囲　　　　; 端子配置・接続確認用の図面ブロック。内部はConnection Portによる端子表現であり、このブロック単体は対象IC/モジュールの電気的機能やソフトウェアを再現しない。
      | 確認の範囲　　　　　; 本説明は保存回路の部品情報・端子割当・既存設計意図を整理したもの。今回の説明更新によって新たな動作試験や実機検証を実施した意味ではない。
      | 設計記録　　　　　　; evaluation\component_annotations_20261022_r01\before_graph.json
      | evaluation\component_annotations_20261022_r01\before_metadata.json
      | evaluation\protection_capacitor_integration_20261021_r01\final_delivery\independent_readback\physical_bom.json
      | 
      | 【この説明欄の略語・記号】
      | 用語1　　　　　　　 ; ADC：Analog-to-Digital Converter（アナログ・デジタル変換器）。測定電圧をデジタル値へ変換する回路。電流や温度も、センサーで電圧へ変換した後に読み取る。
      | 用語2　　　　　　　 ; IC：Integrated Circuit（集積回路）。複数の電子素子と機能を小さな半導体チップに集積した部品。
      | 用語3　　　　　　　 ; GND：Ground（回路の基準電位・電流帰路）。この図の共通基準。保護接地や大地への接続を意味するとは限らない。
      | 
      | 
      | 【実物に対応する端子配置】
      | 表示の向き　　　　　; TOP VIEW / 1番端子が左上
      | 対象パッケージ　　　; SOT-23-3 (DBZ)
      | 番号の意味　　　　　; 図内の番号は実部品の端子番号。GPIO名やSimulink内部のポート番号とは区別する。未使用の端子にもメーカーの機能名を表示する。
      | 表示の範囲　　　　　; 端子の相対的な並びを示す。部品の寸法・縮尺や基板フットプリントを保証する図ではない。
      | メーカー根拠　　　　; https://www.ti.com/lit/gpn/ref3025
      mask prompts: PartRef "物理部品番号"; PartMPN "部品型番"; PartValue "部品値・表示値"; DesignValue "元設計値（記録）"; SourceRef "旧参照名（記録）"
      mask help: 回路図編集用です。端子・配線は実際のSimscape接続ですが、部品内部の動作式は未実装です。値・型番を変更し、配線をドラッグして編集できます。
      settings: AttributesFormatString=REF3025 2.5 V
      mask Display:
      | color('black');
      | plot([0.005 0.995 0.995 0.005 0.005],[0.005 0.005 0.995 0.995 0.005]);
      | text(0.5,0.94,'U6','horizontalAlignment','center','texmode','off');
      | text(0.5,0.86,'TOP VIEW','horizontalAlignment','center','texmode','off');
      | plot([0.10 0.12 0.14 0.12 0.10],[0.97 0.99 0.97 0.95 0.97]);
      | port_label('lconn',1,'1 IN');
      | port_label('lconn',2,'2 OUT');
      | port_label('rconn',1,'3 GND');
  U7 : Subsystem  Description=|  mask(太陽光充電回路 編集用部品){PartRef=U7, PartMPN=SC0918, PartValue=SC0918, DesignValue=Raspberry Pi Pico W (SC0918), SourceRef=MCU/PICO_W}
      | この回路での名前　　; U7
      | 部品名　　　　　　　; SC0918
      | この回路での役割　　; 測定値を読み、太陽光充電の動かし方を決める制御用マイコン基板。
      | ここでの動き　　　　; MicroPythonでの制御を採用し、上下ゲート駆動の信号、補助電源の動作許可、保護回路への許可信号を扱う設計。測定用IC U1から値を読み、電源・保護回路から状態を受け取る。図面上のブロックはプログラムを実行するモデルではない。
      | 
      | 【詳しい働き・仕様・接続・確認の範囲】
      | 部品種別　　　　　　; RP2040搭載Raspberry Pi Pico W
      | 公称値　　　　　　　; Raspberry Pi Pico W (SC0918)
      | 配置目的　　　　　　; SPI経由の測定値を用いて制御判断を行い、上下PWM・絶縁電源イネーブル・保護許可を出力する設計上の制御担当。
      | 意図する動作　　　　; 採用方針はMicroPythonによる制御。GP6/GP7=PWM_H/PWM_L、GP8=BIAS_EN、GP9=BIAS_PG、GP11=MAIN_EN、GP13=PROTECTION_FLT_N、GP16〜GP19=SPI。図面ブロックはMicroPythonやPIOを実行しない。GP11/GP13を含む保護シーケンスと実ファームウェアの統合・一貫試験は、既存資料で未実装／未完了の範囲を残す。
      | 端子と接続　　　　　; 1 GP0 → 未接続、2 GP1 → 未接続、3 GND → GND、4 GP2 → 未接続、5 GP3 → 未接続、6 GP4 → 未接続、7 GP5 → 未接続、8 GND → GND、9 GP6 → PWM_H、10 GP7 → PWM_L、11 GP8 → BIAS_EN、12 GP9 → BIAS_PG、13 GND → GND、14 GP10 → 未接続、15 GP11 → MAIN_EN、16 GP12 → 未接続、17 GP13 → PROTECTION_FLT_N、18 GND → GND、19 GP14 → 未接続、20 GP15 → 未接続、21 GP16 → SPI_MISO、22 GP17 → SPI_CS_N、23 GND → GND、24 GP18 → SPI_SCK、25 GP19 → SPI_MOSI、26 GP20 → 未接続、27 GP21 → 未接続、28 GND → GND、29 GP22 → 未接続、30 RUN → 未接続、31 GP26 → 未接続、32 GP27 → 未接続、33 AGND → GND、34 GP28 → 未接続、35 ADC_VREF → 未接続、36 3V3_OUT → 3V3、37 3V3_EN → 未接続、38 GND → GND、39 VSYS → VSYS_5V、40 VBUS → 未接続、D1 SWCLK → 未接続、D2 SWD_GND → 未接続、D3 SWDIO → 未接続
      | モデルの範囲　　　　; 端子配置・接続確認用の図面ブロック。内部はConnection Portによる端子表現であり、このブロック単体は対象IC/モジュールの電気的機能やソフトウェアを再現しない。
      | 確認の範囲　　　　　; 本説明は保存回路の部品情報・端子割当・既存設計意図を整理したもの。今回の説明更新によって新たな動作試験や実機検証を実施した意味ではない。
      | 設計記録　　　　　　; evaluation\component_annotations_20261022_r01\before_graph.json
      | evaluation\component_annotations_20261022_r01\before_metadata.json
      | evaluation\protection_capacitor_integration_20261021_r01\final_delivery\independent_readback\physical_bom.json
      | 
      | 【この説明欄の略語・記号】
      | 用語1　　　　　　　 ; ADC：Analog-to-Digital Converter（アナログ・デジタル変換器）。測定電圧をデジタル値へ変換する回路。電流や温度も、センサーで電圧へ変換した後に読み取る。
      | 用語2　　　　　　　 ; IC：Integrated Circuit（集積回路）。複数の電子素子と機能を小さな半導体チップに集積した部品。
      | 用語3　　　　　　　 ; PWM：Pulse Width Modulation（パルス幅変調）。周期に対するON時間の割合を変えて、スイッチの平均的な電力伝達を調整する方式。
      | 用語4　　　　　　　 ; PIO：Programmable Input/Output（プログラム可能な入出力回路）。RP2040の専用ハードウェア。短い入出力プログラムを実行して端子信号のタイミングを扱う。
      | 用語5　　　　　　　 ; GPIO：General-Purpose Input/Output（汎用入出力端子）。入力・出力や周辺機能に割り当てられる端子。GPの後の数字はRP2040の端子信号番号で、基板上の物理ピン番号とは別。
      | 用語6　　　　　　　 ; SPI：Serial Peripheral Interface（同期式シリアル通信）。クロックとデータ線を使う通信方式。本回路ではRP2040と外付け測定用ADCの通信に使う。
      | 用語7　　　　　　　 ; MISO：Master In, Slave Out（制御側へ入るSPIデータ線）。この回路ではADCのDOUTからRP2040へ測定値が流れる。名称の主従は通信上の役割を表す。
      | 用語8　　　　　　　 ; MOSI：Master Out, Slave In（制御側から出るSPIデータ線）。この回路ではRP2040からADCのDINへ測定チャネル選択などの情報が流れる。
      | 用語9　　　　　　　 ; SCK：Serial Clock（シリアル通信クロック）。SPIのデータを送り受けするタイミングを定める信号。
      | 用語10　　　　　　　; CS_N：Chip Select（チップ選択信号）。末尾Nはこの設計でLow有効を表す。Lowにして通信対象のADCを選択する。
      | 用語11　　　　　　　; DIN：Data In（データ入力端子）。ADC側から見たデジタルデータ入力。測定対象のアナログ電圧入力とは別。
      | 用語12　　　　　　　; DOUT：Data Out（データ出力端子）。ADC側から見た変換結果のデジタルデータ出力。
      | 用語13　　　　　　　; SWD：Serial Wire Debug（シリアルデバッグ用接続）。SWCLKはデバッグクロック、SWDIOは双方向デバッグデータ、SWD_GNDはその基準。現回路では未接続の端子がある。
      | 用語14　　　　　　　; GND：Ground（回路の基準電位・電流帰路）。この図の共通基準。保護接地や大地への接続を意味するとは限らない。
      | 用語15　　　　　　　; AGND：Analog Ground（アナログ回路の基準端子）。アナログ部分の電流帰路。現図では共通GNDへ接続されるが、実装時の電流経路への配慮は別途必要。
      | 用語16　　　　　　　; PG：Power Good（電源状態通知）。電源出力が規定状態にあるかを知らせる信号。プルアップ条件と実際の通知条件は対象ICの説明で確認する。
      | 用語17　　　　　　　; FLT：Fault（故障状態通知）。LTC4364の故障警告出力。全種類の異常や逆流を一律に通知する信号という意味ではない。
      | 用語18　　　　　　　; EN：Enable（動作許可）。対象機能の動作を許可する信号。端子ごとの有効レベルや接続状態に従う。
      | 用語19　　　　　　　; VREF/REF：基準電圧を表す端子名。REFはReference（基準）の意味。ADCの変換尺度や電流アンプの出力基準に使う。REF1/REF2の接続電位は個別に確認する。
      | 
      | 【補助電源の指令と状態通知】
      | 名前の意味　　　　　; BIASは英単語Bias（バイアス）で、この図ではゲート駆動用の補助電源を指す。EN = Enable（動作許可）、PG = Power Good（電源状態通知）。ラベルは部品ではなく、同じ階層の同名ノードとの接続を示す。
      | BIAS_EN　　　　　　 ; U7のGP8とU10のENA（4番）は同じノード。Highで絶縁電源の動作を許可し、Lowで停止を指示する。R48はそのノードからGNDへの10 kΩプルダウンで、マイコン端子が駆動されない間のLow側の状態を作る。
      | BIAS_PG　　　　　　 ; U10のPG（3番）からU7のGP9へ状態を返す。U10の正常成立時は内部出力がLowへ引き込み、正常不成立・停止時は出力を解放する。R49は解放時のノードを3.3 Vへ引き上げる10 kΩプルアップ。GP9は入力として読む。Highが正常という意味ではない。
      | 確認範囲　　　　　　; 接続とメーカー仕様に基づく説明。今回、MicroPythonの制御プログラムや起動動作試験を変更・実行した意味ではない。
      | メーカー根拠　　　　; https://www.ti.com/lit/gpn/ucc14131-q1（UCC14131-Q1データシート、端子表と11.3.3）
      | 
      | 
      | 【実物に対応する端子配置】
      | 表示の向き　　　　　; Pico Wの部品面。USBコネクタが上。RP2040単体のQFNパッケージではない。
      | 外周ピンの並び　　　; 左側は上から1～20、右側は上から40～21。同じ高さの左右ピンが実物と対応する。
      | 番号の意味　　　　　; 図内の番号はPico W基板の端子番号。GPIO番号やSimulink内部のポート番号とは区別する。未使用のGPIOにも本来の機能名を表示する。
      | 中央のデバッグ端子　; 左右の外周40端子は、USBを上にしたPico W部品面の順番と対応する高さに配置する。基板中央にあるSWD（Serial Wire Debug：シリアルワイヤデバッグ）の3パッドは中央に青で描き、下辺へ引出し線で接続端子を設ける。下辺のD1/D2/D3は回路図での引出し先であり、実基板の外周端子ではない。
      | 表示の範囲　　　　　; ピンの順番と相対的な配置を示す。寸法・縮尺・パッドの機械寸法や基板フットプリントは保証しない。
      | メーカー根拠　　　　; https://datasheets.raspberrypi.com/picow/PicoW-A4-Pinout.pdf
      | 
      | 【c06のPV保護インターフェース】
      | 追加した制御        ; GP10（物理14番）からPV_MCU_RUN、GP12（16番）からPV_MCU_REARMを出す。起動直後はLow。
      | 追加した状態入力    ; GP14（19番）でPV_OC_FAULT_N、GP15（20番）でPV_STOPPEDを読む。末尾NはLow有効。STOPPEDは保持論理の状態で実MOSFET遮断の独立確認ではない。
      | 再許可の条件        ; CH7の上流PV電圧とCH0のVIN電圧を十分に整定後に読み、電源正常・異常原因解消・必要な電圧差を確認してから再許可する。OFF中の電流ゼロだけで復帰しない。
      | 用語                ; MCU：Microcontroller Unit（マイコン）。GPIO：General-Purpose Input/Output（汎用入出力）。CH：Channel（ADCの入力チャネル）。RUN/REARMは保護の許可/再許可であり、Pico W自身のRUN端子とは別。
      mask prompts: PartRef "物理部品番号"; PartMPN "部品型番"; PartValue "部品値・表示値"; DesignValue "元設計値（記録）"; SourceRef "旧参照名（記録）"
      mask help: 回路図編集用です。端子・配線は実際のSimscape接続ですが、部品内部の動作式は未実装です。値・型番を変更し、配線をドラッグして編集できます。
      settings: AttributesFormatString=RP2040 / Pico W  PortSchema="{\"entries\":[{\"content\":{\"sides\":[{\"content\":{\"side\":\"LEFT\",\"connectorIds\":[\"LConn1\",\"LConn2\",\"LConn3\",\"LConn4\",\"LConn5\",\"LConn6\",\"LConn7\",\"LConn8\",\"LConn9\",\"LConn10\",\"LConn11\",\"LConn12\",\"LConn13\",\"LConn14\",\"LConn15\",\"LConn16\",\"LConn17\",\"LConn18\",\"LConn19\",\"LConn20\"]},\"type\":\"ConnectorPlacement.EquallySpacedRectSide\",\"uuid\":\"1ce20663-32b6-4096-8bf4-62cf70693e31\"},{\"content\":{\"side\":\"RIGHT\",\"connectorIds\":[\"RConn1\",\"RConn2\",\"RConn3\",\"RConn4\",\"RConn5\",\"RConn6\",\"RConn7\",\"RConn8\",\"RConn9\",\"RConn10\",\"RConn11\",\"RConn12\",\"RConn13\",\"RConn14\",\"RConn15\",\"RConn16\",\"RConn17\",\"RConn18\",\"RConn19\",\"RConn20\"]},\"type\":\"ConnectorPlacement.EquallySpacedRectSide\",\"uuid\":\"1378d852-2c33-4394-9a15-a73164a9f5bf\"},{\"content\":{\"side\":\"TOP\"},\"type\":\"ConnectorPlacement.EquallySpacedRectSide\",\"uuid\":\"74e5107f-09d6-4a5d-a66b-08e9f47ba0bf\"},{\"content\":{\"side\":\"BOTTOM\",\"connectorIds\":[\"RConn21\",\"RConn22\",\"RConn23\"]},\"type\":\"ConnectorPlacement.EquallySpacedRectSide\",\"uuid\":\"c7c7f5ad-64cf-482b-9736-58cbf5724128\"}]},\"type\":\"ConnectorPlacement.EquallySpacedConnector\",\"uuid\":\"0c38e0bd-d414-45bc-a71d-fd7377b8e653\"}],\"packageUris\":[\"http://schema.mathworks.com/mf0/Connector/R2020b\"],\"version\":\"1.0\"}"
      mask Display:
      | color('black');
      | plot([0.005 0.995 0.995 0.005 0.005],[0.005 0.005 0.995 0.995 0.005]);
      | plot([0.4 0.6 0.6 0.4 0.4],[0.93 0.93 0.995 0.995 0.93]);
      | text(0.5,0.96,'USB','horizontalAlignment','center');
      | text(0.5,0.84,'U7 / TOP VIEW','horizontalAlignment','center','texmode','off');
      | text(0.5,0.69,'RP2040','horizontalAlignment','center');
      | text(0.5,0.62,'Pico W','horizontalAlignment','center');
      | text(0.5,0.44,'SWD pads','horizontalAlignment','center','texmode','off');
      | port_label('lconn',1,'1 GP0');
      | port_label('lconn',2,'2 GP1');
      | port_label('lconn',3,'3 GND');
      | port_label('lconn',4,'4 GP2');
      | port_label('lconn',5,'5 GP3');
      | port_label('lconn',6,'6 GP4');
      | port_label('lconn',7,'7 GP5');
      | port_label('lconn',8,'8 GND');
      | port_label('lconn',9,'9 GP6');
      | port_label('lconn',10,'10 GP7');
      | port_label('lconn',11,'11 GP8');
      | port_label('lconn',12,'12 GP9');
      | port_label('lconn',13,'13 GND');
      | port_label('lconn',14,'14 GP10');
      | port_label('lconn',15,'15 GP11');
      | port_label('lconn',16,'16 GP12');
      | port_label('lconn',17,'17 GP13');
      | port_label('lconn',18,'18 GND');
      | port_label('lconn',19,'19 GP14');
      | port_label('lconn',20,'20 GP15');
      | port_label('rconn',1,'40 VBUS');
      | port_label('rconn',2,'39 VSYS');
      | port_label('rconn',3,'38 GND');
      | port_label('rconn',4,'37 3V3_EN');
      | port_label('rconn',5,'36 3V3_OUT');
      | port_label('rconn',6,'35 ADC_VREF');
      | port_label('rconn',7,'34 GP28');
      | port_label('rconn',8,'33 AGND');
      | port_label('rconn',9,'32 GP27');
      | port_label('rconn',10,'31 GP26');
      | port_label('rconn',11,'30 RUN');
      | port_label('rconn',12,'29 GP22');
      | port_label('rconn',13,'28 GND');
      | port_label('rconn',14,'27 GP21');
      | port_label('rconn',15,'26 GP20');
      | port_label('rconn',16,'25 GP19');
      | port_label('rconn',17,'24 GP18');
      | port_label('rconn',18,'23 GND');
      | port_label('rconn',19,'22 GP17');
      | port_label('rconn',20,'21 GP16');
      | port_label('rconn',21,'D1 SWCLK');
      | color('blue');
      | plot([0.368 0.392 0.392 0.368 0.368],[0.374 0.374 0.386 0.386 0.374]);
      | text(0.38,0.405,'D1','horizontalAlignment','center','texmode','off');
      | plot([0.38 0.38 0.161764706 0.161764706],[0.38 0.18 0.18 0]);
      | color('black');
      | port_label('rconn',22,'D2 SWD_GND');
      | color('blue');
      | plot([0.488 0.512 0.512 0.488 0.488],[0.374 0.374 0.386 0.386 0.374]);
      | text(0.5,0.405,'D2','horizontalAlignment','center','texmode','off');
      | plot([0.5 0.5 0.5 0.5],[0.38 0.18 0.18 0]);
      | color('black');
      | port_label('rconn',23,'D3 SWDIO');
      | color('blue');
      | plot([0.608 0.632 0.632 0.608 0.608],[0.374 0.374 0.386 0.386 0.374]);
      | text(0.62,0.405,'D3','horizontalAlignment','center','texmode','off');
      | plot([0.62 0.62 0.838235294 0.838235294],[0.38 0.18 0.18 0]);
      | color('black');
  U8 : Subsystem  Description=|  mask(太陽光充電回路 編集用部品){PartRef=U8, PartMPN=ACPL-P346-560E, PartValue=ACPL-P346-560E, DesignValue=ACPL-P346 optical gate driver, SourceRef=broadcom_acpl}
      | この回路での名前　　; U8
      | 部品名　　　　　　　; ACPL-P346-560E
      | この回路での役割　　; マイコン側の指令を、上側MOSFET Q1をON/OFFできるゲート駆動へ変える部品。
      | ここでの動き　　　　; 内部の発光素子で指令を絶縁して伝え、U10が作る約12 Vの電源を使ってQ1のゲートを充放電する。出力側の電圧基準はQ1のソースSWで、共通GNDとは異なる。
      | 
      | 【詳しい働き・仕様・接続・確認の範囲】
      | 部品種別　　　　　　; 上側フォトカプラ内蔵ゲートドライバ
      | 公称値　　　　　　　; ACPL-P346 optical gate driver
      | 配置目的　　　　　　; 入力LEDの信号を受け、H12–SW電源からQ1ゲート駆動電流を供給する。
      | 意図する動作　　　　; 入力側はQ3AがLED電流を引き込む。出力側の基準VEEはSW。フォトカプラだけで絶縁電源は作れず、U10が別に必要。
      | 端子と接続　　　　　; 1 ANODE → H_LED_A、2 NC → 未接続、3 CATHODE → H_LED_K、4 VEE → SW、5 VOUT → H_DRV、6 VCC → H12
      | モデルの範囲　　　　; 端子配置・接続確認用の図面ブロック。内部はConnection Portによる端子表現であり、このブロック単体は対象IC/モジュールの電気的機能やソフトウェアを再現しない。
      | 確認の範囲　　　　　; 本説明は保存回路の部品情報・端子割当・既存設計意図を整理したもの。今回の説明更新によって新たな動作試験や実機検証を実施した意味ではない。
      | 設計記録　　　　　　; evaluation\component_annotations_20261022_r01\before_graph.json
      | evaluation\component_annotations_20261022_r01\before_metadata.json
      | evaluation\protection_capacitor_integration_20261021_r01\final_delivery\independent_readback\physical_bom.json
      | 
      | 【この説明欄の略語・記号】
      | 用語1　　　　　　　 ; IC：Integrated Circuit（集積回路）。複数の電子素子と機能を小さな半導体チップに集積した部品。
      | 用語2　　　　　　　 ; MOSFET：Metal-Oxide-Semiconductor Field-Effect Transistor（金属・酸化膜・半導体構造の電界効果トランジスタ）。ゲートとソースの電圧でドレインとソースの導通を制御する素子。N-MOSはNチャネル型を表す。
      | 用語3　　　　　　　 ; LED：Light-Emitting Diode（発光ダイオード）。本回路のゲートドライバ入力では光によって信号を伝え、入力側と出力側を絶縁するために用いる。
      | 用語4　　　　　　　 ; GND：Ground（回路の基準電位・電流帰路）。この図の共通基準。保護接地や大地への接続を意味するとは限らない。
      | 用語5　　　　　　　 ; NC：No Connection（接続しない端子）。メーカー指定の未接続端子。一般の使用していない信号端子と同一に扱わない。
      | 用語6　　　　　　　 ; VIN/VOUT：入力電圧・出力電圧を表す端子／ネット名。INは入力、OUTは出力。電源変換器の電力端子なのか、検出用端子なのかは対象部品によって異なるため、端子と接続の説明に従う。
      | 用語7　　　　　　　 ; VCC/VDD/VEE/VS：ICの電源端子名。文字の歴史的な由来を現在の接続機能へ当てはめない。現回路のVEEはU8/U10では浮動基準SW、U9ではGND。各電圧・基準は端子と接続を参照する。
      | 用語8　　　　　　　 ; SW：Switching Node（スイッチング点）。主電力段の上下MOSFETとL1がつながる、電圧が高速に切り替わる点。GNDとは別電位。
      | 
      | 
      | 【実物に対応する端子配置】
      | 表示の向き　　　　　; TOP VIEW / 1番端子が左上
      | 対象パッケージ　　　; SO-6
      | 番号の意味　　　　　; 図内の番号は実部品の端子番号。GPIO名やSimulink内部のポート番号とは区別する。未使用の端子にもメーカーの機能名を表示する。
      | 表示の範囲　　　　　; 端子の相対的な並びを示す。部品の寸法・縮尺や基板フットプリントを保証する図ではない。
      | メーカー根拠　　　　; https://docs.broadcom.com/doc/AV02-4078EN
      mask prompts: PartRef "物理部品番号"; PartMPN "部品型番"; PartValue "部品値・表示値"; DesignValue "元設計値（記録）"; SourceRef "旧参照名（記録）"
      mask help: 回路図編集用です。端子・配線は実際のSimscape接続ですが、部品内部の動作式は未実装です。値・型番を変更し、配線をドラッグして編集できます。
      settings: AttributesFormatString=ACPL-P346 上側
      mask Display:
      | color('black');
      | plot([0.005 0.995 0.995 0.005 0.005],[0.005 0.005 0.995 0.995 0.005]);
      | text(0.5,0.94,'U8','horizontalAlignment','center','texmode','off');
      | text(0.5,0.86,'TOP VIEW','horizontalAlignment','center','texmode','off');
      | plot([0.10 0.12 0.14 0.12 0.10],[0.97 0.99 0.97 0.95 0.97]);
      | port_label('lconn',1,'1 ANODE');
      | port_label('lconn',2,'2 NC');
      | port_label('lconn',3,'3 CATHODE');
      | port_label('rconn',1,'6 VCC');
      | port_label('rconn',2,'5 VOUT');
      | port_label('rconn',3,'4 VEE');
  U9 : Subsystem  Description=|  mask(太陽光充電回路 編集用部品){PartRef=U9, PartMPN=ACPL-P346-560E, PartValue=ACPL-P346-560E, DesignValue=ACPL-P346 optical gate driver, SourceRef=broadcom_acpl}
      | この回路での名前　　; U9
      | 部品名　　　　　　　; ACPL-P346-560E
      | この回路での役割　　; マイコン側の指令を、下側MOSFET Q2をON/OFFできるゲート駆動へ変える部品。
      | ここでの動き　　　　; 内部の発光素子で指令を絶縁して伝え、12 Vの補助電源を使ってQ2のゲートを充放電する。出力側の電圧基準はQ2のソースと同じ共通GND。
      | 
      | 【詳しい働き・仕様・接続・確認の範囲】
      | 部品種別　　　　　　; 下側フォトカプラ内蔵ゲートドライバ
      | 公称値　　　　　　　; ACPL-P346 optical gate driver
      | 配置目的　　　　　　; 入力LEDの信号を受け、P12–GND電源からQ2ゲート駆動電流を供給する。
      | 意図する動作　　　　; 入力側はQ3BがLED電流を引き込む。出力側の基準VEEはGND。上側U8との遅延差を含めてデッドタイムを評価する。
      | 端子と接続　　　　　; 1 ANODE → L_LED_A、2 NC → 未接続、3 CATHODE → L_LED_K、4 VEE → GND、5 VOUT → L_DRV、6 VCC → P12
      | モデルの範囲　　　　; 端子配置・接続確認用の図面ブロック。内部はConnection Portによる端子表現であり、このブロック単体は対象IC/モジュールの電気的機能やソフトウェアを再現しない。
      | 確認の範囲　　　　　; 本説明は保存回路の部品情報・端子割当・既存設計意図を整理したもの。今回の説明更新によって新たな動作試験や実機検証を実施した意味ではない。
      | 設計記録　　　　　　; evaluation\component_annotations_20261022_r01\before_graph.json
      | evaluation\component_annotations_20261022_r01\before_metadata.json
      | evaluation\protection_capacitor_integration_20261021_r01\final_delivery\independent_readback\physical_bom.json
      | 
      | 【この説明欄の略語・記号】
      | 用語1　　　　　　　 ; IC：Integrated Circuit（集積回路）。複数の電子素子と機能を小さな半導体チップに集積した部品。
      | 用語2　　　　　　　 ; MOSFET：Metal-Oxide-Semiconductor Field-Effect Transistor（金属・酸化膜・半導体構造の電界効果トランジスタ）。ゲートとソースの電圧でドレインとソースの導通を制御する素子。N-MOSはNチャネル型を表す。
      | 用語3　　　　　　　 ; LED：Light-Emitting Diode（発光ダイオード）。本回路のゲートドライバ入力では光によって信号を伝え、入力側と出力側を絶縁するために用いる。
      | 用語4　　　　　　　 ; GND：Ground（回路の基準電位・電流帰路）。この図の共通基準。保護接地や大地への接続を意味するとは限らない。
      | 用語5　　　　　　　 ; NC：No Connection（接続しない端子）。メーカー指定の未接続端子。一般の使用していない信号端子と同一に扱わない。
      | 用語6　　　　　　　 ; VIN/VOUT：入力電圧・出力電圧を表す端子／ネット名。INは入力、OUTは出力。電源変換器の電力端子なのか、検出用端子なのかは対象部品によって異なるため、端子と接続の説明に従う。
      | 用語7　　　　　　　 ; VCC/VDD/VEE/VS：ICの電源端子名。文字の歴史的な由来を現在の接続機能へ当てはめない。現回路のVEEはU8/U10では浮動基準SW、U9ではGND。各電圧・基準は端子と接続を参照する。
      | 用語8　　　　　　　 ; SW：Switching Node（スイッチング点）。主電力段の上下MOSFETとL1がつながる、電圧が高速に切り替わる点。GNDとは別電位。
      | 
      | 
      | 【実物に対応する端子配置】
      | 表示の向き　　　　　; TOP VIEW / 1番端子が左上
      | 対象パッケージ　　　; SO-6
      | 番号の意味　　　　　; 図内の番号は実部品の端子番号。GPIO名やSimulink内部のポート番号とは区別する。未使用の端子にもメーカーの機能名を表示する。
      | 表示の範囲　　　　　; 端子の相対的な並びを示す。部品の寸法・縮尺や基板フットプリントを保証する図ではない。
      | メーカー根拠　　　　; https://docs.broadcom.com/doc/AV02-4078EN
      mask prompts: PartRef "物理部品番号"; PartMPN "部品型番"; PartValue "部品値・表示値"; DesignValue "元設計値（記録）"; SourceRef "旧参照名（記録）"
      mask help: 回路図編集用です。端子・配線は実際のSimscape接続ですが、部品内部の動作式は未実装です。値・型番を変更し、配線をドラッグして編集できます。
      settings: AttributesFormatString=ACPL-P346 下側
      mask Display:
      | color('black');
      | plot([0.005 0.995 0.995 0.005 0.005],[0.005 0.005 0.995 0.995 0.005]);
      | text(0.5,0.94,'U9','horizontalAlignment','center','texmode','off');
      | text(0.5,0.86,'TOP VIEW','horizontalAlignment','center','texmode','off');
      | plot([0.10 0.12 0.14 0.12 0.10],[0.97 0.99 0.97 0.95 0.97]);
      | port_label('lconn',1,'1 ANODE');
      | port_label('lconn',2,'2 NC');
      | port_label('lconn',3,'3 CATHODE');
      | port_label('rconn',1,'6 VCC');
      | port_label('rconn',2,'5 VOUT');
      | port_label('rconn',3,'4 VEE');
  connections:
  Connection Label5/LConn1 -- BT1/LConn1 -- F3/RConn1
  BT1/RConn1 -- GND_Label_001/LConn1
  R4/RConn1 -- C1/LConn1 -- R6/RConn1 -- R8/RConn1 -- R10/RConn1 -- R12/RConn1 -- R14/RConn1
  C1/RConn1 -- GND_Label_002/LConn1
  C9/LConn1 -- C10/LConn1 -- MeasureLabel_R1_VIN/LConn1 -- Q1/RConn1 -- PV_Reverse_Protection/RConn1 -- R1/LConn1 -- C8/LConn1 -- C7/LConn1 -- C4/LConn1 -- C3/LConn1 -- C2/LConn1
  C10/RConn1 -- GND_Label_003/LConn1
  C14/LConn1 -- C13/LConn1 -- CircuitNet_VOUT/LConn1 -- R2/RConn1 -- C15/LConn1 -- C16/LConn1 -- LTC4364_Protection/LConn1
  C13/RConn1 -- GND_Label_006/LConn1
  C14/RConn1 -- GND_Label_007/LConn1
  C15/RConn1 -- GND_Label_008/LConn1
  C16/RConn1 -- GND_Label_009/LConn1
  U1/RConn1 -- C17/LConn1 -- C18/LConn1 -- ReadLabel_U1_V3V3/LConn1
  C17/RConn1 -- GND_Label_010/LConn1
  C18/RConn1 -- GND_Label_011/LConn1
  R18/LConn1 -- MeasureLabel_C19_ADC_VPV/LConn1 -- U1/LConn1 -- C19/LConn1 -- R17/RConn1
  C19/RConn1 -- GND_Label_012/LConn1
  C2/RConn1 -- GND_Label_013/LConn1
  R21/LConn1 -- MeasureLabel_C20_ADC_VOUT/LConn1 -- U1/LConn3 -- C20/LConn1 -- R20/RConn1
  C20/RConn1 -- GND_Label_014/LConn1
  C21/LConn1 -- U1/LConn7 -- MeasureLabel_C21_ADC_VBAT/LConn1 -- R23/RConn1 -- R24/LConn1
  C21/RConn1 -- GND_Label_015/LConn1
  ReadLabel_U3_V3V3/LConn1 -- C24/LConn1 -- U3/RConn3
  C24/RConn1 -- GND_Label_018/LConn1
  MeasureLabel_C25_ADC_IL/LConn1 -- C25/LConn1 -- R26/RConn1
  C25/RConn1 -- GND_Label_019/LConn1
  ReadLabel_U4_V3V3/LConn1 -- C26/LConn1 -- U4/LConn1
  C26/RConn1 -- GND_Label_020/LConn1
  MeasureLabel_C27_ADC_TBAT/LConn1 -- C27/LConn1 -- R28/RConn1
  C27/RConn1 -- GND_Label_021/LConn1
  ReadLabel_U5_V3V3/LConn1 -- C28/LConn1 -- U5/LConn1
  C28/RConn1 -- GND_Label_022/LConn1
  MeasureLabel_C29_ADC_TSINK/LConn1 -- C29/LConn1 -- R29/RConn1
  C29/RConn1 -- GND_Label_023/LConn1
  C3/RConn1 -- GND_Label_024/LConn1
  C30/LConn1 -- ReadLabel_U6_V3V3/LConn1 -- U6/LConn1
  C30/RConn1 -- GND_Label_025/LConn1
  C31/LConn1 -- R30/RConn1
  C31/RConn1 -- GND_Label_026/LConn1
  ReadLabel_U8_H12/LConn1 -- C32/LConn1 -- U8/RConn1
  R37/RConn1 -- C32/RConn1 -- U8/RConn3 -- C39/RConn1 -- U10/RConn1 -- U10/RConn2 -- U10/RConn6 -- U10/RConn7 -- U10/RConn10 -- U10/RConn11 -- U10/RConn12 -- U10/RConn13 -- U10/RConn14 -- U10/RConn15 -- U10/RConn16 -- U10/RConn17 -- U10/RConn18 -- C37/RConn1 -- C38/RConn1 -- R46/RConn1 -- D1/LConn1 -- Q2/RConn1 -- Q1/RConn2 -- R13/LConn1 -- R11/LConn1 -- R9/LConn1 -- R7/LConn1 -- R5/LConn1 -- R3/LConn1 -- L1/LConn1
  C33/LConn1 -- ReadLabel_U9_P12/LConn1 -- U9/RConn1
  C33/RConn1 -- GND_Label_027/LConn1
  ReadLabel_U10_P12/LConn1 -- C34/LConn1 -- C35/LConn1 -- C36/LConn1 -- U10/LConn7 -- U10/LConn6
  C34/RConn1 -- GND_Label_028/LConn1
  C35/RConn1 -- GND_Label_029/LConn1
  C36/RConn1 -- GND_Label_030/LConn1
  C37/LConn1 -- C38/LConn1 -- ReadLabel_U10_H12/LConn1 -- U10/RConn9 -- U10/RConn8
  ReadLabel_U10_H_FB1/LConn1 -- C39/LConn1 -- U10/RConn3 -- U10/RConn4
  C4/RConn1 -- GND_Label_031/LConn1
  C41/LConn1 -- C40/LConn1 -- C42/LConn1 -- C43/LConn1 -- C44/LConn1 -- U11/LConn2 -- ReadLabel_U11_BAT_AUX/LConn1 -- F1/RConn1
  C40/RConn1 -- GND_Label_032/LConn1
  C41/RConn1 -- GND_Label_033/LConn1
  C42/RConn1 -- GND_Label_034/LConn1
  C43/RConn1 -- GND_Label_035/LConn1
  C44/RConn1 -- GND_Label_036/LConn1
  ReadLabel_U11_P12/LConn1 -- C46/LConn1 -- C45/LConn1 -- U11/LConn4
  C45/RConn1 -- GND_Label_037/LConn1
  C46/RConn1 -- GND_Label_038/LConn1
  ReadLabel_U12_P12/LConn1 -- C47/LConn1 -- U12/LConn1
  C47/RConn1 -- GND_Label_039/LConn1
  C48/LConn1 -- D3/LConn1 -- ReadLabel_U12_P5/LConn1 -- U12/LConn3
  C48/RConn1 -- GND_Label_040/LConn1
  C7/RConn1 -- GND_Label_043/LConn1
  C8/RConn1 -- GND_Label_044/LConn1
  C9/RConn1 -- GND_Label_045/LConn1
  F3/LConn1 -- CircuitNet_BAT_PLUS/LConn1 -- LTC4364_Protection/RConn1
  CircuitNet_MAIN_EN/LConn1 -- U7/LConn15
  Connection Label/LConn1 -- U7/LConn9
  Connection Label1/LConn1 -- R34/LConn1
  Connection Label2/LConn1 -- U7/LConn10
  Connection Label3/LConn1 -- R41/LConn1
  Connection Label4/LConn1 -- F4/LConn1
  D1/RConn1 -- R36/RConn1 -- R37/LConn1 -- Q1/LConn1
  GND_Label_046/LConn1 -- D2/LConn1 -- R44/RConn1 -- Q2/RConn2
  R44/LConn1 -- D2/RConn1 -- R43/RConn1 -- Q2/LConn1
  D3/RConn1 -- ReadLabel_D3_VSYS_5V/LConn1
  F1/LConn1 -- F4/RConn1
  F2/LConn1 -- PV2/RConn1
  F2/RConn1 -- PVLabel_Input/LConn1 -- PV_Reverse_Protection/LConn1
  GND_Label_047/LConn1 -- PV1/LConn1
  GND_Label_049/LConn1 -- Q3A/RConn2
  GND_Label_050/LConn1 -- Q3B/RConn2
  GND_Label_053/LConn1 -- R1/RConn1
  GND_Label_054/LConn1 -- R18/RConn1
  GND_Label_055/LConn1 -- R21/RConn1
  GND_Label_056/LConn1 -- R24/RConn1
  GND_Label_057/LConn1 -- R35/RConn1
  GND_Label_058/LConn1 -- R42/RConn1
  GND_Label_060/LConn1 -- R48/RConn1
  GND_Label_064/LConn1 -- U1/RConn8
  GND_Label_065/LConn1 -- U1/RConn3
  U10/LConn18 -- GND_Label_069/LConn1 -- U10/LConn17 -- U10/LConn16 -- U10/LConn15 -- U10/LConn14 -- U10/LConn13 -- U10/LConn12 -- U10/LConn11 -- U10/LConn10 -- U10/LConn9 -- U10/LConn8 -- U10/LConn5 -- U10/LConn2 -- U10/LConn1
  GND_Label_080/LConn1 -- U11/LConn3
  GND_Label_081/LConn1 -- U12/LConn2
  GND_Label_085/LConn1 -- U3/LConn2
  GND_Label_086/LConn1 -- U3/LConn3
  GND_Label_087/LConn1 -- U3/LConn4
  GND_Label_088/LConn1 -- U4/RConn1
  GND_Label_089/LConn1 -- U5/RConn1
  GND_Label_090/LConn1 -- U6/RConn1
  GND_Label_091/LConn1 -- U7/LConn3
  GND_Label_092/LConn1 -- U7/LConn8
  GND_Label_093/LConn1 -- U7/LConn13
  GND_Label_094/LConn1 -- U7/LConn18
  GND_Label_095/LConn1 -- U7/RConn18
  GND_Label_096/LConn1 -- U7/RConn13
  GND_Label_097/LConn1 -- U7/RConn8
  GND_Label_098/LConn1 -- U7/RConn3
  GND_Label_099/LConn1 -- U9/RConn3
  L1/RConn1 -- R2/LConn3
  LTC4364_Protection/LConn2 -- ProtectionNet_MCU_EN/LConn1
  LTC4364_Protection/LConn3 -- ProtectionNet_RETURN/LConn1
  LTC4364_Protection/LConn4 -- ProtectionNet_VLOGIC/LConn1
  LTC4364_Protection/RConn2 -- ProtectionNet_FLT/LConn1
  MCU_GP13_Protection/LConn1 -- U7/LConn17
  MeasureLabel_R16_VIN/LConn1 -- R16/LConn1
  MeasureLabel_R19_VOUT/LConn1 -- R19/LConn1
  MeasureLabel_R2_IL_SENSE_M/LConn1 -- R2/LConn1
  MeasureLabel_R2_IL_SENSE_P/LConn1 -- R2/LConn2
  MeasureLabel_U1_ADC_IL/LConn1 -- U1/LConn4
  MeasureLabel_U1_ADC_TBAT/LConn1 -- U1/LConn5
  MeasureLabel_U1_ADC_TSINK/LConn1 -- U1/LConn6
  MeasureLabel_U1_VREF2V5_ADC/LConn1 -- U1/RConn2
  MeasureLabel_U3_IL_SENSE_M/LConn1 -- U3/LConn1
  MeasureLabel_U3_IL_SENSE_P/LConn1 -- U3/RConn1
  MeasureLabel_U3_VREF2V5_ADC/LConn1 -- U3/RConn2
  U6/LConn2 -- MeasureLabel_U6_VREF2V5_ADC/LConn1 -- R30/LConn1
  PV1/RConn1 -- PV2/LConn1
  R35/LConn1 -- Q3A/LConn1 -- R34/RConn1
  Q3A/RConn1 -- R32/RConn1
  R42/LConn1 -- Q3B/LConn1 -- R41/RConn1
  Q3B/RConn1 -- R39/RConn1
  R10/LConn1 -- R9/RConn1
  R11/RConn1 -- R12/LConn1
  R13/RConn1 -- R14/LConn1
  R15/LConn1 -- ReadLabel_R15_V3V3/LConn1
  R15/RConn1 -- ReadLabel_R15_SPI_CS_N/LConn1 -- U1/RConn7
  R16/RConn1 -- R17/LConn1
  R19/RConn1 -- R20/LConn1
  R22/LConn1 -- ReadLabel_R22_BAT_PLUS/LConn1
  R22/RConn1 -- R23/LConn1
  R26/LConn1 -- U3/RConn4
  R28/LConn1 -- U4/LConn2
  R29/LConn1 -- U5/LConn2
  R3/RConn1 -- R4/LConn1
  R31/LConn1 -- ReadLabel_R31_P5/LConn1
  R33/LConn1 -- R31/RConn1 -- U8/LConn1
  R33/RConn1 -- R32/LConn1 -- U8/LConn3
  R36/LConn1 -- U8/RConn2
  R38/LConn1 -- ReadLabel_R38_P5/LConn1
  R40/LConn1 -- R38/RConn1 -- U9/LConn1
  R40/RConn1 -- R39/LConn1 -- U9/LConn3
  R43/LConn1 -- U9/RConn2
  ReadLabel_R45_H12/LConn1 -- R45/LConn1 -- R47/RConn1
  R45/RConn1 -- ReadLabel_R45_H_FB/LConn1
  R46/LConn1 -- ReadLabel_R46_H_FB/LConn1
  R47/LConn1 -- U10/RConn5
  ReadLabel_U7_BIAS_EN/LConn1 -- R48/LConn1 -- U7/LConn11
  ReadLabel_U7_BIAS_PG/LConn1 -- R49/LConn1 -- U7/LConn12
  R49/RConn1 -- ReadLabel_R49_V3V3/LConn1
  R5/RConn1 -- R6/LConn1
  R7/RConn1 -- R8/LConn1
  ReadLabel_U10_BIAS_EN/LConn1 -- U10/LConn4
  ReadLabel_U10_BIAS_PG/LConn1 -- U10/LConn3
  ReadLabel_U1_SPI_MISO/LConn1 -- U1/RConn5
  ReadLabel_U1_SPI_MOSI/LConn1 -- U1/RConn6
  ReadLabel_U1_SPI_SCK/LConn1 -- U1/RConn4
  ReadLabel_U7_SPI_CS_N/LConn1 -- U7/RConn19
  ReadLabel_U7_SPI_MISO/LConn1 -- U7/RConn20
  ReadLabel_U7_SPI_MOSI/LConn1 -- U7/RConn16
  ReadLabel_U7_SPI_SCK/LConn1 -- U7/RConn17
  ReadLabel_U7_V3V3/LConn1 -- U7/RConn5
  ReadLabel_U7_VSYS_5V/LConn1 -- U7/RConn2
  PV_Reverse_Protection/LConn3 -- PVLabel_Module_P3V3/LConn1
  PV_Reverse_Protection/LConn4 -- PVLabel_Module_VREF2V5/LConn1
  PV_Reverse_Protection/LConn2 -- PVLabel_Module_GND/LConn1
  PV_Reverse_Protection/RConn2 -- PVLabel_Module_IPV_OUT/LConn1
  PV_Reverse_Protection/LConn5 -- PVLabel_Module_MCU_RUN/LConn1
  PV_Reverse_Protection/LConn6 -- PVLabel_Module_MCU_REARM/LConn1
  PV_Reverse_Protection/RConn3 -- PVLabel_Module_OC_FAULT_N/LConn1
  PV_Reverse_Protection/RConn4 -- PVLabel_Module_PV_STOPPED/LConn1
  U7/LConn14 -- PVLabel_U7_GP10/LConn1
  U7/LConn16 -- PVLabel_U7_GP12/LConn1
  U7/LConn19 -- PVLabel_U7_GP14/LConn1
  U7/LConn20 -- PVLabel_U7_GP15/LConn1
  PVLabel_ADC_CurrentInput/LConn1 -- R25/LConn1
  U1/LConn2 -- R25/RConn1 -- C23/LConn1
  C23/RConn1 -- GND_Label_017/LConn1
  PVLabel_Voltage_Input/LConn1 -- PV_RV_H1/LConn1
  PV_RV_H1/RConn1 -- PV_RV_H2/LConn1
  U1/LConn8 -- PV_RV_H2/RConn1 -- PV_RV_L/LConn1 -- PV_CV_ADC/LConn1
  PV_RV_L/RConn1 -- PVLabel_Voltage_RGround/LConn1
  PV_CV_ADC/RConn1 -- PVLabel_Voltage_CGround/LConn1
